simulink model "solar_pv_protected_c07_circuit"  (R2026b)
(part 6 of 16)

      | 試験資料            ; C:\Users\hosik\OneDrive\ドキュメント\ChatGPT\oosem\evaluation\pv_protection_integration_20261023_r01\runtime\observations\standard_final_r04_aggregate\aggregate.json
      | 
      | 【通電許可・停止・再許可の流れ】
      | この回路での役割    ; パネルから主電力段への通電を許可し、逆流または異常時に停止し、条件が整うまで勝手に再投入しない。
      | 起動手順1           ; マイコンはMCU_RUNとMCU_REARMをLowに置き、保持回路のクリアを成立させる。電源投入時のQ状態が最初からLowとは仮定しない。
      | 起動手順2           ; PV_U6が3.3Vと2.5Vを監視する。両方が窓内に入り復帰待ち時間を経たとき、2本のRESETが解放されANALOG_OKがHighになる。
      | 起動手順3           ; マイコンはADC CH7の保護前PV電圧とCH0の保護後VINを十分に整定して読み、入力電圧・電圧差・故障原因の解消を確認する。OFF中の電流ゼロだけを理由に復帰しない。
      | 起動手順4           ; MCU_RUNをHighへ上げる。REV_OK/ANALOG_OK/MCU_RUNがそろってクリアが解除された後、MCU_REARMへ短い立上りパルスを1回与える。Q=PV_ALLOWがHighとなる。
      | 起動手順5           ; LTC7000A自身のUV/OV・電源準備・過電流条件も成立したときゲートを充電する。RGと追加RCでON側の傾きを抑える。これは主電力段Q1/Q2のPWM制御とは別の保護開閉。
      | 逆流した場合        ; U2の出力がV_REVを下回るとPV_U3がREV_OKをLowへ下げる。公称判定は約−0.5A。AND出力がLowとなりPV_U5を非同期クリアし、PV_ALLOW Lowでゲートを放電する。停止後も保持し、再許可パルスなしに復帰しない。
      | 順方向の異常        ; LTC7000AがR27の差動電圧から順方向過電流を判定する。ISET=GND/1mΩの公称検出は約20A。UV/OVも独立に判定する。OC_FAULT_NはLow有効の故障通知。マイコンは原因を確認しRUNをLowへ戻してから復帰手順を行う設計意図。
      | 停止情報            ; PV_STOPPEDは保持回路の反転出力。実際のMOSFET遮断や故障原因を単独で保証しない。OC_FAULT_Nと電圧・電流測定を用途に応じて併用する。
      | 確認の境界          ; 試験で与えた指令・境界条件と、RP2040上で動くMicroPythonプログラムの実行確認は別。今回の記述は実ファームウェアの動作試験を実施したという意味ではない。
      | 試験との対応        ; この図面は実部品の端子と接続を示す。保存実行モジュール SHA256=f40bf5e1ef20bc97d0d4775a6ac457f3c30378c5fe9d07d29ab7bde4d975da32 の数値計算用ICコアを図面コピーから除去してある。実行用のICはメーカーのトランジスタモデルではなく、限定範囲の近似動作モデル。試験の合否と条件は C:\Users\hosik\OneDrive\ドキュメント\ChatGPT\oosem\evaluation\pv_protection_integration_20261023_r01\runtime\observations\standard_final_r04_aggregate\aggregate.json を参照する。
      | 用語と記号          ; IC：Integrated Circuit（集積回路）。GND：Ground（共通の基準電位・電流帰路）。MCU：Microcontroller Unit（マイコン）。High/Low：デジタル信号の高/低レベル。UV：Under Voltage（低電圧）、OV：Over Voltage（過電圧）、OC：Over Current（過電流）。SOA：Safe Operating Area（安全動作領域）。末尾NはLowで有効になる信号を表す。
      | 
      | 【c07 図面整理】
      | 機能区画Gate_Driver / Reverse_Detector / Stop_Latchを展開。GND以外のConnection Labelを直接配線へ置換。ICは一部品として表示。元c06の電気的接続・部品値・型番を保持する静的な図面変更。動作試験の再実行や実機確認ではない。
      mask Display: disp(sprintf('パネル側保護回路 c06\nLTC7000A / 逆流判定 / 停止保持\nダブルクリックで詳細'));port_label('lconn',1,'PV_IN');port_label('lconn',2,'GND');port_label('lconn',3,'P3V3');port_label('lconn',4,'VREF2V5');port_label('lconn',5,'MCU_RUN');port_label('lconn',6,'MCU_REARM');port_label('rconn',1,'PV_OUT');port_label('rconn',2,'IPV_OUT');port_label('rconn',3,'OC_FAULT_N');port_label('rconn',4,'PV_STOPPED');
  ProtectionNet_FLT : ConnectionLabel  Description=|  Label=PROTECTION_FLT_N
      | この回路での名前　　; PROTECTION_FLT_N
      | 種別　　　　　　　　; ConnectionLabel
      | この回路での役割　　; 保護IC P_U1のFLT出力から、RP2040基板U7のGP13へ異常状態を返す。P_RFLT_PUを介して3.3Vへプルアップされる。すべての異常や逆流を個別通知する信号ではない。
      | この場所の直接接続　; P_RFLT_PU（LTC4364のオープンドレインFLTをMCUの3.3 V系へ引き上げる／22 kΩ）: 2
      |                     ; P_U1（保護MOSFETを制御する保護IC／LTC4364IMS-1#PBF）: FLT
      | 直接接続の範囲　　　; このラベルから実際の線・分岐・明示的な境界端子だけを追った接続。同名ラベルによる離れた場所への接続はこの欄に含めない。
      | 同一ネットの主接続　; P_U1（保護MOSFETを制御する保護IC／LTC4364IMS-1#PBF）: FLT
      |                     ; U7（RP2040搭載Pico W／SC0918）: 17(GP13)
      |                     ; P_RFLT_PU（LTC4364のオープンドレインFLTをMCUの3.3 V系へ引き上げる／22 kΩ）: 2
      | 同一ネット全端子　　; P_RFLT_PU: 2
      |                     ; P_U1: FLT
      |                     ; U7: 17(GP13)
      | 接続部品数　　　　　; 3部品（部品番号で集計。同一ネット全体）
      | 接続端子数　　　　　; 3端子（423端子の部品対応表で集計。ラベル・境界ポートの重複は含めない）
      | この場所の端子数　　; 2端子／2部品（同名ラベルによる接続を除く）
      | 同階層同名ラベル数　; 2個（このラベル自身を含む）
      | 全階層の接続ラベル　; 2個（実際に同じノードへつながるラベル。名前が違う別名も含む）
      | 接続ルール　　　　　; 同じ階層の同じラベル名を仮想配線として結ぶ。別のSubsystem内とは名前だけでつながらず、明示的なConnection Portと配線をたどる。色は用途の表示であり接続を決めない。
      | 確認の範囲　　　　　; 現在の保存回路の端子・配線から求めた静的接続。抵抗やICの内部を導線として短絡せずに集計した。説明の更新は動作シミュレーション、タイミング、実部品の性能・実機動作を保証するものではない。
      | 記録の基準　　　　　; measurement_label_layout_20261022_r01/after_layout_graph.json。部品対応表は端子名の対応付けにのみ使用。
      | 
      | 【この説明欄の略語・記号】
      | 用語1　　　　　　　 ; IC：Integrated Circuit（集積回路）。複数の電子素子と機能を小さな半導体チップに集積した部品。
      | 用語2　　　　　　　 ; MCU：Microcontroller Unit（マイクロコントローラ）。プログラムを実行し、測定値の処理や出力制御を担当する小型計算機。
      | 用語3　　　　　　　 ; GPIO：General-Purpose Input/Output（汎用入出力端子）。入力・出力や周辺機能に割り当てられる端子。GPの後の数字はRP2040の端子信号番号で、基板上の物理ピン番号とは別。
      | 用語4　　　　　　　 ; MOSFET：Metal-Oxide-Semiconductor Field-Effect Transistor（金属・酸化膜・半導体構造の電界効果トランジスタ）。ゲートとソースの電圧でドレインとソースの導通を制御する素子。N-MOSはNチャネル型を表す。
      | 用語5　　　　　　　 ; FLT：Fault（故障状態通知）。LTC4364の故障警告出力。全種類の異常や逆流を一律に通知する信号という意味ではない。
  ProtectionNet_MCU_EN : ConnectionLabel  Description=|  Label=MAIN_EN
      | この回路での名前　　; MAIN_EN
      | 種別　　　　　　　　; ConnectionLabel
      | この回路での役割　　; RP2040基板U7のGP11から、保護回路の停止入力へ指令を渡す。直接同じノードなのは直列抵抗P_RSHDN_SERの入力側までで、保護ICのSHDNにはこの抵抗を介して接続する。
      | この場所の直接接続　; P_RSHDN_SER（RP2040のMAIN_ENとLTC4364のSHDN間へ入る／1 kΩ）: 1
      | 直接接続の範囲　　　; このラベルから実際の線・分岐・明示的な境界端子だけを追った接続。同名ラベルによる離れた場所への接続はこの欄に含めない。
      | 同一ネットの主接続　; U7（RP2040搭載Pico W／SC0918）: 15(GP11)
      |                     ; P_RSHDN_SER（RP2040のMAIN_ENとLTC4364のSHDN間へ入る／1 kΩ）: 1
      | 同一ネット全端子　　; P_RSHDN_SER: 1
      |                     ; U7: 15(GP11)
      | 接続部品数　　　　　; 2部品（部品番号で集計。同一ネット全体）
      | 接続端子数　　　　　; 2端子（423端子の部品対応表で集計。ラベル・境界ポートの重複は含めない）
      | この場所の端子数　　; 1端子／1部品（同名ラベルによる接続を除く）
      | 同階層同名ラベル数　; 2個（このラベル自身を含む）
      | 全階層の接続ラベル　; 2個（実際に同じノードへつながるラベル。名前が違う別名も含む）
      | 接続ルール　　　　　; 同じ階層の同じラベル名を仮想配線として結ぶ。別のSubsystem内とは名前だけでつながらず、明示的なConnection Portと配線をたどる。色は用途の表示であり接続を決めない。
      | 確認の範囲　　　　　; 現在の保存回路の端子・配線から求めた静的接続。抵抗やICの内部を導線として短絡せずに集計した。説明の更新は動作シミュレーション、タイミング、実部品の性能・実機動作を保証するものではない。
      | 記録の基準　　　　　; measurement_label_layout_20261022_r01/after_layout_graph.json。部品対応表は端子名の対応付けにのみ使用。
      | 
      | 【この説明欄の略語・記号】
      | 用語1　　　　　　　 ; IC：Integrated Circuit（集積回路）。複数の電子素子と機能を小さな半導体チップに集積した部品。
      | 用語2　　　　　　　 ; MCU：Microcontroller Unit（マイクロコントローラ）。プログラムを実行し、測定値の処理や出力制御を担当する小型計算機。
      | 用語3　　　　　　　 ; GPIO：General-Purpose Input/Output（汎用入出力端子）。入力・出力や周辺機能に割り当てられる端子。GPの後の数字はRP2040の端子信号番号で、基板上の物理ピン番号とは別。
      | 用語4　　　　　　　 ; SHDN：Shutdown（停止制御端子）。LTC4364ではLowで停止を指示する。Highは動作許可であり、保護判定を無効にするものではない。
      | 用語5　　　　　　　 ; EN：Enable（動作許可）。対象機能の動作を許可する信号。端子ごとの有効レベルや接続状態に従う。
  ProtectionNet_RETURN : ConnectionLabel  Description=|  Label=GND
      | この回路での名前　　; GND
      | 種別　　　　　　　　; ConnectionLabel
      | この回路での役割　　; 電池BT1の負極、太陽電池列の負極、制御・測定・保護回路のGNDを結ぶ共通の帰路。高側駆動の浮動帰路SWとは別のノード。
      | 共通帰路の代表接続　; BT1（充電先の蓄電池／51.2V 100Ah LiFePO4）: -
      |                     ; PV1（直列太陽電池列の負極側パネル／400W panel 1/2）: -
      |                     ; U7（RP2040搭載Pico W／SC0918）: 3(GND), 8(GND), 13(GND), 18(GND), 23(GND), 28(GND), 33(AGND), 38(GND)
      |                     ; U1（外付けADC／MCP3208-CI/SL）: 8(CH7), 9(DGND), 14(AGND)
      |                     ; P_U1（保護MOSFETを制御する保護IC／LTC4364IMS-1#PBF）: GND
      |                     ; Q2（同期整流降圧回路の下側スイッチ／TK9R6E15Q5,S1X）: 3(S)
      |                     ; U9（低側の光ゲートドライバ／ACPL-P346-560E）: 4(VEE)
      |                     ; U10（高側ゲート用の浮動電源を作る絶縁DC/DC／UCC14131QDWNRQ1）: 1(GNDP), 2(GNDP), 5(GNDP), 8(GNDP), 9(GNDP), 10(GNDP), 11(GNDP), 12(GNDP), 13(GNDP), 14(GNDP), 15(GNDP), 16(GNDP), 17(GNDP), 18(GNDP)
      | この場所の直接接続　; P_RSHDN_PD（SHDNをGNDへ下げ、MCU未駆動時に停止側へ保つ／47 kΩ）: 2
      | 直接接続の範囲　　　; このラベルから実際の線・分岐・明示的な境界端子だけを追った接続。同名ラベルによる離れた場所への接続はこの欄に含めない。
      | 同一ネット全端子　　; BT1: -
      |                     ; C1: 2(n)
      |                     ; C2: 2(n)
      |                     ; C3: 2(n)
      |                     ; C4: 2(n)
      |                     ; C7: 2(n)
      |                     ; C8: 2(n)
      |                     ; C9: 2(n)
      |                     ; C10: 2(n)
      |                     ; C13: 2(n)
      |                     ; C14: 2(n)
      |                     ; C15: 2(n)
      |                     ; C16: 2(n)
      |                     ; C17: 2
      |                     ; C18: 2
      |                     ; C19: 2
      |                     ; C20: 2
      |                     ; C21: 2
      |                     ; C22: 2
      |                     ; C23: 2
      |                     ; C24: 2
      |                     ; C25: 2
      |                     ; C26: 2
      |                     ; C27: 2
      |                     ; C28: 2
      |                     ; C29: 2
      |                     ; C30: 2
      |                     ; C31: 2
      |                     ; C33: 2
      |                     ; C34: 2
      |                     ; C35: 2
      |                     ; C36: 2
      |                     ; C40: 2
      |                     ; C41: 2
      |                     ; C42: 2
      |                     ; C43: 2
      |                     ; C44: 2
      |                     ; C45: 2
      |                     ; C46: 2
      |                     ; C47: 2
      |                     ; C48: 2
      |                     ; D2: 2(A)
      |                     ; PV1: -
      |                     ; P_CHG: N
      |                     ; P_COUT: N
      |                     ; P_CTMR: N
      |                     ; P_D1: A
      |                     ; P_R3: 2
      |                     ; P_R8: 2
      |                     ; P_RSHDN_PD: 2
      |                     ; P_U1: GND
      |                     ; Q2: 3(S)
      |                     ; Q3: 1(S1), 4(S2)
      |                     ; R1: 2(n)
      |                     ; R18: 2
      |                     ; R21: 2
      |                     ; R24: 2
      |                     ; R35: 2
      |                     ; R42: 2
      |                     ; R44: 2
      |                     ; R48: 2
      |                     ; U1: 8(CH7), 9(DGND), 14(AGND)
      |                     ; U2: 2(GND), 3(REF2), 4(RESERVED_GND)
      |                     ; U3: 2(GND), 3(REF2), 4(RESERVED_GND)
      |                     ; U4: 3(GND)
      |                     ; U5: 3(GND)
      |                     ; U6: 3(GND)
      |                     ; U7: 3(GND), 8(GND), 13(GND), 18(GND), 23(GND), 28(GND), 33(AGND), 38(GND)
      |                     ; U9: 4(VEE)
      |                     ; U10: 1(GNDP), 2(GNDP), 5(GNDP), 8(GNDP), 9(GNDP), 10(GNDP), 11(GNDP), 12(GNDP), 13(GNDP), 14(GNDP), 15(GNDP), 16(GNDP), 17(GNDP), 18(GNDP)
      |                     ; U11: 2(GND)
      |                     ; U12: 2(GND)
      | 接続部品数　　　　　; 72部品（部品番号で集計。同一ネット全体）
      | 接続端子数　　　　　; 99端子（423端子の部品対応表で集計。ラベル・境界ポートの重複は含めない）
      | この場所の端子数　　; 1端子／1部品（同名ラベルによる接続を除く）
      | 同階層同名ラベル数　; 75個（このラベル自身を含む）
      | 全階層の接続ラベル　; 87個（実際に同じノードへつながるラベル。名前が違う別名も含む）
      | 接続ルール　　　　　; 同じ階層の同じラベル名を仮想配線として結ぶ。別のSubsystem内とは名前だけでつながらず、明示的なConnection Portと配線をたどる。色は用途の表示であり接続を決めない。
      | 確認の範囲　　　　　; 現在の保存回路の端子・配線から求めた静的接続。抵抗やICの内部を導線として短絡せずに集計した。説明の更新は動作シミュレーション、タイミング、実部品の性能・実機動作を保証するものではない。
      | 記録の基準　　　　　; measurement_label_layout_20261022_r01/after_layout_graph.json。部品対応表は端子名の対応付けにのみ使用。
      | 
      | 【この説明欄の略語・記号】
      | 用語1　　　　　　　 ; DC：Direct Current（直流）。ここでは直流電源または直流成分。DCバイアスはコンデンサに重なる直流電圧を指す。
      | 用語2　　　　　　　 ; DC/DC：DC-to-DC Converter（直流電圧変換器）。直流入力を別の直流電圧へ変換する電源回路。絶縁の有無は個々の部品説明で確認する。
      | 用語3　　　　　　　 ; ADC：Analog-to-Digital Converter（アナログ・デジタル変換器）。測定電圧をデジタル値へ変換する回路。電流や温度も、センサーで電圧へ変換した後に読み取る。
      | 用語4　　　　　　　 ; IC：Integrated Circuit（集積回路）。複数の電子素子と機能を小さな半導体チップに集積した部品。
      | 用語5　　　　　　　 ; MCU：Microcontroller Unit（マイクロコントローラ）。プログラムを実行し、測定値の処理や出力制御を担当する小型計算機。
      | 用語6　　　　　　　 ; CH：Channel（測定チャネル）。CH0〜CH7はADCの入力番号であり、同時測定を意味しない。
      | 用語7　　　　　　　 ; MOSFET：Metal-Oxide-Semiconductor Field-Effect Transistor（金属・酸化膜・半導体構造の電界効果トランジスタ）。ゲートとソースの電圧でドレインとソースの導通を制御する素子。N-MOSはNチャネル型を表す。
      | 用語8　　　　　　　 ; LiFePO4：Lithium Iron Phosphate（リン酸鉄リチウム）。電池の正極材料を示す化学式。英語の頭文字を並べた略語ではない。
      | 用語9　　　　　　　 ; GND：Ground（回路の基準電位・電流帰路）。この図の共通基準。保護接地や大地への接続を意味するとは限らない。
      | 用語10　　　　　　　; AGND：Analog Ground（アナログ回路の基準端子）。アナログ部分の電流帰路。現図では共通GNDへ接続されるが、実装時の電流経路への配慮は別途必要。
      | 用語11　　　　　　　; DGND：Digital Ground（デジタル回路の基準端子）。デジタル部分の電流帰路。現図では共通GNDへ接続される。
      | 用語12　　　　　　　; SHDN：Shutdown（停止制御端子）。LTC4364ではLowで停止を指示する。Highは動作許可であり、保護判定を無効にするものではない。
      | 用語13　　　　　　　; VREF/REF：基準電圧を表す端子名。REFはReference（基準）の意味。ADCの変換尺度や電流アンプの出力基準に使う。REF1/REF2の接続電位は個別に確認する。
      | 用語14　　　　　　　; VCC/VDD/VEE/VS：ICの電源端子名。文字の歴史的な由来を現在の接続機能へ当てはめない。現回路のVEEはU8/U10では浮動基準SW、U9ではGND。各電圧・基準は端子と接続を参照する。
      | 用語15　　　　　　　; GNDP：U10の一次側電源の基準端子。絶縁電源の入力側GND。二次側基準VEE=SWと直接同一の導体ではない。
      | 用語16　　　　　　　; SW：Switching Node（スイッチング点）。主電力段の上下MOSFETとL1がつながる、電圧が高速に切り替わる点。GNDとは別電位。
  ProtectionNet_VLOGIC : ConnectionLabel  Description=|  Label=V3V3
      | この回路での名前　　; V3V3
      | 種別　　　　　　　　; ConnectionLabel
      | この回路での役割　　; RP2040基板U7の3.3V出力から、ADC・電流検出IC・温度センサー・基準電圧ICなどへ電源を分配する。信号のプルアップ抵抗にも供給する。
      | この場所の直接接続　; P_RFLT_PU（LTC4364のオープンドレインFLTをMCUの3.3 V系へ引き上げる／22 kΩ）: 1
      | 直接接続の範囲　　　; このラベルから実際の線・分岐・明示的な境界端子だけを追った接続。同名ラベルによる離れた場所への接続はこの欄に含めない。
      | 同一ネットの主接続　; U7（RP2040搭載Pico W／SC0918）: 36(3V3_OUT)
      |                     ; U1（外付けADC／MCP3208-CI/SL）: 16(VDD)
      |                     ; U2（PV入力電流の検出アンプ／INA241A3IDDFR）: 6(VS)
      |                     ; U3（L1直後の出力電流の検出アンプ／INA241A3IDDFR）: 6(VS)
      |                     ; U4（電池温度センサー／TMP235A2DBZR）: 1(VDD)
      |                     ; U5（放熱器温度センサー／TMP235A2DBZR）: 1(VDD)
      |                     ; U6（2.5Vの測定基準電圧源／REF3025EAIDBZR）: 1(IN)
      |                     ; R49（U10のオープンドレインPG信号BIAS_PGをPicoの3V3へ引き上げ、GP9で読める電圧にする／10k 1%）: 2
      |                     ; P_RFLT_PU（LTC4364のオープンドレインFLTをMCUの3.3 V系へ引き上げる／22 kΩ）: 1
      | 同一ネット全端子　　; C17: 1
      |                     ; C18: 1
      |                     ; C22: 1
      |                     ; C24: 1
      |                     ; C26: 1
      |                     ; C28: 1
      |                     ; C30: 1
      |                     ; P_RFLT_PU: 1
      |                     ; R15: 1
      |                     ; R49: 2
      |                     ; U1: 16(VDD)
      |                     ; U2: 6(VS)
      |                     ; U3: 6(VS)
      |                     ; U4: 1(VDD)
      |                     ; U5: 1(VDD)
      |                     ; U6: 1(IN)
      |                     ; U7: 36(3V3_OUT)
      | 接続部品数　　　　　; 17部品（部品番号で集計。同一ネット全体）
      | 接続端子数　　　　　; 17端子（423端子の部品対応表で集計。ラベル・境界ポートの重複は含めない）
      | この場所の端子数　　; 1端子／1部品（同名ラベルによる接続を除く）
      | 同階層同名ラベル数　; 10個（このラベル自身を含む）
      | 全階層の接続ラベル　; 10個（実際に同じノードへつながるラベル。名前が違う別名も含む）
      | 接続ルール　　　　　; 同じ階層の同じラベル名を仮想配線として結ぶ。別のSubsystem内とは名前だけでつながらず、明示的なConnection Portと配線をたどる。色は用途の表示であり接続を決めない。
      | 確認の範囲　　　　　; 現在の保存回路の端子・配線から求めた静的接続。抵抗やICの内部を導線として短絡せずに集計した。説明の更新は動作シミュレーション、タイミング、実部品の性能・実機動作を保証するものではない。
      | 記録の基準　　　　　; measurement_label_layout_20261022_r01/after_layout_graph.json。部品対応表は端子名の対応付けにのみ使用。
      | 
      | 【この説明欄の略語・記号】
      | 用語1　　　　　　　 ; ADC：Analog-to-Digital Converter（アナログ・デジタル変換器）。測定電圧をデジタル値へ変換する回路。電流や温度も、センサーで電圧へ変換した後に読み取る。
      | 用語2　　　　　　　 ; IC：Integrated Circuit（集積回路）。複数の電子素子と機能を小さな半導体チップに集積した部品。
      | 用語3　　　　　　　 ; MCU：Microcontroller Unit（マイクロコントローラ）。プログラムを実行し、測定値の処理や出力制御を担当する小型計算機。
      | 用語4　　　　　　　 ; GPIO：General-Purpose Input/Output（汎用入出力端子）。入力・出力や周辺機能に割り当てられる端子。GPの後の数字はRP2040の端子信号番号で、基板上の物理ピン番号とは別。
      | 用語5　　　　　　　 ; MOSFET：Metal-Oxide-Semiconductor Field-Effect Transistor（金属・酸化膜・半導体構造の電界効果トランジスタ）。ゲートとソースの電圧でドレインとソースの導通を制御する素子。N-MOSはNチャネル型を表す。
      | 用語6　　　　　　　 ; PV：Photovoltaic（太陽光発電）。光を電気へ変える発電方式。PVを含むネット名は太陽電池側の測定・電力経路を表す。
      | 用語7　　　　　　　 ; GND：Ground（回路の基準電位・電流帰路）。この図の共通基準。保護接地や大地への接続を意味するとは限らない。
      | 用語8　　　　　　　 ; PG：Power Good（電源状態通知）。電源出力が規定状態にあるかを知らせる信号。プルアップ条件と実際の通知条件は対象ICの説明で確認する。
      | 用語9　　　　　　　 ; FLT：Fault（故障状態通知）。LTC4364の故障警告出力。全種類の異常や逆流を一律に通知する信号という意味ではない。
      | 用語10　　　　　　　; VCC/VDD/VEE/VS：ICの電源端子名。文字の歴史的な由来を現在の接続機能へ当てはめない。現回路のVEEはU8/U10では浮動基準SW、U9ではGND。各電圧・基準は端子と接続を参照する。
      | 用語11　　　　　　　; SW：Switching Node（スイッチング点）。主電力段の上下MOSFETとL1がつながる、電圧が高速に切り替わる点。GNDとは別電位。
  Q1 : ee_lib/Semiconductors & Converters/N-Channel MOSFET  Description=|  paramTerminal=ee.enum.mosfet.numberOfTerminals.three  parameterization=ee.enum.mosfet.parameterization.datasheet  Beta=5.0 A/V^2  Rds=0.025 Ohm  Id=6.0 A  Vgs=10 V  Vth=1.7 V  Vth0=1.7 V  lam=0 1/V  gamma_vth=0.5 V^(1/2)  phib=0.5 V  Vth1=1.9071 V  Vbs1=-1 V  Vth2=2.066 V  Vbs2=-2 V  Tmeas=25 degC  Vgs_vec=[-1, -.5, 2, 3, 4, 5] V  Vds_vec=[0, 2, 4, 8, 12, 16, 20] V  Vbs_vec=[0, -4, -6, -12] V  T_vec=[25, 125] degC  Vth_vec=[.4, 1.2, 1.4, 1.45] V  Vth_mat=[.4, .35; 1.2, 1.15; 1.4, 1.35; 1.45, 1.4] V  Ids_mat=[0, 0, 0, 0, 0, 0, 0; 0, 0, 0, 0, 0, 0, 0; 0, .003, .0038, .0043, .0046, .0048, .0049; 0, .0055, .008, .009, .0095, .01, .0101; 0, .0115, .016, .018, .019, .0195, .02; 0, .0152, .0225, .0265, .028, .0295, .03] A  Ids_mat0=[0, 0, 0, 0, 0, 0, 0; 0, 0, 0, 0, 0, 0, 0; 0, .003, .0038, .0043, .0046, .0048, .0049; 0, .0055, .008, .009, .0095, .01, .0101; 0, .0115, .016, .018, .019, .0195, .02; 0, .0152, .0225, .0265, .028, .0295, .03] A  Ids_mat_3D=zeros(6, 7, 2) A  Ids_mat_3D0=zeros(6, 7, 2) A  IV_table_symmetry=ee.enum.mosfet.symmetricNIV.no  RS=0.0001 Ohm  RD=0.01 Ohm  RB=0.001 Ohm  LeadRs=0 Ohm  LeadRd=0 Ohm  LeadRg=0 Ohm  LeadRb=0 Ohm  LS=0 nH  LD=0 nH  LG=0 nH  LB=0 nH  C_param=ee.enum.mosfet.capacitanceParam.fixedciss  C_GS=270 pF  C_GD=80 pF  C_GB=0 pF  C_DS=0 pF  C_iss=350 pF  C_rss=80 pF  C_oss=0 pF  C_iss_vec=[720, 700, 590, 470, 390, 310] pF  C_rss_vec=[450, 400, 300, 190, 95, 55] pF  C_oss_vec=[900, 810, 690, 420, 270, 170] pF  C_GS_vec=[270, 300, 290, 280, 295, 255] pF  C_GD_vec=[450, 400, 300, 190, 95, 55] pF  C_GB_vec=[270, 300, 290, 280, 295, 255] pF  C_Vgs_vec=0 V  C_DS_vec=[450, 410, 390, 230, 175, 115] pF  C_Vds_vec=[.1, .3, 1, 3, 10, 30] V  V_GS_for_cap_data=0 V  charge_linearity_param=ee.enum.mosfet.cgdLinearity.constant  C_OX=200 pF  V_C_OX=-0.5 V  charge_linearity_param_vgb=ee.enum.mosfet.cgbLinearity.instantly  charge_linearity_param_with_vgb=ee.enum.mosfet.cgbLinearityWithSeparateCgb.instantly  Di_param=ee.enum.mosfet.diodeParam.no  IsDiode=1e-12 A  Vbi=0.6 V  n=1  Cj0Diode=0 pF  TT=50e-9 s  Tmeas_dio=25 degC  TableTypeNoT=ee.enum.mosfet.tableType.IfMat  TableType=ee.enum.diode.tableType.IfMat  IfVec=[.07, .12, .19, 1.75, 4.24, 7.32, 11.2] A  IfMat=[.07, .12, .19, 1.75, 4.24, 7.32, 11.2; .16, .3, .72, 2.14, 4.02, 6.35, 9.12] A  VfVecV=[.9, 1.15, 1.25, 1.5, 1.75, 2.17, 2.6, 2.85] V  VfMatV=[.9, 1.15, 1.25, 1.5, 1.75, 2.17, 2.6, 2.85; .58, .68, .75, 1.1, 1.38, 1.77, 2.27, 2.7] V  TjVec=[25, 125] degC  VfVec=[.5, .7, .9, 1.3, 1.7, 2.1, 2.5] V  IfVecV=[.1, .2, .5, 1, 2, 4, 7, 10] A  diode_Goff=1e-12 1/Ohm  prmDatasheet=ee.enum.temperatureParameterization.none  prmEquCoeff=ee.enum.temperatureParameterization.none  dVth_dT=-6 mV/K  dVth0_dT=-6 mV/K  Rds_T2=0.037 Ohm  BEXDatasheet=-1.5  BEXEquCoeff=-1.5  etaisDatasheet=3  etaisEquCoeff=3  Tmeas2=125 degC  etaisTabulated=3  TdeviceDatasheet=25 degC  TdeviceEquCoeff=25 degC  TdeviceTabulated=25 degC  i_g_specify=off  i_g_priority=None  i_g=0 A  i_g_nominal_specify=off  i_g_nominal_value=1  i_g_nominal_unit=A  i_d_specify=off  i_d_priority=None  i_d=0 A  i_d_nominal_specify=off  i_d_nominal_value=1  i_d_nominal_unit=A  i_b_specify=off  i_b_priority=None  i_b=0 A  i_b_nominal_specify=off  i_b_nominal_value=1  i_b_nominal_unit=A  voltage_gs_specify=off  voltage_gs_priority=None  voltage_gs=0 V  voltage_gs_nominal_specify=off  voltage_gs_nominal_value=1  voltage_gs_nominal_unit=V  voltage_ds_specify=off  voltage_ds_priority=None  voltage_ds=0 V  voltage_ds_nominal_specify=off  voltage_ds_nominal_value=1  voltage_ds_nominal_unit=V  voltage_bs_specify=off  voltage_bs_priority=None  voltage_bs=0 V  voltage_bs_nominal_specify=off  voltage_bs_nominal_value=1  voltage_bs_nominal_unit=V  v_Cgs_specify=off  v_Cgs_priority=High  v_Cgs=0 V  v_Cgs_nominal_specify=off  v_Cgs_nominal_value=1  v_Cgs_nominal_unit=V  v_Cds_specify=off  v_Cds_priority=High  v_Cds=0 V  v_Cds_nominal_specify=off  v_Cds_nominal_value=1  v_Cds_nominal_unit=V  v_Cbs_specify=off  v_Cbs_priority=High  v_Cbs=0 V  v_Cbs_nominal_specify=off  v_Cbs_nominal_value=1  v_Cbs_nominal_unit=V  thermal_network_parameterization=ee.enum.thermalNetworkTopology.junctionCase  Rth=[0, 10] K/W  Rth_Cauer=[1, 3, 10] K/W  Rth_Foster=[.08, .14, .22, .16] K/W  thermal_mass_parameterization=ee.enum.thermalNetwork.timeconstant  thermal_mass=[0, 1] J/K  thermal_mass_Cauer=[.1, .3, 1] J/K  thermal_mass_Foster=[.001, .005, .05, .5] J/K  thermal_time_constant=[0, 10] s  thermal_time_constant_Cauer=[1, 3, 10] s  thermal_time_constant_Foster=[7e-05, .0007, .01, .08] s  thermal_mass_initial_temperatures=[25, 25] degC  thermal_mass_initial_temperatures_Cauer=[25, 25, 25] degC  Tvec_initial_Foster=[25, 25, 25, 25] degC  betaref=18 A/V^2  Vfbref=-1.1 V  gamma=3.5 V^(1/2)  phib2ref=1 V  thesatref=0.4 1/V  alpha=0  Vp=5e-2 V  thesrref=0 1/V  m=8  Tref=25 degC  Rsref=2e-3 Ohm  Rdref=0.17 Ohm  Rgref=8.4 Ohm  Rbref=2e-3 Ohm  Cox=1500 pF  Cgso=100 pF  Cgdo=14 pF  Isref=5.2e-13 A  Cj0=480 pF  Tprm=ee.enum.temperatureParameterization.none  etabet=1.3  Stvfb=5e-4 V/K  Stphib=-8.5e-4 V/K  etasat=1.04  etasr=0.65  etar=0.95  etais=3  Tsim=25 degC  Ig_specify=off  Ig_priority=None  Ig=0 A  Ig_nominal_specify=off  Ig_nominal_value=1  Ig_nominal_unit=nA  Ids_specify=off  Ids_priority=None  Ids=0 A  Ids_nominal_specify=off  Ids_nominal_value=1  Ids_nominal_unit=A  Ib_specify=off  Ib_priority=None  Ib=0 A  Ib_nominal_specify=off  Ib_nominal_value=1  Ib_nominal_unit=uA  V_gs_specify=off  V_gs_priority=None  V_gs=0 V  V_gs_nominal_specify=off  V_gs_nominal_value=1  V_gs_nominal_unit=V  V_ds_specify=off  V_ds_priority=None  V_ds=0 V  V_ds_nominal_specify=off  V_ds_nominal_value=1  V_ds_nominal_unit=V  V_bs_specify=off  V_bs_priority=None  V_bs=0 V  V_bs_nominal_specify=off  V_bs_nominal_value=1  V_bs_nominal_unit=V  QGoverCox_specify=off  QGoverCox_priority=None  QGoverCox=0 V  QGoverCox_nominal_specify=off  QGoverCox_nominal_value=1  QGoverCox_nominal_unit=V  QDoverCox_specify=off  QDoverCox_priority=None  QDoverCox=0 V  QDoverCox_nominal_specify=off  QDoverCox_nominal_value=1  QDoverCox_nominal_unit=V  QBoverCox_specify=off  QBoverCox_priority=None  QBoverCox=0 V  QBoverCox_nominal_specify=off  QBoverCox_nominal_value=1  QBoverCox_nominal_unit=V  T0=[25, 25] degC  T0_Cauer=[25, 25, 25] degC
      | この回路での名前　　; Q1
      | 部品名　　　　　　　; TK9R6E15Q5,S1X
      | この回路での役割　　; 太陽電池から主インダクタL1へ電力を送り込む、降圧回路の上側スイッチ。
      | ここでの動き　　　　; ゲートドライバU8の指令でON/OFFし、入力電源をL1側へつなぐ時間を調整する。ソースの電圧も上下するため、ゲートはソースSWに対する電圧で駆動する。
      | 
      | 【詳しい働き・仕様・接続・確認の範囲】
      | 部品種別　　　　　　; 上側NチャネルMOSFET
      | 公称値　　　　　　　; TK9R6E15Q5,S1X
      | 配置目的　　　　　　; 同期整流降圧回路の上側スイッチ。VINをSWへ断続的に接続し、L1へエネルギーを渡す。
      | 意図する動作　　　　; U8からR36を介して駆動。ソースSWはスイッチングするため、ゲート電圧はSW基準で扱う。Q2との同時ONを避ける必要がある。
      | 端子と接続　　　　　; 3 S → SW、1 G → GATE_H、2 D → VIN
      | モデルの範囲　　　　; Simscape標準NチャネルMOSFETの近似。掲載型番の全特性へ同定済みではなく、設定値とメーカー定格を区別する。Idはモデル校正用電流で最大許容電流ではない。
      | モデル設定　　　　　; Rds=25 mΩ、Vgs=10 V、Id=6 A、Vth=1.7 V、LeadRg=0 Ω。これらは保存モデルの設定値であり、すべてが実部品の保証値という意味ではない。
      | 確認の範囲　　　　　; 本説明は保存回路の部品情報・端子割当・既存設計意図を整理したもの。今回の説明更新によって新たな動作試験や実機検証を実施した意味ではない。
      | 設計記録　　　　　　; evaluation\component_annotations_20261022_r01\before_graph.json
      | evaluation\component_annotations_20261022_r01\before_metadata.json
      | evaluation\protection_capacitor_integration_20261021_r01\final_delivery\independent_readback\physical_bom.json
      | 
      | 【この説明欄の略語・記号】
      | 用語1　　　　　　　 ; MOSFET：Metal-Oxide-Semiconductor Field-Effect Transistor（金属・酸化膜・半導体構造の電界効果トランジスタ）。ゲートとソースの電圧でドレインとソースの導通を制御する素子。N-MOSはNチャネル型を表す。
      | 用語2　　　　　　　 ; VGS：Gate-to-Source Voltage（ゲート・ソース間電圧）。ゲートの電圧をソース基準で表す。GND基準のゲート電圧とは同じとは限らない。
      | 用語3　　　　　　　 ; Rds：Drain-to-Source On-Resistance（導通時のドレイン・ソース間抵抗）。十分にONにした条件での抵抗。温度やゲート電圧などの条件に依存する。
      | 用語4　　　　　　　 ; Vth：Threshold Voltage（しきい値電圧）。MOSFETが指定された小電流を流し始めるゲート電圧の目安。十分にONにする駆動電圧ではない。
      | 用語5　　　　　　　 ; ID：Drain Current（ドレイン電流）。MOSFETのドレインを流れる電流。Idというモデル設定値は校正条件である場合があり、最大電流定格とは区別する。
      | 用語6　　　　　　　 ; LeadRg：Gate lead resistance（モデル内のゲート側直列抵抗パラメータ）。このモデルで内部ゲート抵抗をまとめて与える設定名。パッケージのリード単独の抵抗という保証値ではない。
      | 用語7　　　　　　　 ; GND：Ground（回路の基準電位・電流帰路）。この図の共通基準。保護接地や大地への接続を意味するとは限らない。
      | 用語8　　　　　　　 ; VIN/VOUT：入力電圧・出力電圧を表す端子／ネット名。INは入力、OUTは出力。電源変換器の電力端子なのか、検出用端子なのかは対象部品によって異なるため、端子と接続の説明に従う。
      | 用語9　　　　　　　 ; SW：Switching Node（スイッチング点）。主電力段の上下MOSFETとL1がつながる、電圧が高速に切り替わる点。GNDとは別電位。
      settings: AttributesFormatString=N-MOS 上側
  Q2 : ee_lib/Semiconductors & Converters/N-Channel MOSFET  Description=|  paramTerminal=ee.enum.mosfet.numberOfTerminals.three  parameterization=ee.enum.mosfet.parameterization.datasheet  Beta=5.0 A/V^2  Rds=0.025 Ohm  Id=6.0 A  Vgs=10 V  Vth=1.7 V  Vth0=1.7 V  lam=0 1/V  gamma_vth=0.5 V^(1/2)  phib=0.5 V  Vth1=1.9071 V  Vbs1=-1 V  Vth2=2.066 V  Vbs2=-2 V  Tmeas=25 degC  Vgs_vec=[-1, -.5, 2, 3, 4, 5] V  Vds_vec=[0, 2, 4, 8, 12, 16, 20] V  Vbs_vec=[0, -4, -6, -12] V  T_vec=[25, 125] degC  Vth_vec=[.4, 1.2, 1.4, 1.45] V  Vth_mat=[.4, .35; 1.2, 1.15; 1.4, 1.35; 1.45, 1.4] V  Ids_mat=[0, 0, 0, 0, 0, 0, 0; 0, 0, 0, 0, 0, 0, 0; 0, .003, .0038, .0043, .0046, .0048, .0049; 0, .0055, .008, .009, .0095, .01, .0101; 0, .0115, .016, .018, .019, .0195, .02; 0, .0152, .0225, .0265, .028, .0295, .03] A  Ids_mat0=[0, 0, 0, 0, 0, 0, 0; 0, 0, 0, 0, 0, 0, 0; 0, .003, .0038, .0043, .0046, .0048, .0049; 0, .0055, .008, .009, .0095, .01, .0101; 0, .0115, .016, .018, .019, .0195, .02; 0, .0152, .0225, .0265, .028, .0295, .03] A  Ids_mat_3D=zeros(6, 7, 2) A  Ids_mat_3D0=zeros(6, 7, 2) A  IV_table_symmetry=ee.enum.mosfet.symmetricNIV.no  RS=0.0001 Ohm  RD=0.01 Ohm  RB=0.001 Ohm  LeadRs=0 Ohm  LeadRd=0 Ohm  LeadRg=0 Ohm  LeadRb=0 Ohm  LS=0 nH  LD=0 nH  LG=0 nH  LB=0 nH  C_param=ee.enum.mosfet.capacitanceParam.fixedciss  C_GS=270 pF  C_GD=80 pF  C_GB=0 pF  C_DS=0 pF  C_iss=350 pF  C_rss=80 pF  C_oss=0 pF  C_iss_vec=[720, 700, 590, 470, 390, 310] pF  C_rss_vec=[450, 400, 300, 190, 95, 55] pF  C_oss_vec=[900, 810, 690, 420, 270, 170] pF  C_GS_vec=[270, 300, 290, 280, 295, 255] pF  C_GD_vec=[450, 400, 300, 190, 95, 55] pF  C_GB_vec=[270, 300, 290, 280, 295, 255] pF  C_Vgs_vec=0 V  C_DS_vec=[450, 410, 390, 230, 175, 115] pF  C_Vds_vec=[.1, .3, 1, 3, 10, 30] V  V_GS_for_cap_data=0 V  charge_linearity_param=ee.enum.mosfet.cgdLinearity.constant  C_OX=200 pF  V_C_OX=-0.5 V  charge_linearity_param_vgb=ee.enum.mosfet.cgbLinearity.instantly  charge_linearity_param_with_vgb=ee.enum.mosfet.cgbLinearityWithSeparateCgb.instantly  Di_param=ee.enum.mosfet.diodeParam.no  IsDiode=1e-12 A  Vbi=0.6 V  n=1  Cj0Diode=0 pF  TT=50e-9 s  Tmeas_dio=25 degC  TableTypeNoT=ee.enum.mosfet.tableType.IfMat  TableType=ee.enum.diode.tableType.IfMat  IfVec=[.07, .12, .19, 1.75, 4.24, 7.32, 11.2] A  IfMat=[.07, .12, .19, 1.75, 4.24, 7.32, 11.2; .16, .3, .72, 2.14, 4.02, 6.35, 9.12] A  VfVecV=[.9, 1.15, 1.25, 1.5, 1.75, 2.17, 2.6, 2.85] V  VfMatV=[.9, 1.15, 1.25, 1.5, 1.75, 2.17, 2.6, 2.85; .58, .68, .75, 1.1, 1.38, 1.77, 2.27, 2.7] V  TjVec=[25, 125] degC  VfVec=[.5, .7, .9, 1.3, 1.7, 2.1, 2.5] V  IfVecV=[.1, .2, .5, 1, 2, 4, 7, 10] A  diode_Goff=1e-12 1/Ohm  prmDatasheet=ee.enum.temperatureParameterization.none  prmEquCoeff=ee.enum.temperatureParameterization.none  dVth_dT=-6 mV/K  dVth0_dT=-6 mV/K  Rds_T2=0.037 Ohm  BEXDatasheet=-1.5  BEXEquCoeff=-1.5  etaisDatasheet=3  etaisEquCoeff=3  Tmeas2=125 degC  etaisTabulated=3  TdeviceDatasheet=25 degC  TdeviceEquCoeff=25 degC  TdeviceTabulated=25 degC  i_g_specify=off  i_g_priority=None  i_g=0 A  i_g_nominal_specify=off  i_g_nominal_value=1  i_g_nominal_unit=A  i_d_specify=off  i_d_priority=None  i_d=0 A  i_d_nominal_specify=off  i_d_nominal_value=1  i_d_nominal_unit=A  i_b_specify=off  i_b_priority=None  i_b=0 A  i_b_nominal_specify=off  i_b_nominal_value=1  i_b_nominal_unit=A  voltage_gs_specify=off  voltage_gs_priority=None  voltage_gs=0 V  voltage_gs_nominal_specify=off  voltage_gs_nominal_value=1  voltage_gs_nominal_unit=V  voltage_ds_specify=off  voltage_ds_priority=None  voltage_ds=0 V  voltage_ds_nominal_specify=off  voltage_ds_nominal_value=1  voltage_ds_nominal_unit=V  voltage_bs_specify=off  voltage_bs_priority=None  voltage_bs=0 V  voltage_bs_nominal_specify=off  voltage_bs_nominal_value=1  voltage_bs_nominal_unit=V  v_Cgs_specify=off  v_Cgs_priority=High  v_Cgs=0 V  v_Cgs_nominal_specify=off  v_Cgs_nominal_value=1  v_Cgs_nominal_unit=V  v_Cds_specify=off  v_Cds_priority=High  v_Cds=0 V  v_Cds_nominal_specify=off  v_Cds_nominal_value=1  v_Cds_nominal_unit=V  v_Cbs_specify=off  v_Cbs_priority=High  v_Cbs=0 V  v_Cbs_nominal_specify=off  v_Cbs_nominal_value=1  v_Cbs_nominal_unit=V  thermal_network_parameterization=ee.enum.thermalNetworkTopology.junctionCase  Rth=[0, 10] K/W  Rth_Cauer=[1, 3, 10] K/W  Rth_Foster=[.08, .14, .22, .16] K/W  thermal_mass_parameterization=ee.enum.thermalNetwork.timeconstant  thermal_mass=[0, 1] J/K  thermal_mass_Cauer=[.1, .3, 1] J/K  thermal_mass_Foster=[.001, .005, .05, .5] J/K  thermal_time_constant=[0, 10] s  thermal_time_constant_Cauer=[1, 3, 10] s  thermal_time_constant_Foster=[7e-05, .0007, .01, .08] s  thermal_mass_initial_temperatures=[25, 25] degC  thermal_mass_initial_temperatures_Cauer=[25, 25, 25] degC  Tvec_initial_Foster=[25, 25, 25, 25] degC  betaref=18 A/V^2  Vfbref=-1.1 V  gamma=3.5 V^(1/2)  phib2ref=1 V  thesatref=0.4 1/V  alpha=0  Vp=5e-2 V  thesrref=0 1/V  m=8  Tref=25 degC  Rsref=2e-3 Ohm  Rdref=0.17 Ohm  Rgref=8.4 Ohm  Rbref=2e-3 Ohm  Cox=1500 pF  Cgso=100 pF  Cgdo=14 pF  Isref=5.2e-13 A  Cj0=480 pF  Tprm=ee.enum.temperatureParameterization.none  etabet=1.3  Stvfb=5e-4 V/K  Stphib=-8.5e-4 V/K  etasat=1.04  etasr=0.65  etar=0.95  etais=3  Tsim=25 degC  Ig_specify=off  Ig_priority=None  Ig=0 A  Ig_nominal_specify=off  Ig_nominal_value=1  Ig_nominal_unit=nA  Ids_specify=off  Ids_priority=None  Ids=0 A  Ids_nominal_specify=off  Ids_nominal_value=1  Ids_nominal_unit=A  Ib_specify=off  Ib_priority=None  Ib=0 A  Ib_nominal_specify=off  Ib_nominal_value=1  Ib_nominal_unit=uA  V_gs_specify=off  V_gs_priority=None  V_gs=0 V  V_gs_nominal_specify=off  V_gs_nominal_value=1  V_gs_nominal_unit=V  V_ds_specify=off  V_ds_priority=None  V_ds=0 V  V_ds_nominal_specify=off  V_ds_nominal_value=1  V_ds_nominal_unit=V  V_bs_specify=off  V_bs_priority=None  V_bs=0 V  V_bs_nominal_specify=off  V_bs_nominal_value=1  V_bs_nominal_unit=V  QGoverCox_specify=off  QGoverCox_priority=None  QGoverCox=0 V  QGoverCox_nominal_specify=off  QGoverCox_nominal_value=1  QGoverCox_nominal_unit=V  QDoverCox_specify=off  QDoverCox_priority=None  QDoverCox=0 V  QDoverCox_nominal_specify=off  QDoverCox_nominal_value=1  QDoverCox_nominal_unit=V  QBoverCox_specify=off  QBoverCox_priority=None  QBoverCox=0 V  QBoverCox_nominal_specify=off  QBoverCox_nominal_value=1  QBoverCox_nominal_unit=V  T0=[25, 25] degC  T0_Cauer=[25, 25, 25] degC
      | この回路での名前　　; Q2
      | 部品名　　　　　　　; TK9R6E15Q5,S1X
      | この回路での役割　　; 上側スイッチQ1がOFFの間にも、L1の電流が流れ続ける経路を作る下側スイッチ。
      | ここでの動き　　　　; ゲートドライバU9でON/OFFする。ダイオードの代わりに低い抵抗で電流を通す同期整流を担い、Q1との同時ONを避ける制御を必要とする。
      | 
      | 【詳しい働き・仕様・接続・確認の範囲】
      | 部品種別　　　　　　; 下側NチャネルMOSFET
      | 公称値　　　　　　　; TK9R6E15Q5,S1X
      | 配置目的　　　　　　; 同期整流降圧回路の下側スイッチ。Q1 OFF期間にL1電流の経路を作り、ダイオードだけの場合の導通損失を減らす。
      | 意図する動作　　　　; U9からR43を介して駆動。Q1とのデッドタイム、逆電流・軽負荷時の扱いは制御条件に依存する。
      | 端子と接続　　　　　; 3 S → GND、1 G → GATE_L、2 D → SW
      | モデルの範囲　　　　; Simscape標準NチャネルMOSFETの近似。掲載型番の全特性へ同定済みではなく、設定値とメーカー定格を区別する。Idはモデル校正用電流で最大許容電流ではない。
      | モデル設定　　　　　; Rds=25 mΩ、Vgs=10 V、Id=6 A、Vth=1.7 V、LeadRg=0 Ω。これらは保存モデルの設定値であり、すべてが実部品の保証値という意味ではない。
      | 確認の範囲　　　　　; 本説明は保存回路の部品情報・端子割当・既存設計意図を整理したもの。今回の説明更新によって新たな動作試験や実機検証を実施した意味ではない。
      | 設計記録　　　　　　; evaluation\component_annotations_20261022_r01\before_graph.json
      | evaluation\component_annotations_20261022_r01\before_metadata.json
      | evaluation\protection_capacitor_integration_20261021_r01\final_delivery\independent_readback\physical_bom.json
      | 
      | 【この説明欄の略語・記号】
      | 用語1　　　　　　　 ; MOSFET：Metal-Oxide-Semiconductor Field-Effect Transistor（金属・酸化膜・半導体構造の電界効果トランジスタ）。ゲートとソースの電圧でドレインとソースの導通を制御する素子。N-MOSはNチャネル型を表す。
      | 用語2　　　　　　　 ; VGS：Gate-to-Source Voltage（ゲート・ソース間電圧）。ゲートの電圧をソース基準で表す。GND基準のゲート電圧とは同じとは限らない。
      | 用語3　　　　　　　 ; Rds：Drain-to-Source On-Resistance（導通時のドレイン・ソース間抵抗）。十分にONにした条件での抵抗。温度やゲート電圧などの条件に依存する。
      | 用語4　　　　　　　 ; Vth：Threshold Voltage（しきい値電圧）。MOSFETが指定された小電流を流し始めるゲート電圧の目安。十分にONにする駆動電圧ではない。
      | 用語5　　　　　　　 ; ID：Drain Current（ドレイン電流）。MOSFETのドレインを流れる電流。Idというモデル設定値は校正条件である場合があり、最大電流定格とは区別する。
      | 用語6　　　　　　　 ; LeadRg：Gate lead resistance（モデル内のゲート側直列抵抗パラメータ）。このモデルで内部ゲート抵抗をまとめて与える設定名。パッケージのリード単独の抵抗という保証値ではない。
      | 用語7　　　　　　　 ; GND：Ground（回路の基準電位・電流帰路）。この図の共通基準。保護接地や大地への接続を意味するとは限らない。
      | 用語8　　　　　　　 ; SW：Switching Node（スイッチング点）。主電力段の上下MOSFETとL1がつながる、電圧が高速に切り替わる点。GNDとは別電位。
      settings: AttributesFormatString=N-MOS 同期整流
  Q3A : ee_lib/Semiconductors & Converters/N-Channel MOSFET  Description=|  paramTerminal=ee.enum.mosfet.numberOfTerminals.three  parameterization=ee.enum.mosfet.parameterization.datasheet  Beta=5.0 A/V^2  Rds=0.025 Ohm  Id=6.0 A  Vgs=10 V  Vth=1.7 V  Vth0=1.7 V  lam=0 1/V  gamma_vth=0.5 V^(1/2)  phib=0.5 V  Vth1=1.9071 V  Vbs1=-1 V  Vth2=2.066 V  Vbs2=-2 V  Tmeas=25 degC  Vgs_vec=[-1, -.5, 2, 3, 4, 5] V  Vds_vec=[0, 2, 4, 8, 12, 16, 20] V  Vbs_vec=[0, -4, -6, -12] V  T_vec=[25, 125] degC  Vth_vec=[.4, 1.2, 1.4, 1.45] V  Vth_mat=[.4, .35; 1.2, 1.15; 1.4, 1.35; 1.45, 1.4] V  Ids_mat=[0, 0, 0, 0, 0, 0, 0; 0, 0, 0, 0, 0, 0, 0; 0, .003, .0038, .0043, .0046, .0048, .0049; 0, .0055, .008, .009, .0095, .01, .0101; 0, .0115, .016, .018, .019, .0195, .02; 0, .0152, .0225, .0265, .028, .0295, .03] A  Ids_mat0=[0, 0, 0, 0, 0, 0, 0; 0, 0, 0, 0, 0, 0, 0; 0, .003, .0038, .0043, .0046, .0048, .0049; 0, .0055, .008, .009, .0095, .01, .0101; 0, .0115, .016, .018, .019, .0195, .02; 0, .0152, .0225, .0265, .028, .0295, .03] A  Ids_mat_3D=zeros(6, 7, 2) A  Ids_mat_3D0=zeros(6, 7, 2) A  IV_table_symmetry=ee.enum.mosfet.symmetricNIV.no  RS=0.0001 Ohm  RD=0.01 Ohm  RB=0.001 Ohm  LeadRs=0 Ohm  LeadRd=0 Ohm  LeadRg=0 Ohm  LeadRb=0 Ohm  LS=0 nH  LD=0 nH  LG=0 nH  LB=0 nH  C_param=ee.enum.mosfet.capacitanceParam.fixedciss  C_GS=270 pF  C_GD=80 pF  C_GB=0 pF  C_DS=0 pF  C_iss=350 pF  C_rss=80 pF  C_oss=0 pF  C_iss_vec=[720, 700, 590, 470, 390, 310] pF  C_rss_vec=[450, 400, 300, 190, 95, 55] pF  C_oss_vec=[900, 810, 690, 420, 270, 170] pF  C_GS_vec=[270, 300, 290, 280, 295, 255] pF  C_GD_vec=[450, 400, 300, 190, 95, 55] pF  C_GB_vec=[270, 300, 290, 280, 295, 255] pF  C_Vgs_vec=0 V  C_DS_vec=[450, 410, 390, 230, 175, 115] pF  C_Vds_vec=[.1, .3, 1, 3, 10, 30] V  V_GS_for_cap_data=0 V  charge_linearity_param=ee.enum.mosfet.cgdLinearity.constant  C_OX=200 pF  V_C_OX=-0.5 V  charge_linearity_param_vgb=ee.enum.mosfet.cgbLinearity.instantly  charge_linearity_param_with_vgb=ee.enum.mosfet.cgbLinearityWithSeparateCgb.instantly  Di_param=ee.enum.mosfet.diodeParam.no  IsDiode=1e-12 A  Vbi=0.6 V  n=1  Cj0Diode=0 pF  TT=50e-9 s  Tmeas_dio=25 degC  TableTypeNoT=ee.enum.mosfet.tableType.IfMat  TableType=ee.enum.diode.tableType.IfMat  IfVec=[.07, .12, .19, 1.75, 4.24, 7.32, 11.2] A  IfMat=[.07, .12, .19, 1.75, 4.24, 7.32, 11.2; .16, .3, .72, 2.14, 4.02, 6.35, 9.12] A  VfVecV=[.9, 1.15, 1.25, 1.5, 1.75, 2.17, 2.6, 2.85] V  VfMatV=[.9, 1.15, 1.25, 1.5, 1.75, 2.17, 2.6, 2.85; .58, .68, .75, 1.1, 1.38, 1.77, 2.27, 2.7] V  TjVec=[25, 125] degC  VfVec=[.5, .7, .9, 1.3, 1.7, 2.1, 2.5] V  IfVecV=[.1, .2, .5, 1, 2, 4, 7, 10] A  diode_Goff=1e-12 1/Ohm  prmDatasheet=ee.enum.temperatureParameterization.none  prmEquCoeff=ee.enum.temperatureParameterization.none  dVth_dT=-6 mV/K  dVth0_dT=-6 mV/K  Rds_T2=0.037 Ohm  BEXDatasheet=-1.5  BEXEquCoeff=-1.5  etaisDatasheet=3  etaisEquCoeff=3  Tmeas2=125 degC  etaisTabulated=3  TdeviceDatasheet=25 degC  TdeviceEquCoeff=25 degC  TdeviceTabulated=25 degC  i_g_specify=off  i_g_priority=None  i_g=0 A  i_g_nominal_specify=off  i_g_nominal_value=1  i_g_nominal_unit=A  i_d_specify=off  i_d_priority=None  i_d=0 A  i_d_nominal_specify=off  i_d_nominal_value=1  i_d_nominal_unit=A  i_b_specify=off  i_b_priority=None  i_b=0 A  i_b_nominal_specify=off  i_b_nominal_value=1  i_b_nominal_unit=A  voltage_gs_specify=off  voltage_gs_priority=None  voltage_gs=0 V  voltage_gs_nominal_specify=off  voltage_gs_nominal_value=1  voltage_gs_nominal_unit=V  voltage_ds_specify=off  voltage_ds_priority=None  voltage_ds=0 V  voltage_ds_nominal_specify=off  voltage_ds_nominal_value=1  voltage_ds_nominal_unit=V  voltage_bs_specify=off  voltage_bs_priority=None  voltage_bs=0 V  voltage_bs_nominal_specify=off  voltage_bs_nominal_value=1  voltage_bs_nominal_unit=V  v_Cgs_specify=off  v_Cgs_priority=High  v_Cgs=0 V  v_Cgs_nominal_specify=off  v_Cgs_nominal_value=1  v_Cgs_nominal_unit=V  v_Cds_specify=off  v_Cds_priority=High  v_Cds=0 V  v_Cds_nominal_specify=off  v_Cds_nominal_value=1  v_Cds_nominal_unit=V  v_Cbs_specify=off  v_Cbs_priority=High  v_Cbs=0 V  v_Cbs_nominal_specify=off  v_Cbs_nominal_value=1  v_Cbs_nominal_unit=V  thermal_network_parameterization=ee.enum.thermalNetworkTopology.junctionCase  Rth=[0, 10] K/W  Rth_Cauer=[1, 3, 10] K/W  Rth_Foster=[.08, .14, .22, .16] K/W  thermal_mass_parameterization=ee.enum.thermalNetwork.timeconstant  thermal_mass=[0, 1] J/K  thermal_mass_Cauer=[.1, .3, 1] J/K  thermal_mass_Foster=[.001, .005, .05, .5] J/K  thermal_time_constant=[0, 10] s  thermal_time_constant_Cauer=[1, 3, 10] s  thermal_time_constant_Foster=[7e-05, .0007, .01, .08] s  thermal_mass_initial_temperatures=[25, 25] degC  thermal_mass_initial_temperatures_Cauer=[25, 25, 25] degC  Tvec_initial_Foster=[25, 25, 25, 25] degC  betaref=18 A/V^2  Vfbref=-1.1 V  gamma=3.5 V^(1/2)  phib2ref=1 V  thesatref=0.4 1/V  alpha=0  Vp=5e-2 V  thesrref=0 1/V  m=8  Tref=25 degC  Rsref=2e-3 Ohm  Rdref=0.17 Ohm  Rgref=8.4 Ohm  Rbref=2e-3 Ohm  Cox=1500 pF  Cgso=100 pF  Cgdo=14 pF  Isref=5.2e-13 A  Cj0=480 pF  Tprm=ee.enum.temperatureParameterization.none  etabet=1.3  Stvfb=5e-4 V/K  Stphib=-8.5e-4 V/K  etasat=1.04  etasr=0.65  etar=0.95  etais=3  Tsim=25 degC  Ig_specify=off  Ig_priority=None  Ig=0 A  Ig_nominal_specify=off  Ig_nominal_value=1  Ig_nominal_unit=nA  Ids_specify=off  Ids_priority=None  Ids=0 A  Ids_nominal_specify=off  Ids_nominal_value=1  Ids_nominal_unit=A  Ib_specify=off  Ib_priority=None  Ib=0 A  Ib_nominal_specify=off  Ib_nominal_value=1  Ib_nominal_unit=uA  V_gs_specify=off  V_gs_priority=None  V_gs=0 V  V_gs_nominal_specify=off  V_gs_nominal_value=1  V_gs_nominal_unit=V  V_ds_specify=off  V_ds_priority=None  V_ds=0 V  V_ds_nominal_specify=off  V_ds_nominal_value=1  V_ds_nominal_unit=V  V_bs_specify=off  V_bs_priority=None  V_bs=0 V  V_bs_nominal_specify=off  V_bs_nominal_value=1  V_bs_nominal_unit=V  QGoverCox_specify=off  QGoverCox_priority=None  QGoverCox=0 V  QGoverCox_nominal_specify=off  QGoverCox_nominal_value=1  QGoverCox_nominal_unit=V  QDoverCox_specify=off  QDoverCox_priority=None  QDoverCox=0 V  QDoverCox_nominal_specify=off  QDoverCox_nominal_value=1  QDoverCox_nominal_unit=V  QBoverCox_specify=off  QBoverCox_priority=None  QBoverCox=0 V  QBoverCox_nominal_specify=off  QBoverCox_nominal_value=1  QBoverCox_nominal_unit=V  T0=[25, 25] degC  T0_Cauer=[25, 25, 25] degC
      | この回路での名前　　; Q3A
      | 部品名　　　　　　　; PMGD175XNEX
      | この回路での役割　　; 上側ゲートドライバU8の内部発光素子を、マイコンの信号で点滅させる小型スイッチ。
      | ここでの動き　　　　; マイコンの上側指令に応じて発光素子の電流をGNDへ流す。Q3Bと同じ1個の部品に入っている別の素子で、充電用の主電流は流さない。
      | 
      | 【詳しい働き・仕様・接続・確認の範囲】
      | 識別の補足　　　　　; Q3A（同じQ3パッケージ内の素子）
      | 部品種別　　　　　　; デュアルMOSFETの上側ドライバLED駆動素子
      | 公称値　　　　　　　; dual 30V logic-level LED sink
      | 配置目的　　　　　　; RP2040のPWM_Hを受け、U8の入力LED電流をGNDへ引き込む。
      | 意図する動作　　　　; Q3Bと同じPMGD175XNEXパッケージ内の別素子。主電力を直接スイッチングするQ1とは役割が異なる。
      | 端子と接続　　　　　; 1 S1 → GND、2 G1 → H_LED_GATE、6 D1 → H_LED_SINK
      | モデルの範囲　　　　; Simscape標準NチャネルMOSFETの近似。掲載型番の全特性へ同定済みではなく、設定値とメーカー定格を区別する。Idはモデル校正用電流で最大許容電流ではない。
      | モデル設定　　　　　; Rds=25 mΩ、Vgs=10 V、Id=6 A、Vth=1.7 V、LeadRg=0 Ω。これらは保存モデルの設定値であり、すべてが実部品の保証値という意味ではない。
      | 確認の範囲　　　　　; 本説明は保存回路の部品情報・端子割当・既存設計意図を整理したもの。今回の説明更新によって新たな動作試験や実機検証を実施した意味ではない。
      | 設計記録　　　　　　; evaluation\component_annotations_20261022_r01\before_graph.json
      | evaluation\component_annotations_20261022_r01\before_metadata.json
      | evaluation\protection_capacitor_integration_20261021_r01\final_delivery\independent_readback\physical_bom.json
      | 
      | 【この説明欄の略語・記号】
      | 用語1　　　　　　　 ; PWM：Pulse Width Modulation（パルス幅変調）。周期に対するON時間の割合を変えて、スイッチの平均的な電力伝達を調整する方式。
      | 用語2　　　　　　　 ; MOSFET：Metal-Oxide-Semiconductor Field-Effect Transistor（金属・酸化膜・半導体構造の電界効果トランジスタ）。ゲートとソースの電圧でドレインとソースの導通を制御する素子。N-MOSはNチャネル型を表す。
      | 用語3　　　　　　　 ; VGS：Gate-to-Source Voltage（ゲート・ソース間電圧）。ゲートの電圧をソース基準で表す。GND基準のゲート電圧とは同じとは限らない。
      | 用語4　　　　　　　 ; Rds：Drain-to-Source On-Resistance（導通時のドレイン・ソース間抵抗）。十分にONにした条件での抵抗。温度やゲート電圧などの条件に依存する。
      | 用語5　　　　　　　 ; Vth：Threshold Voltage（しきい値電圧）。MOSFETが指定された小電流を流し始めるゲート電圧の目安。十分にONにする駆動電圧ではない。
      | 用語6　　　　　　　 ; ID：Drain Current（ドレイン電流）。MOSFETのドレインを流れる電流。Idというモデル設定値は校正条件である場合があり、最大電流定格とは区別する。
      | 用語7　　　　　　　 ; LeadRg：Gate lead resistance（モデル内のゲート側直列抵抗パラメータ）。このモデルで内部ゲート抵抗をまとめて与える設定名。パッケージのリード単独の抵抗という保証値ではない。
      | 用語8　　　　　　　 ; LED：Light-Emitting Diode（発光ダイオード）。本回路のゲートドライバ入力では光によって信号を伝え、入力側と出力側を絶縁するために用いる。
      | 用語9　　　　　　　 ; GND：Ground（回路の基準電位・電流帰路）。この図の共通基準。保護接地や大地への接続を意味するとは限らない。
      settings: AttributesFormatString=N-MOS LED駆動 A
  Q3B : ee_lib/Semiconductors & Converters/N-Channel MOSFET  Description=|  paramTerminal=ee.enum.mosfet.numberOfTerminals.three  parameterization=ee.enum.mosfet.parameterization.datasheet  Beta=5.0 A/V^2  Rds=0.025 Ohm  Id=6.0 A  Vgs=10 V  Vth=1.7 V  Vth0=1.7 V  lam=0 1/V  gamma_vth=0.5 V^(1/2)  phib=0.5 V  Vth1=1.9071 V  Vbs1=-1 V  Vth2=2.066 V  Vbs2=-2 V  Tmeas=25 degC  Vgs_vec=[-1, -.5, 2, 3, 4, 5] V  Vds_vec=[0, 2, 4, 8, 12, 16, 20] V  Vbs_vec=[0, -4, -6, -12] V  T_vec=[25, 125] degC  Vth_vec=[.4, 1.2, 1.4, 1.45] V  Vth_mat=[.4, .35; 1.2, 1.15; 1.4, 1.35; 1.45, 1.4] V  Ids_mat=[0, 0, 0, 0, 0, 0, 0; 0, 0, 0, 0, 0, 0, 0; 0, .003, .0038, .0043, .0046, .0048, .0049; 0, .0055, .008, .009, .0095, .01, .0101; 0, .0115, .016, .018, .019, .0195, .02; 0, .0152, .0225, .0265, .028, .0295, .03] A  Ids_mat0=[0, 0, 0, 0, 0, 0, 0; 0, 0, 0, 0, 0, 0, 0; 0, .003, .0038, .0043, .0046, .0048, .0049; 0, .0055, .008, .009, .0095, .01, .0101; 0, .0115, .016, .018, .019, .0195, .02; 0, .0152, .0225, .0265, .028, .0295, .03] A  Ids_mat_3D=zeros(6, 7, 2) A  Ids_mat_3D0=zeros(6, 7, 2) A  IV_table_symmetry=ee.enum.mosfet.symmetricNIV.no  RS=0.0001 Ohm  RD=0.01 Ohm  RB=0.001 Ohm  LeadRs=0 Ohm  LeadRd=0 Ohm  LeadRg=0 Ohm  LeadRb=0 Ohm  LS=0 nH  LD=0 nH  LG=0 nH  LB=0 nH  C_param=ee.enum.mosfet.capacitanceParam.fixedciss  C_GS=270 pF  C_GD=80 pF  C_GB=0 pF  C_DS=0 pF  C_iss=350 pF  C_rss=80 pF  C_oss=0 pF  C_iss_vec=[720, 700, 590, 470, 390, 310] pF  C_rss_vec=[450, 400, 300, 190, 95, 55] pF  C_oss_vec=[900, 810, 690, 420, 270, 170] pF  C_GS_vec=[270, 300, 290, 280, 295, 255] pF  C_GD_vec=[450, 400, 300, 190, 95, 55] pF  C_GB_vec=[270, 300, 290, 280, 295, 255] pF  C_Vgs_vec=0 V  C_DS_vec=[450, 410, 390, 230, 175, 115] pF  C_Vds_vec=[.1, .3, 1, 3, 10, 30] V  V_GS_for_cap_data=0 V  charge_linearity_param=ee.enum.mosfet.cgdLinearity.constant  C_OX=200 pF  V_C_OX=-0.5 V  charge_linearity_param_vgb=ee.enum.mosfet.cgbLinearity.instantly  charge_linearity_param_with_vgb=ee.enum.mosfet.cgbLinearityWithSeparateCgb.instantly  Di_param=ee.enum.mosfet.diodeParam.no  IsDiode=1e-12 A  Vbi=0.6 V  n=1  Cj0Diode=0 pF  TT=50e-9 s  Tmeas_dio=25 degC  TableTypeNoT=ee.enum.mosfet.tableType.IfMat  TableType=ee.enum.diode.tableType.IfMat  IfVec=[.07, .12, .19, 1.75, 4.24, 7.32, 11.2] A  IfMat=[.07, .12, .19, 1.75, 4.24, 7.32, 11.2; .16, .3, .72, 2.14, 4.02, 6.35, 9.12] A  VfVecV=[.9, 1.15, 1.25, 1.5, 1.75, 2.17, 2.6, 2.85] V  VfMatV=[.9, 1.15, 1.25, 1.5, 1.75, 2.17, 2.6, 2.85; .58, .68, .75, 1.1, 1.38, 1.77, 2.27, 2.7] V  TjVec=[25, 125] degC  VfVec=[.5, .7, .9, 1.3, 1.7, 2.1, 2.5] V  IfVecV=[.1, .2, .5, 1, 2, 4, 7, 10] A  diode_Goff=1e-12 1/Ohm  prmDatasheet=ee.enum.temperatureParameterization.none  prmEquCoeff=ee.enum.temperatureParameterization.none  dVth_dT=-6 mV/K  dVth0_dT=-6 mV/K  Rds_T2=0.037 Ohm  BEXDatasheet=-1.5  BEXEquCoeff=-1.5  etaisDatasheet=3  etaisEquCoeff=3  Tmeas2=125 degC  etaisTabulated=3  TdeviceDatasheet=25 degC  TdeviceEquCoeff=25 degC  TdeviceTabulated=25 degC  i_g_specify=off  i_g_priority=None  i_g=0 A  i_g_nominal_specify=off  i_g_nominal_value=1  i_g_nominal_unit=A  i_d_specify=off  i_d_priority=None  i_d=0 A  i_d_nominal_specify=off  i_d_nominal_value=1  i_d_nominal_unit=A  i_b_specify=off  i_b_priority=None  i_b=0 A  i_b_nominal_specify=off  i_b_nominal_value=1  i_b_nominal_unit=A  voltage_gs_specify=off  voltage_gs_priority=None  voltage_gs=0 V  voltage_gs_nominal_specify=off  voltage_gs_nominal_value=1  voltage_gs_nominal_unit=V  voltage_ds_specify=off  voltage_ds_priority=None  voltage_ds=0 V  voltage_ds_nominal_specify=off  voltage_ds_nominal_value=1  voltage_ds_nominal_unit=V  voltage_bs_specify=off  voltage_bs_priority=None  voltage_bs=0 V  voltage_bs_nominal_specify=off  voltage_bs_nominal_value=1  voltage_bs_nominal_unit=V  v_Cgs_specify=off  v_Cgs_priority=High  v_Cgs=0 V  v_Cgs_nominal_specify=off  v_Cgs_nominal_value=1  v_Cgs_nominal_unit=V  v_Cds_specify=off  v_Cds_priority=High  v_Cds=0 V  v_Cds_nominal_specify=off  v_Cds_nominal_value=1  v_Cds_nominal_unit=V  v_Cbs_specify=off  v_Cbs_priority=High  v_Cbs=0 V  v_Cbs_nominal_specify=off  v_Cbs_nominal_value=1  v_Cbs_nominal_unit=V  thermal_network_parameterization=ee.enum.thermalNetworkTopology.junctionCase  Rth=[0, 10] K/W  Rth_Cauer=[1, 3, 10] K/W  Rth_Foster=[.08, .14, .22, .16] K/W  thermal_mass_parameterization=ee.enum.thermalNetwork.timeconstant  thermal_mass=[0, 1] J/K  thermal_mass_Cauer=[.1, .3, 1] J/K  thermal_mass_Foster=[.001, .005, .05, .5] J/K  thermal_time_constant=[0, 10] s  thermal_time_constant_Cauer=[1, 3, 10] s  thermal_time_constant_Foster=[7e-05, .0007, .01, .08] s  thermal_mass_initial_temperatures=[25, 25] degC  thermal_mass_initial_temperatures_Cauer=[25, 25, 25] degC  Tvec_initial_Foster=[25, 25, 25, 25] degC  betaref=18 A/V^2  Vfbref=-1.1 V  gamma=3.5 V^(1/2)  phib2ref=1 V  thesatref=0.4 1/V  alpha=0  Vp=5e-2 V  thesrref=0 1/V  m=8  Tref=25 degC  Rsref=2e-3 Ohm  Rdref=0.17 Ohm  Rgref=8.4 Ohm  Rbref=2e-3 Ohm  Cox=1500 pF  Cgso=100 pF  Cgdo=14 pF  Isref=5.2e-13 A  Cj0=480 pF  Tprm=ee.enum.temperatureParameterization.none  etabet=1.3  Stvfb=5e-4 V/K  Stphib=-8.5e-4 V/K  etasat=1.04  etasr=0.65  etar=0.95  etais=3  Tsim=25 degC  Ig_specify=off  Ig_priority=None  Ig=0 A  Ig_nominal_specify=off  Ig_nominal_value=1  Ig_nominal_unit=nA  Ids_specify=off  Ids_priority=None  Ids=0 A  Ids_nominal_specify=off  Ids_nominal_value=1  Ids_nominal_unit=A  Ib_specify=off  Ib_priority=None  Ib=0 A  Ib_nominal_specify=off  Ib_nominal_value=1  Ib_nominal_unit=uA  V_gs_specify=off  V_gs_priority=None  V_gs=0 V  V_gs_nominal_specify=off  V_gs_nominal_value=1  V_gs_nominal_unit=V  V_ds_specify=off  V_ds_priority=None  V_ds=0 V  V_ds_nominal_specify=off  V_ds_nominal_value=1  V_ds_nominal_unit=V  V_bs_specify=off  V_bs_priority=None  V_bs=0 V  V_bs_nominal_specify=off  V_bs_nominal_value=1  V_bs_nominal_unit=V  QGoverCox_specify=off  QGoverCox_priority=None  QGoverCox=0 V  QGoverCox_nominal_specify=off  QGoverCox_nominal_value=1  QGoverCox_nominal_unit=V  QDoverCox_specify=off  QDoverCox_priority=None  QDoverCox=0 V  QDoverCox_nominal_specify=off  QDoverCox_nominal_value=1  QDoverCox_nominal_unit=V  QBoverCox_specify=off  QBoverCox_priority=None  QBoverCox=0 V  QBoverCox_nominal_specify=off  QBoverCox_nominal_value=1  QBoverCox_nominal_unit=V  T0=[25, 25] degC  T0_Cauer=[25, 25, 25] degC
      | この回路での名前　　; Q3B
      | 部品名　　　　　　　; PMGD175XNEX
      | この回路での役割　　; 下側ゲートドライバU9の内部発光素子を、マイコンの信号で点滅させる小型スイッチ。
      | ここでの動き　　　　; マイコンの下側指令に応じて発光素子の電流をGNDへ流す。Q3Aと同じ1個の部品に入っている別の素子で、上下の指令を別々に扱う。
      | 
      | 【詳しい働き・仕様・接続・確認の範囲】
      | 識別の補足　　　　　; Q3B（同じQ3パッケージ内の素子）
      | 部品種別　　　　　　; デュアルMOSFETの下側ドライバLED駆動素子
      | 公称値　　　　　　　; dual 30V logic-level LED sink
      | 配置目的　　　　　　; RP2040のPWM_Lを受け、U9の入力LED電流をGNDへ引き込む。
      | 意図する動作　　　　; Q3Aと同じPMGD175XNEXパッケージ内の別素子。ゲートのプルダウンで未駆動時の状態を定める。
      | 端子と接続　　　　　; 3 D2 → L_LED_SINK、4 S2 → GND、5 G2 → L_LED_GATE
      | モデルの範囲　　　　; Simscape標準NチャネルMOSFETの近似。掲載型番の全特性へ同定済みではなく、設定値とメーカー定格を区別する。Idはモデル校正用電流で最大許容電流ではない。
      | モデル設定　　　　　; Rds=25 mΩ、Vgs=10 V、Id=6 A、Vth=1.7 V、LeadRg=0 Ω。これらは保存モデルの設定値であり、すべてが実部品の保証値という意味ではない。
      | 確認の範囲　　　　　; 本説明は保存回路の部品情報・端子割当・既存設計意図を整理したもの。今回の説明更新によって新たな動作試験や実機検証を実施した意味ではない。
      | 設計記録　　　　　　; evaluation\component_annotations_20261022_r01\before_graph.json
      | evaluation\component_annotations_20261022_r01\before_metadata.json
      | evaluation\protection_capacitor_integration_20261021_r01\final_delivery\independent_readback\physical_bom.json
      | 
      | 【この説明欄の略語・記号】
      | 用語1　　　　　　　 ; PWM：Pulse Width Modulation（パルス幅変調）。周期に対するON時間の割合を変えて、スイッチの平均的な電力伝達を調整する方式。
      | 用語2　　　　　　　 ; MOSFET：Metal-Oxide-Semiconductor Field-Effect Transistor（金属・酸化膜・半導体構造の電界効果トランジスタ）。ゲートとソースの電圧でドレインとソースの導通を制御する素子。N-MOSはNチャネル型を表す。
      | 用語3　　　　　　　 ; VGS：Gate-to-Source Voltage（ゲート・ソース間電圧）。ゲートの電圧をソース基準で表す。GND基準のゲート電圧とは同じとは限らない。
      | 用語4　　　　　　　 ; Rds：Drain-to-Source On-Resistance（導通時のドレイン・ソース間抵抗）。十分にONにした条件での抵抗。温度やゲート電圧などの条件に依存する。
      | 用語5　　　　　　　 ; Vth：Threshold Voltage（しきい値電圧）。MOSFETが指定された小電流を流し始めるゲート電圧の目安。十分にONにする駆動電圧ではない。
      | 用語6　　　　　　　 ; ID：Drain Current（ドレイン電流）。MOSFETのドレインを流れる電流。Idというモデル設定値は校正条件である場合があり、最大電流定格とは区別する。
      | 用語7　　　　　　　 ; LeadRg：Gate lead resistance（モデル内のゲート側直列抵抗パラメータ）。このモデルで内部ゲート抵抗をまとめて与える設定名。パッケージのリード単独の抵抗という保証値ではない。
      | 用語8　　　　　　　 ; LED：Light-Emitting Diode（発光ダイオード）。本回路のゲートドライバ入力では光によって信号を伝え、入力側と出力側を絶縁するために用いる。
      | 用語9　　　　　　　 ; GND：Ground（回路の基準電位・電流帰路）。この図の共通基準。保護接地や大地への接続を意味するとは限らない。
      settings: AttributesFormatString=N-MOS LED駆動 B
  R1 : fl_lib/Electrical/Electrical Elements/Resistor  Description=|  R=15000 Ohm  i_specify=off  i_priority=None  i=0 A  i_nominal_specify=off  i_nominal_value=1  i_nominal_unit=A  v_specify=off  v_priority=None  v=0 V  v_nominal_specify=off  v_nominal_value=1  v_nominal_unit=V
      | この回路での名前　　; R1
      | 部品名　　　　　　　; PR02000201502FA100
      | この回路での役割　　; 充電器の入力コンデンサに残った電荷を、電源を切った後に少しずつ抜くための抵抗。
      | ここでの動き　　　　; 入力電圧がかかる場所から共通GNDへ、小さな電流の通り道を常に作る。蓄えた電気を熱として消費するため、通電中にも損失が出る。実際の放電時間はコンデンサの容量と最初の電圧で変わる。
      | 
      | 【詳しい働き・仕様・接続・確認の範囲】
      | 部品種別　　　　　　; 入力コンデンサ放電抵抗
      | 公称値　　　　　　　; 15 kohm
      | 配置目的　　　　　　; VIN–GND間へ常時接続し、入力側コンデンサの電荷を徐々に放電する。
      | 意図する動作　　　　; 通電時は常時損失が発生する。放電時間は合成容量・初期電圧に依存し、感電防止の保証時間は未確定。
      | 端子と接続　　　　　; 2 n → GND、1 p → VIN
      | モデルの範囲　　　　; Simscape抵抗の集中定数表現。部品の許容差、定格電力、温度係数、寄生インダクタンスの適合を示すものではない。
      | モデル設定　　　　　; R=15 kΩ。これらは保存モデルの設定値であり、すべてが実部品の保証値という意味ではない。
      | 確認の範囲　　　　　; 本説明は保存回路の部品情報・端子割当・既存設計意図を整理したもの。今回の説明更新によって新たな動作試験や実機検証を実施した意味ではない。
      | 設計記録　　　　　　; evaluation\component_annotations_20261022_r01\before_graph.json
      | evaluation\component_annotations_20261022_r01\before_metadata.json
      | evaluation\protection_capacitor_integration_20261021_r01\final_delivery\independent_readback\physical_bom.json
      | 
      | 【この説明欄の略語・記号】
      | 用語1　　　　　　　 ; GND：Ground（回路の基準電位・電流帰路）。この図の共通基準。保護接地や大地への接続を意味するとは限らない。
      | 用語2　　　　　　　 ; VIN/VOUT：入力電圧・出力電圧を表す端子／ネット名。INは入力、OUTは出力。電源変換器の電力端子なのか、検出用端子なのかは対象部品によって異なるため、端子と接続の説明に従う。
      settings: AttributesFormatString=15 kΩ
  R10 : fl_lib/Electrical/Electrical Elements/Resistor  Description=|  R=4.42 Ohm  i_specify=off  i_priority=None  i=0 A  i_nominal_specify=off  i_nominal_value=1  i_nominal_unit=A  v_specify=off  v_priority=None  v=0 V  v_nominal_specify=off  v_nominal_value=1  v_nominal_unit=V
      | この回路での名前　　; R10
      | 部品名　　　　　　　; CRCW25124R42FKEGHP
      | この回路での役割　　; 主電力MOSFET Q1・Q2の切替え時に生じる、電圧の振動を弱めるためのスナバ抵抗。
      | ここでの動き　　　　; C1と組み合わせ、切替え時の振動エネルギーを熱として消費する。R9と直列の一組になり、同じ二個直列の枝を六組並列にして抵抗値と電力負担を分ける。実際の減衰量・パルス電力・温度は別途確認する。
      | 
      | 【詳しい働き・仕様・接続・確認の範囲】
      | 部品種別　　　　　　; スナバ抵抗
      | 公称値　　　　　　　; 4.42 ohm
      | 配置目的　　　　　　; Q1/Q2のSWノードからC1へつながるスナバ抵抗網の一部。R3〜R14は2個直列の枝を6本並列にした構成。
      | 意図する動作　　　　; スイッチング時の振動エネルギーを抵抗で消費する意図。個々のパルス電力・温度・配置寄生は別途確認する。
      | 端子と接続　　　　　; 2 n → SNUB_C、1 p → SNUB_MID_4
      | モデルの範囲　　　　; Simscape抵抗の集中定数表現。部品の許容差、定格電力、温度係数、寄生インダクタンスの適合を示すものではない。
      | モデル設定　　　　　; R=4.42 Ω。これらは保存モデルの設定値であり、すべてが実部品の保証値という意味ではない。
      | 確認の範囲　　　　　; 本説明は保存回路の部品情報・端子割当・既存設計意図を整理したもの。今回の説明更新によって新たな動作試験や実機検証を実施した意味ではない。
      | 設計記録　　　　　　; evaluation\component_annotations_20261022_r01\before_graph.json
      | evaluation\component_annotations_20261022_r01\before_metadata.json
      | evaluation\protection_capacitor_integration_20261021_r01\final_delivery\independent_readback\physical_bom.json
      | 
      | 【この説明欄の略語・記号】
      | 用語1　　　　　　　 ; MOSFET：Metal-Oxide-Semiconductor Field-Effect Transistor（金属・酸化膜・半導体構造の電界効果トランジスタ）。ゲートとソースの電圧でドレインとソースの導通を制御する素子。N-MOSはNチャネル型を表す。
      | 用語2　　　　　　　 ; GND：Ground（回路の基準電位・電流帰路）。この図の共通基準。保護接地や大地への接続を意味するとは限らない。
      | 用語3　　　　　　　 ; SW：Switching Node（スイッチング点）。主電力段の上下MOSFETとL1がつながる、電圧が高速に切り替わる点。GNDとは別電位。
      settings: AttributesFormatString=4.42 Ω
  R11 : fl_lib/Electrical/Electrical Elements/Resistor  Description=|  R=4.42 Ohm  i_specify=off  i_priority=None  i=0 A  i_nominal_specify=off  i_nominal_value=1  i_nominal_unit=A  v_specify=off  v_priority=None  v=0 V  v_nominal_specify=off  v_nominal_value=1  v_nominal_unit=V
      | この回路での名前　　; R11
      | 部品名　　　　　　　; CRCW25124R42FKEGHP
      | この回路での役割　　; 主電力MOSFET Q1・Q2の切替え時に生じる、電圧の振動を弱めるためのスナバ抵抗。
      | ここでの動き　　　　; C1と組み合わせ、切替え時の振動エネルギーを熱として消費する。R12と直列の一組になり、同じ二個直列の枝を六組並列にして抵抗値と電力負担を分ける。実際の減衰量・パルス電力・温度は別途確認する。
      | 
      | 【詳しい働き・仕様・接続・確認の範囲】
      | 部品種別　　　　　　; スナバ抵抗
      | 公称値　　　　　　　; 4.42 ohm
      | 配置目的　　　　　　; Q1/Q2のSWノードからC1へつながるスナバ抵抗網の一部。R3〜R14は2個直列の枝を6本並列にした構成。
      | 意図する動作　　　　; スイッチング時の振動エネルギーを抵抗で消費する意図。個々のパルス電力・温度・配置寄生は別途確認する。
      | 端子と接続　　　　　; 1 p → SW、2 n → SNUB_MID_5
      | モデルの範囲　　　　; Simscape抵抗の集中定数表現。部品の許容差、定格電力、温度係数、寄生インダクタンスの適合を示すものではない。
      | モデル設定　　　　　; R=4.42 Ω。これらは保存モデルの設定値であり、すべてが実部品の保証値という意味ではない。
      | 確認の範囲　　　　　; 本説明は保存回路の部品情報・端子割当・既存設計意図を整理したもの。今回の説明更新によって新たな動作試験や実機検証を実施した意味ではない。
      | 設計記録　　　　　　; evaluation\component_annotations_20261022_r01\before_graph.json
      | evaluation\component_annotations_20261022_r01\before_metadata.json
      | evaluation\protection_capacitor_integration_20261021_r01\final_delivery\independent_readback\physical_bom.json
      | 
      | 【この説明欄の略語・記号】
      | 用語1　　　　　　　 ; MOSFET：Metal-Oxide-Semiconductor Field-Effect Transistor（金属・酸化膜・半導体構造の電界効果トランジスタ）。ゲートとソースの電圧でドレインとソースの導通を制御する素子。N-MOSはNチャネル型を表す。
      | 用語2　　　　　　　 ; GND：Ground（回路の基準電位・電流帰路）。この図の共通基準。保護接地や大地への接続を意味するとは限らない。
      | 用語3　　　　　　　 ; SW：Switching Node（スイッチング点）。主電力段の上下MOSFETとL1がつながる、電圧が高速に切り替わる点。GNDとは別電位。
      settings: AttributesFormatString=4.42 Ω
  R12 : fl_lib/Electrical/Electrical Elements/Resistor  Description=|  R=4.42 Ohm  i_specify=off  i_priority=None  i=0 A  i_nominal_specify=off  i_nominal_value=1  i_nominal_unit=A  v_specify=off  v_priority=None  v=0 V  v_nominal_specify=off  v_nominal_value=1  v_nominal_unit=V
      | この回路での名前　　; R12
      | 部品名　　　　　　　; CRCW25124R42FKEGHP
      | この回路での役割　　; 主電力MOSFET Q1・Q2の切替え時に生じる、電圧の振動を弱めるためのスナバ抵抗。
      | ここでの動き　　　　; C1と組み合わせ、切替え時の振動エネルギーを熱として消費する。R11と直列の一組になり、同じ二個直列の枝を六組並列にして抵抗値と電力負担を分ける。実際の減衰量・パルス電力・温度は別途確認する。
      | 
      | 【詳しい働き・仕様・接続・確認の範囲】
      | 部品種別　　　　　　; スナバ抵抗
      | 公称値　　　　　　　; 4.42 ohm
      | 配置目的　　　　　　; Q1/Q2のSWノードからC1へつながるスナバ抵抗網の一部。R3〜R14は2個直列の枝を6本並列にした構成。
      | 意図する動作　　　　; スイッチング時の振動エネルギーを抵抗で消費する意図。個々のパルス電力・温度・配置寄生は別途確認する。
      | 端子と接続　　　　　; 2 n → SNUB_C、1 p → SNUB_MID_5
      | モデルの範囲　　　　; Simscape抵抗の集中定数表現。部品の許容差、定格電力、温度係数、寄生インダクタンスの適合を示すものではない。
      | モデル設定　　　　　; R=4.42 Ω。これらは保存モデルの設定値であり、すべてが実部品の保証値という意味ではない。
      | 確認の範囲　　　　　; 本説明は保存回路の部品情報・端子割当・既存設計意図を整理したもの。今回の説明更新によって新たな動作試験や実機検証を実施した意味ではない。
      | 設計記録　　　　　　; evaluation\component_annotations_20261022_r01\before_graph.json
      | evaluation\component_annotations_20261022_r01\before_metadata.json
      | evaluation\protection_capacitor_integration_20261021_r01\final_delivery\independent_readback\physical_bom.json
      | 
      | 【この説明欄の略語・記号】
      | 用語1　　　　　　　 ; MOSFET：Metal-Oxide-Semiconductor Field-Effect Transistor（金属・酸化膜・半導体構造の電界効果トランジスタ）。ゲートとソースの電圧でドレインとソースの導通を制御する素子。N-MOSはNチャネル型を表す。
      | 用語2　　　　　　　 ; GND：Ground（回路の基準電位・電流帰路）。この図の共通基準。保護接地や大地への接続を意味するとは限らない。
      | 用語3　　　　　　　 ; SW：Switching Node（スイッチング点）。主電力段の上下MOSFETとL1がつながる、電圧が高速に切り替わる点。GNDとは別電位。
      settings: AttributesFormatString=4.42 Ω
  R13 : fl_lib/Electrical/Electrical Elements/Resistor  Description=|  R=4.42 Ohm  i_specify=off  i_priority=None  i=0 A  i_nominal_specify=off  i_nominal_value=1  i_nominal_unit=A  v_specify=off  v_priority=None  v=0 V  v_nominal_specify=off  v_nominal_value=1  v_nominal_unit=V
      | この回路での名前　　; R13
      | 部品名　　　　　　　; CRCW25124R42FKEGHP
      | この回路での役割　　; 主電力MOSFET Q1・Q2の切替え時に生じる、電圧の振動を弱めるためのスナバ抵抗。
      | ここでの動き　　　　; C1と組み合わせ、切替え時の振動エネルギーを熱として消費する。R14と直列の一組になり、同じ二個直列の枝を六組並列にして抵抗値と電力負担を分ける。実際の減衰量・パルス電力・温度は別途確認する。
      | 
      | 【詳しい働き・仕様・接続・確認の範囲】
      | 部品種別　　　　　　; スナバ抵抗
      | 公称値　　　　　　　; 4.42 ohm
      | 配置目的　　　　　　; Q1/Q2のSWノードからC1へつながるスナバ抵抗網の一部。R3〜R14は2個直列の枝を6本並列にした構成。
      | 意図する動作　　　　; スイッチング時の振動エネルギーを抵抗で消費する意図。個々のパルス電力・温度・配置寄生は別途確認する。
      | 端子と接続　　　　　; 2 n → SNUB_MID_6、1 p → SW
      | モデルの範囲　　　　; Simscape抵抗の集中定数表現。部品の許容差、定格電力、温度係数、寄生インダクタンスの適合を示すものではない。
      | モデル設定　　　　　; R=4.42 Ω。これらは保存モデルの設定値であり、すべてが実部品の保証値という意味ではない。
      | 確認の範囲　　　　　; 本説明は保存回路の部品情報・端子割当・既存設計意図を整理したもの。今回の説明更新によって新たな動作試験や実機検証を実施した意味ではない。
      | 設計記録　　　　　　; evaluation\component_annotations_20261022_r01\before_graph.json
      | evaluation\component_annotations_20261022_r01\before_metadata.json
      | evaluation\protection_capacitor_integration_20261021_r01\final_delivery\independent_readback\physical_bom.json
      | 
      | 【この説明欄の略語・記号】
      | 用語1　　　　　　　 ; MOSFET：Metal-Oxide-Semiconductor Field-Effect Transistor（金属・酸化膜・半導体構造の電界効果トランジスタ）。ゲートとソースの電圧でドレインとソースの導通を制御する素子。N-MOSはNチャネル型を表す。
      | 用語2　　　　　　　 ; GND：Ground（回路の基準電位・電流帰路）。この図の共通基準。保護接地や大地への接続を意味するとは限らない。
      | 用語3　　　　　　　 ; SW：Switching Node（スイッチング点）。主電力段の上下MOSFETとL1がつながる、電圧が高速に切り替わる点。GNDとは別電位。
      settings: AttributesFormatString=4.42 Ω
  R14 : fl_lib/Electrical/Electrical Elements/Resistor  Description=|  R=4.42 Ohm  i_specify=off  i_priority=None  i=0 A  i_nominal_specify=off  i_nominal_value=1  i_nominal_unit=A  v_specify=off  v_priority=None  v=0 V  v_nominal_specify=off  v_nominal_value=1  v_nominal_unit=V
      | この回路での名前　　; R14
      | 部品名　　　　　　　; CRCW25124R42FKEGHP
      | この回路での役割　　; 主電力MOSFET Q1・Q2の切替え時に生じる、電圧の振動を弱めるためのスナバ抵抗。
      | ここでの動き　　　　; C1と組み合わせ、切替え時の振動エネルギーを熱として消費する。R13と直列の一組になり、同じ二個直列の枝を六組並列にして抵抗値と電力負担を分ける。実際の減衰量・パルス電力・温度は別途確認する。
      | 
      | 【詳しい働き・仕様・接続・確認の範囲】
      | 部品種別　　　　　　; スナバ抵抗
      | 公称値　　　　　　　; 4.42 ohm
      | 配置目的　　　　　　; Q1/Q2のSWノードからC1へつながるスナバ抵抗網の一部。R3〜R14は2個直列の枝を6本並列にした構成。
      | 意図する動作　　　　; スイッチング時の振動エネルギーを抵抗で消費する意図。個々のパルス電力・温度・配置寄生は別途確認する。
      | 端子と接続　　　　　; 2 n → SNUB_C、1 p → SNUB_MID_6
      | モデルの範囲　　　　; Simscape抵抗の集中定数表現。部品の許容差、定格電力、温度係数、寄生インダクタンスの適合を示すものではない。
      | モデル設定　　　　　; R=4.42 Ω。これらは保存モデルの設定値であり、すべてが実部品の保証値という意味ではない。
      | 確認の範囲　　　　　; 本説明は保存回路の部品情報・端子割当・既存設計意図を整理したもの。今回の説明更新によって新たな動作試験や実機検証を実施した意味ではない。
      | 設計記録　　　　　　; evaluation\component_annotations_20261022_r01\before_graph.json
      | evaluation\component_annotations_20261022_r01\before_metadata.json
      | evaluation\protection_capacitor_integration_20261021_r01\final_delivery\independent_readback\physical_bom.json
      | 
      | 【この説明欄の略語・記号】
      | 用語1　　　　　　　 ; MOSFET：Metal-Oxide-Semiconductor Field-Effect Transistor（金属・酸化膜・半導体構造の電界効果トランジスタ）。ゲートとソースの電圧でドレインとソースの導通を制御する素子。N-MOSはNチャネル型を表す。
      | 用語2　　　　　　　 ; GND：Ground（回路の基準電位・電流帰路）。この図の共通基準。保護接地や大地への接続を意味するとは限らない。
      | 用語3　　　　　　　 ; SW：Switching Node（スイッチング点）。主電力段の上下MOSFETとL1がつながる、電圧が高速に切り替わる点。GNDとは別電位。
      settings: AttributesFormatString=4.42 Ω
  R15 : fl_lib/Electrical/Electrical Elements/Resistor  Description=|  R=10000 Ohm  i_specify=off  i_priority=None  i=0 A  i_nominal_specify=off  i_nominal_value=1  i_nominal_unit=A  v_specify=off  v_priority=None  v=0 V  v_nominal_specify=off  v_nominal_value=1  v_nominal_unit=V
      | この回路での名前　　; R15
      | 部品名　　　　　　　; RC0603FR-0710KL
      | この回路での役割　　; マイコンがまだ信号を出していない間、測定用の変換IC U1を通信の非選択状態に置くための抵抗。
      | ここでの動き　　　　; U1の選択信号を3.3 V側のHighへ引き上げる。通信するときはマイコンがこの信号をLowへ引き下げてU1を選ぶ。U1本体へ運転電力を供給する役目ではない。
      | 
      | 【詳しい働き・仕様・接続・確認の範囲】
      | 部品種別　　　　　　; ADCチップ選択プルアップ抵抗
      | 公称値　　　　　　　; 10 kohm
      | 配置目的　　　　　　; SPI_CS_Nを3V3へ引き上げ、RP2040の出力が未確定なときにU1を非選択側へ保つ。
      | 意図する動作　　　　; 通信時にはGPIOがLOWへ駆動して選択する。起動中のGPIO設定との整合はファームウェア側でも確認する。
      | 端子と接続　　　　　; 1 1 → 3V3、2 2 → SPI_CS_N
      | モデルの範囲　　　　; Simscape抵抗の集中定数表現。部品の許容差、定格電力、温度係数、寄生インダクタンスの適合を示すものではない。
      | モデル設定　　　　　; R=10 kΩ。これらは保存モデルの設定値であり、すべてが実部品の保証値という意味ではない。
      | 確認の範囲　　　　　; 本説明は保存回路の部品情報・端子割当・既存設計意図を整理したもの。今回の説明更新によって新たな動作試験や実機検証を実施した意味ではない。
      | 設計記録　　　　　　; evaluation\component_annotations_20261022_r01\before_graph.json
      | evaluation\component_annotations_20261022_r01\before_metadata.json
      | evaluation\protection_capacitor_integration_20261021_r01\final_delivery\independent_readback\physical_bom.json
      | 
      | 【この説明欄の略語・記号】
      | 用語1　　　　　　　 ; ADC：Analog-to-Digital Converter（アナログ・デジタル変換器）。測定電圧をデジタル値へ変換する回路。電流や温度も、センサーで電圧へ変換した後に読み取る。
      | 用語2　　　　　　　 ; GPIO：General-Purpose Input/Output（汎用入出力端子）。入力・出力や周辺機能に割り当てられる端子。GPの後の数字はRP2040の端子信号番号で、基板上の物理ピン番号とは別。
      | 用語3　　　　　　　 ; SPI：Serial Peripheral Interface（同期式シリアル通信）。クロックとデータ線を使う通信方式。本回路ではRP2040と外付け測定用ADCの通信に使う。
      | 用語4　　　　　　　 ; CS_N：Chip Select（チップ選択信号）。末尾Nはこの設計でLow有効を表す。Lowにして通信対象のADCを選択する。
      settings: AttributesFormatString=10 kΩ
  R16 : fl_lib/Electrical/Electrical Elements/Resistor  Description=|  R=75000 Ohm  i_specify=off  i_priority=None  i=0 A  i_nominal_specify=off  i_nominal_value=1  i_nominal_unit=A  v_specify=off  v_priority=None  v=0 V  v_nominal_specify=off  v_nominal_value=1  v_nominal_unit=V
      | この回路での名前　　; R16
      | 部品名　　　　　　　; RG2012P-753-B-T5
      | この回路での役割　　; 太陽光パネル側の入力電圧を、測定用の変換IC U1に入力できる小さな電圧へ縮めるための抵抗。
      | ここでの動き　　　　; R17と直列になり、高い電圧を受け持つ側の抵抗を二個に分ける。二個それぞれ75 kΩで、通常の分圧動作では高電圧側の電圧負担を分担する。下側のR18と合わせて測定信号を作る。
      | 
      | 【詳しい働き・仕様・接続・確認の範囲】
      | 部品種別　　　　　　; PV入力電圧分圧・上側抵抗
      | 公称値　　　　　　　; 75 kohm 0.1%
      | 配置目的　　　　　　; VINの電圧をADC範囲へ縮小する分圧回路の上側75 kΩの1個。
      | 意図する動作　　　　; R17と直列、R18を下側として使用。電圧定格・許容差・入力異常時のADC保護は別評価。
      | 端子と接続　　　　　; 1 1 → VIN、2 2 → VPV_DIV_MID
      | モデルの範囲　　　　; Simscape抵抗の集中定数表現。部品の許容差、定格電力、温度係数、寄生インダクタンスの適合を示すものではない。
      | モデル設定　　　　　; R=75 kΩ。これらは保存モデルの設定値であり、すべてが実部品の保証値という意味ではない。
      | 確認の範囲　　　　　; 本説明は保存回路の部品情報・端子割当・既存設計意図を整理したもの。今回の説明更新によって新たな動作試験や実機検証を実施した意味ではない。
      | 設計記録　　　　　　; evaluation\component_annotations_20261022_r01\before_graph.json
      | evaluation\component_annotations_20261022_r01\before_metadata.json
      | evaluation\protection_capacitor_integration_20261021_r01\final_delivery\independent_readback\physical_bom.json
      | 
      | 【この説明欄の略語・記号】
      | 用語1　　　　　　　 ; ADC：Analog-to-Digital Converter（アナログ・デジタル変換器）。測定電圧をデジタル値へ変換する回路。電流や温度も、センサーで電圧へ変換した後に読み取る。
      | 用語2　　　　　　　 ; PV：Photovoltaic（太陽光発電）。光を電気へ変える発電方式。PVを含むネット名は太陽電池側の測定・電力経路を表す。
      | 用語3　　　　　　　 ; VIN/VOUT：入力電圧・出力電圧を表す端子／ネット名。INは入力、OUTは出力。電源変換器の電力端子なのか、検出用端子なのかは対象部品によって異なるため、端子と接続の説明に従う。
      settings: AttributesFormatString=75 kΩ
  R17 : fl_lib/Electrical/Electrical Elements/Resistor  Description=|  R=75000 Ohm  i_specify=off  i_priority=None  i=0 A  i_nominal_specify=off  i_nominal_value=1  i_nominal_unit=A  v_specify=off  v_priority=None  v=0 V  v_nominal_specify=off  v_nominal_value=1  v_nominal_unit=V
      | この回路での名前　　; R17
      | 部品名　　　　　　　; RG2012P-753-B-T5
      | この回路での役割　　; 太陽光パネル側の入力電圧の測定で、電圧を小さくする働きと抵抗一個あたりの電圧負担を、R16と分けるための抵抗。
      | ここでの動き　　　　; R16と合わせて上側150 kΩとなり、下側R18の3.3 kΩと組み合わせる。公称の測定電圧は元の電圧の3.3/(75+75+3.3)、約2.15%になる。抵抗の誤差や測定ICの誤差は別に含める。
      | 
      | 【詳しい働き・仕様・接続・確認の範囲】
      | 部品種別　　　　　　; PV入力電圧分圧・上側直列抵抗
      | 公称値　　　　　　　; 75 kohm 0.1%
      | 配置目的　　　　　　; R16に直列に追加される75 kΩで、高電圧側の分圧抵抗を分担する。
      | 意図する動作　　　　; R18=3.3 kΩと合わせた公称分圧比は3.3/(75+75+3.3)。ADC_VPVの値を元電圧へ換算する係数に用いる。
      | 端子と接続　　　　　; 1 1 → VPV_DIV_MID、2 2 → ADC_VPV
      | モデルの範囲　　　　; Simscape抵抗の集中定数表現。部品の許容差、定格電力、温度係数、寄生インダクタンスの適合を示すものではない。
      | モデル設定　　　　　; R=75 kΩ。これらは保存モデルの設定値であり、すべてが実部品の保証値という意味ではない。
      | 確認の範囲　　　　　; 本説明は保存回路の部品情報・端子割当・既存設計意図を整理したもの。今回の説明更新によって新たな動作試験や実機検証を実施した意味ではない。
      | 設計記録　　　　　　; evaluation\component_annotations_20261022_r01\before_graph.json
      | evaluation\component_annotations_20261022_r01\before_metadata.json
      | evaluation\protection_capacitor_integration_20261021_r01\final_delivery\independent_readback\physical_bom.json
      | 
      | 【この説明欄の略語・記号】
      | 用語1　　　　　　　 ; ADC：Analog-to-Digital Converter（アナログ・デジタル変換器）。測定電圧をデジタル値へ変換する回路。電流や温度も、センサーで電圧へ変換した後に読み取る。
      | 用語2　　　　　　　 ; PV：Photovoltaic（太陽光発電）。光を電気へ変える発電方式。PVを含むネット名は太陽電池側の測定・電力経路を表す。
      settings: AttributesFormatString=75 kΩ
  R18 : fl_lib/Electrical/Electrical Elements/Resistor  Description=|  R=3300 Ohm  i_specify=off  i_priority=None  i=0 A  i_nominal_specify=off  i_nominal_value=1  i_nominal_unit=A  v_specify=off  v_priority=None  v=0 V  v_nominal_specify=off  v_nominal_value=1  v_nominal_unit=V
      | この回路での名前　　; R18
      | 部品名　　　　　　　; RG2012P-332-B-T5
      | この回路での役割　　; 太陽光パネル側の入力電圧を何分の一にして測定するかを、上側の抵抗と一緒に決めるための抵抗。
      | ここでの動き　　　　; R16・R17から来た測定点を3.3 kΩで共通GNDへつなぐ。上側合計150 kΩとの比で、測定電圧は元の約2.15%になる。同じ測定点のコンデンサと組み合わせ、信号に混ざる速い変化も抑える。
      | 
      | 【詳しい働き・仕様・接続・確認の範囲】
      | 部品種別　　　　　　; PV入力電圧分圧・下側抵抗
      | 公称値　　　　　　　; 3.3 kohm 0.1%
      | 配置目的　　　　　　; ADC_VPVからGNDへ接続し、上側150 kΩとともに分圧比を決める。
      | 意図する動作　　　　; 分圧ノードのコンデンサとRCフィルタも構成する。公称比だけで測定精度を保証せず、抵抗公差・ADC・基準源も誤差に含める。
      | 端子と接続　　　　　; 1 1 → ADC_VPV、2 2 → GND
      | モデルの範囲　　　　; Simscape抵抗の集中定数表現。部品の許容差、定格電力、温度係数、寄生インダクタンスの適合を示すものではない。
      | モデル設定　　　　　; R=3.3 kΩ。これらは保存モデルの設定値であり、すべてが実部品の保証値という意味ではない。
      | 確認の範囲　　　　　; 本説明は保存回路の部品情報・端子割当・既存設計意図を整理したもの。今回の説明更新によって新たな動作試験や実機検証を実施した意味ではない。
      | 設計記録　　　　　　; evaluation\component_annotations_20261022_r01\before_graph.json
      | evaluation\component_annotations_20261022_r01\before_metadata.json
      | evaluation\protection_capacitor_integration_20261021_r01\final_delivery\independent_readback\physical_bom.json
      | 
      | 【この説明欄の略語・記号】
      | 用語1　　　　　　　 ; ADC：Analog-to-Digital Converter（アナログ・デジタル変換器）。測定電圧をデジタル値へ変換する回路。電流や温度も、センサーで電圧へ変換した後に読み取る。
      | 用語2　　　　　　　 ; PV：Photovoltaic（太陽光発電）。光を電気へ変える発電方式。PVを含むネット名は太陽電池側の測定・電力経路を表す。
      | 用語3　　　　　　　 ; RC：Resistor-Capacitor（抵抗とコンデンサの組合せ）。主に測定信号のフィルタや時定数を作る。カットオフ周波数は実際の接続と抵抗・容量から求める。
      | 用語4　　　　　　　 ; GND：Ground（回路の基準電位・電流帰路）。この図の共通基準。保護接地や大地への接続を意味するとは限らない。
      settings: AttributesFormatString=3.3 kΩ
  R19 : fl_lib/Electrical/Electrical Elements/Resistor  Description=|  R=75000 Ohm  i_specify=off  i_priority=None  i=0 A  i_nominal_specify=off  i_nominal_value=1  i_nominal_unit=A  v_specify=off  v_priority=None  v=0 V  v_nominal_specify=off  v_nominal_value=1  v_nominal_unit=V
      | この回路での名前　　; R19
      | 部品名　　　　　　　; RG2012P-753-B-T5
      | この回路での役割　　; 充電器の出力電圧を、測定用の変換IC U1に入力できる小さな電圧へ縮めるための抵抗。
      | ここでの動き　　　　; R20と直列になり、高い電圧を受け持つ側の抵抗を二個に分ける。二個それぞれ75 kΩで、通常の分圧動作では高電圧側の電圧負担を分担する。下側のR21と合わせて測定信号を作る。
      | 
      | 【詳しい働き・仕様・接続・確認の範囲】
      | 部品種別　　　　　　; 充電器出力電圧分圧・上側抵抗
      | 公称値　　　　　　　; 75 kohm 0.1%
      | 配置目的　　　　　　; VOUTの電圧をADC範囲へ縮小する分圧回路の上側75 kΩの1個。
      | 意図する動作　　　　; R20と直列、R21を下側として使用。電圧定格・許容差・入力異常時のADC保護は別評価。
      | 端子と接続　　　　　; 1 1 → VOUT、2 2 → VOUT_DIV_MID
      | モデルの範囲　　　　; Simscape抵抗の集中定数表現。部品の許容差、定格電力、温度係数、寄生インダクタンスの適合を示すものではない。
      | モデル設定　　　　　; R=75 kΩ。これらは保存モデルの設定値であり、すべてが実部品の保証値という意味ではない。
      | 確認の範囲　　　　　; 本説明は保存回路の部品情報・端子割当・既存設計意図を整理したもの。今回の説明更新によって新たな動作試験や実機検証を実施した意味ではない。
      | 設計記録　　　　　　; evaluation\component_annotations_20261022_r01\before_graph.json
      | evaluation\component_annotations_20261022_r01\before_metadata.json
      | evaluation\protection_capacitor_integration_20261021_r01\final_delivery\independent_readback\physical_bom.json
      | 
      | 【この説明欄の略語・記号】
      | 用語1　　　　　　　 ; ADC：Analog-to-Digital Converter（アナログ・デジタル変換器）。測定電圧をデジタル値へ変換する回路。電流や温度も、センサーで電圧へ変換した後に読み取る。
      | 用語2　　　　　　　 ; VIN/VOUT：入力電圧・出力電圧を表す端子／ネット名。INは入力、OUTは出力。電源変換器の電力端子なのか、検出用端子なのかは対象部品によって異なるため、端子と接続の説明に従う。
      settings: AttributesFormatString=75 kΩ
  R2 : Subsystem  Description=|  mask(太陽光充電回路 編集用部品){PartRef=R2, PartMPN=CSS4J-4026R-1L00F, PartValue=1 mOhm / Kelvin, DesignValue=CSS4J-4026R-1L00F, SourceRef=MAIN_SHUNT}
      | この回路での名前　　; R2
      | 部品名　　　　　　　; CSS4J-4026R-1L00F
      | この回路での役割　　; インダクタを出た充電電流を測るための、小さな抵抗。
      | ここでの動き　　　　; 充電電流が通ると生じる微小な電圧差を、測定用アンプU3に渡す。大電流を流す端子と電圧を測る端子を分け、主配線の電圧降下を測定へ混ぜにくくする。
      | 
      | 【詳しい働き・仕様・接続・確認の範囲】
      | 部品種別　　　　　　; 充電電流測定用4端子シャント
      | 公称値　　　　　　　; CSS4J-4026R-1L00F
      | 配置目的　　　　　　; L_OUTからVOUTへ流れる電流の電圧降下をU3で測定する。
      | 意図する動作　　　　; 電力端子IP/IMと測定端子KP/KMを分離するKelvin接続。図面で同電位でも、PCBでは電流配線と測定配線を端子近傍まで分ける。
      | 端子と接続　　　　　; IM IM → VOUT、KM KM → IL_SENSE_M、IP IP → L_OUT、KP KP → IL_SENSE_P
      | モデルの範囲　　　　; 4端子の接続を内部の標準抵抗へ割り当てた表現。Kelvin配線の抵抗・熱・磁気結合を実測同定したモデルではない。
      | モデル設定　　　　　; 内部シャントR=1 mΩ。これらは保存モデルの設定値であり、すべてが実部品の保証値という意味ではない。
      | 確認の範囲　　　　　; 本説明は保存回路の部品情報・端子割当・既存設計意図を整理したもの。今回の説明更新によって新たな動作試験や実機検証を実施した意味ではない。
      | 設計記録　　　　　　; evaluation\component_annotations_20261022_r01\before_graph.json
      | evaluation\component_annotations_20261022_r01\before_metadata.json
      | evaluation\protection_capacitor_integration_20261021_r01\final_delivery\independent_readback\physical_bom.json
      | 
      | 【この説明欄の略語・記号】
      | 用語1　　　　　　　 ; PCB：Printed Circuit Board（プリント配線板）。部品を実装し、銅配線で接続する基板。
      | 用語2　　　　　　　 ; VIN/VOUT：入力電圧・出力電圧を表す端子／ネット名。INは入力、OUTは出力。電源変換器の電力端子なのか、検出用端子なのかは対象部品によって異なるため、端子と接続の説明に従う。
      | 用語3　　　　　　　 ; IP/IM・KP/KM：4端子シャントの端子役割を区別する設計上の表記。IP/IMは主電流端子、KP/KMはKelvin（4端子測定）の検出端子。P/Mは正側・負側の区別であり、端子番号は採用部品の割当を参照する。
      mask prompts: PartRef "物理部品番号"; PartMPN "部品型番"; PartValue "部品値・表示値"; DesignValue "元設計値（記録）"; SourceRef "旧参照名（記録）"
      mask help: 回路図編集用です。端子・配線は実際のSimscape接続ですが、部品内部の動作式は未実装です。値・型番を変更し、配線をドラッグして編集できます。
      settings: AttributesFormatString=CSS4J-4026R-1L00F
      mask Display:
      | color('black');
      | plot([0 .30 .30 .35],[0.181818 0.181818 .5 .5]);
      | plot([0 .30 .30],[0.5 0.5 .5]);
      | plot([0 .13 .13 .70 .70],[0.818182 0.818182 .94 .94 .5]);
      | plot([.35 .35 .65 .65 .35],[.35 .65 .65 .35 .35]);
      | plot([.65 .70 .70 1],[.5 .5 0.5 0.5]);
      | text(0,0.261818,'IP','horizontalAlignment','left');
      | text(0,0.58,'KP','horizontalAlignment','left');
      | text(0,0.898182,'KM','horizontalAlignment','left');
      | text(1,0.58,'IM','horizontalAlignment','right');
  R20 : fl_lib/Electrical/Electrical Elements/Resistor  Description=|  R=75000 Ohm  i_specify=off  i_priority=None  i=0 A  i_nominal_specify=off  i_nominal_value=1  i_nominal_unit=A  v_specify=off  v_priority=None  v=0 V  v_nominal_specify=off  v_nominal_value=1  v_nominal_unit=V
      | この回路での名前　　; R20
      | 部品名　　　　　　　; RG2012P-753-B-T5
      | この回路での役割　　; 充電器の出力電圧の測定で、電圧を小さくする働きと抵抗一個あたりの電圧負担を、R19と分けるための抵抗。
      | ここでの動き　　　　; R19と合わせて上側150 kΩとなり、下側R21の3.3 kΩと組み合わせる。公称の測定電圧は元の電圧の3.3/(75+75+3.3)、約2.15%になる。抵抗の誤差や測定ICの誤差は別に含める。
      | 
      | 【詳しい働き・仕様・接続・確認の範囲】
      | 部品種別　　　　　　; 充電器出力電圧分圧・上側直列抵抗
      | 公称値　　　　　　　; 75 kohm 0.1%
      | 配置目的　　　　　　; R19に直列に追加される75 kΩで、高電圧側の分圧抵抗を分担する。
      | 意図する動作　　　　; R21=3.3 kΩと合わせた公称分圧比は3.3/(75+75+3.3)。ADC_VOUTの値を元電圧へ換算する係数に用いる。
      | 端子と接続　　　　　; 1 1 → VOUT_DIV_MID、2 2 → ADC_VOUT
      | モデルの範囲　　　　; Simscape抵抗の集中定数表現。部品の許容差、定格電力、温度係数、寄生インダクタンスの適合を示すものではない。
      | モデル設定　　　　　; R=75 kΩ。これらは保存モデルの設定値であり、すべてが実部品の保証値という意味ではない。
      | 確認の範囲　　　　　; 本説明は保存回路の部品情報・端子割当・既存設計意図を整理したもの。今回の説明更新によって新たな動作試験や実機検証を実施した意味ではない。
      | 設計記録　　　　　　; evaluation\component_annotations_20261022_r01\before_graph.json
      | evaluation\component_annotations_20261022_r01\before_metadata.json
      | evaluation\protection_capacitor_integration_20261021_r01\final_delivery\independent_readback\physical_bom.json
      | 
      | 【この説明欄の略語・記号】
      | 用語1　　　　　　　 ; ADC：Analog-to-Digital Converter（アナログ・デジタル変換器）。測定電圧をデジタル値へ変換する回路。電流や温度も、センサーで電圧へ変換した後に読み取る。
      | 用語2　　　　　　　 ; VIN/VOUT：入力電圧・出力電圧を表す端子／ネット名。INは入力、OUTは出力。電源変換器の電力端子なのか、検出用端子なのかは対象部品によって異なるため、端子と接続の説明に従う。
      settings: AttributesFormatString=75 kΩ
  R21 : fl_lib/Electrical/Electrical Elements/Resistor  Description=|  R=3300 Ohm  i_specify=off  i_priority=None  i=0 A  i_nominal_specify=off  i_nominal_value=1  i_nominal_unit=A  v_specify=off  v_priority=None  v=0 V  v_nominal_specify=off  v_nominal_value=1  v_nominal_unit=V
      | この回路での名前　　; R21
      | 部品名　　　　　　　; RG2012P-332-B-T5
      | この回路での役割　　; 充電器の出力電圧を何分の一にして測定するかを、上側の抵抗と一緒に決めるための抵抗。
      | ここでの動き　　　　; R19・R20から来た測定点を3.3 kΩで共通GNDへつなぐ。上側合計150 kΩとの比で、測定電圧は元の約2.15%になる。同じ測定点のコンデンサと組み合わせ、信号に混ざる速い変化も抑える。
      | 
      | 【詳しい働き・仕様・接続・確認の範囲】
      | 部品種別　　　　　　; 充電器出力電圧分圧・下側抵抗
      | 公称値　　　　　　　; 3.3 kohm 0.1%
      | 配置目的　　　　　　; ADC_VOUTからGNDへ接続し、上側150 kΩとともに分圧比を決める。
      | 意図する動作　　　　; 分圧ノードのコンデンサとRCフィルタも構成する。公称比だけで測定精度を保証せず、抵抗公差・ADC・基準源も誤差に含める。
      | 端子と接続　　　　　; 1 1 → ADC_VOUT、2 2 → GND
      | モデルの範囲　　　　; Simscape抵抗の集中定数表現。部品の許容差、定格電力、温度係数、寄生インダクタンスの適合を示すものではない。
      | モデル設定　　　　　; R=3.3 kΩ。これらは保存モデルの設定値であり、すべてが実部品の保証値という意味ではない。
      | 確認の範囲　　　　　; 本説明は保存回路の部品情報・端子割当・既存設計意図を整理したもの。今回の説明更新によって新たな動作試験や実機検証を実施した意味ではない。
      | 設計記録　　　　　　; evaluation\component_annotations_20261022_r01\before_graph.json
      | evaluation\component_annotations_20261022_r01\before_metadata.json
      | evaluation\protection_capacitor_integration_20261021_r01\final_delivery\independent_readback\physical_bom.json
      | 
      | 【この説明欄の略語・記号】
      | 用語1　　　　　　　 ; ADC：Analog-to-Digital Converter（アナログ・デジタル変換器）。測定電圧をデジタル値へ変換する回路。電流や温度も、センサーで電圧へ変換した後に読み取る。
      | 用語2　　　　　　　 ; RC：Resistor-Capacitor（抵抗とコンデンサの組合せ）。主に測定信号のフィルタや時定数を作る。カットオフ周波数は実際の接続と抵抗・容量から求める。
      | 用語3　　　　　　　 ; GND：Ground（回路の基準電位・電流帰路）。この図の共通基準。保護接地や大地への接続を意味するとは限らない。
      | 用語4　　　　　　　 ; VIN/VOUT：入力電圧・出力電圧を表す端子／ネット名。INは入力、OUTは出力。電源変換器の電力端子なのか、検出用端子なのかは対象部品によって異なるため、端子と接続の説明に従う。
      settings: AttributesFormatString=3.3 kΩ
  R22 : fl_lib/Electrical/Electrical Elements/Resistor  Description=|  R=75000 Ohm  i_specify=off  i_priority=None  i=0 A  i_nominal_specify=off  i_nominal_value=1  i_nominal_unit=A  v_specify=off  v_priority=None  v=0 V  v_nominal_specify=off  v_nominal_value=1  v_nominal_unit=V
      | この回路での名前　　; R22
      | 部品名　　　　　　　; RG2012P-753-B-T5
      | この回路での役割　　; 蓄電池側の電圧を、測定用の変換IC U1に入力できる小さな電圧へ縮めるための抵抗。
      | ここでの動き　　　　; R23と直列になり、高い電圧を受け持つ側の抵抗を二個に分ける。二個それぞれ75 kΩで、通常の分圧動作では高電圧側の電圧負担を分担する。下側のR24と合わせて測定信号を作る。
      | 
      | 【詳しい働き・仕様・接続・確認の範囲】
      | 部品種別　　　　　　; 電池側電圧分圧・上側抵抗
      | 公称値　　　　　　　; 75 kohm 0.1%
      | 配置目的　　　　　　; BAT_PLUSの電圧をADC範囲へ縮小する分圧回路の上側75 kΩの1個。
      | 意図する動作　　　　; R23と直列、R24を下側として使用。電圧定格・許容差・入力異常時のADC保護は別評価。
      | 端子と接続　　　　　; 1 1 → BAT_PLUS、2 2 → VBAT_DIV_MID
      | モデルの範囲　　　　; Simscape抵抗の集中定数表現。部品の許容差、定格電力、温度係数、寄生インダクタンスの適合を示すものではない。
      | モデル設定　　　　　; R=75 kΩ。これらは保存モデルの設定値であり、すべてが実部品の保証値という意味ではない。
      | 確認の範囲　　　　　; 本説明は保存回路の部品情報・端子割当・既存設計意図を整理したもの。今回の説明更新によって新たな動作試験や実機検証を実施した意味ではない。
      | 設計記録　　　　　　; evaluation\component_annotations_20261022_r01\before_graph.json
      | evaluation\component_annotations_20261022_r01\before_metadata.json
      | evaluation\protection_capacitor_integration_20261021_r01\final_delivery\independent_readback\physical_bom.json
      | 
      | 【この説明欄の略語・記号】
      | 用語1　　　　　　　 ; ADC：Analog-to-Digital Converter（アナログ・デジタル変換器）。測定電圧をデジタル値へ変換する回路。電流や温度も、センサーで電圧へ変換した後に読み取る。
      settings: AttributesFormatString=75 kΩ
  R23 : fl_lib/Electrical/Electrical Elements/Resistor  Description=|  R=75000 Ohm  i_specify=off  i_priority=None  i=0 A  i_nominal_specify=off  i_nominal_value=1  i_nominal_unit=A  v_specify=off  v_priority=None  v=0 V  v_nominal_specify=off  v_nominal_value=1  v_nominal_unit=V
      | この回路での名前　　; R23
      | 部品名　　　　　　　; RG2012P-753-B-T5
      | この回路での役割　　; 蓄電池側の電圧の測定で、電圧を小さくする働きと抵抗一個あたりの電圧負担を、R22と分けるための抵抗。
      | ここでの動き　　　　; R22と合わせて上側150 kΩとなり、下側R24の3.3 kΩと組み合わせる。公称の測定電圧は元の電圧の3.3/(75+75+3.3)、約2.15%になる。抵抗の誤差や測定ICの誤差は別に含める。
      | 
      | 【詳しい働き・仕様・接続・確認の範囲】
      | 部品種別　　　　　　; 電池側電圧分圧・上側直列抵抗
      | 公称値　　　　　　　; 75 kohm 0.1%
      | 配置目的　　　　　　; R22に直列に追加される75 kΩで、高電圧側の分圧抵抗を分担する。
      | 意図する動作　　　　; R24=3.3 kΩと合わせた公称分圧比は3.3/(75+75+3.3)。ADC_VBATの値を元電圧へ換算する係数に用いる。
      | 端子と接続　　　　　; 1 1 → VBAT_DIV_MID、2 2 → ADC_VBAT
      | モデルの範囲　　　　; Simscape抵抗の集中定数表現。部品の許容差、定格電力、温度係数、寄生インダクタンスの適合を示すものではない。
      | モデル設定　　　　　; R=75 kΩ。これらは保存モデルの設定値であり、すべてが実部品の保証値という意味ではない。
      | 確認の範囲　　　　　; 本説明は保存回路の部品情報・端子割当・既存設計意図を整理したもの。今回の説明更新によって新たな動作試験や実機検証を実施した意味ではない。
      | 設計記録　　　　　　; evaluation\component_annotations_20261022_r01\before_graph.json
      | evaluation\component_annotations_20261022_r01\before_metadata.json
      | evaluation\protection_capacitor_integration_20261021_r01\final_delivery\independent_readback\physical_bom.json
      | 
      | 【この説明欄の略語・記号】
      | 用語1　　　　　　　 ; ADC：Analog-to-Digital Converter（アナログ・デジタル変換器）。測定電圧をデジタル値へ変換する回路。電流や温度も、センサーで電圧へ変換した後に読み取る。
      settings: AttributesFormatString=75 kΩ
  R24 : fl_lib/Electrical/Electrical Elements/Resistor  Description=|  R=3300 Ohm  i_specify=off  i_priority=None  i=0 A  i_nominal_specify=off  i_nominal_value=1  i_nominal_unit=A  v_specify=off  v_priority=None  v=0 V  v_nominal_specify=off  v_nominal_value=1  v_nominal_unit=V
      | この回路での名前　　; R24
      | 部品名　　　　　　　; RG2012P-332-B-T5
      | この回路での役割　　; 蓄電池側の電圧を何分の一にして測定するかを、上側の抵抗と一緒に決めるための抵抗。
      | ここでの動き　　　　; R22・R23から来た測定点を3.3 kΩで共通GNDへつなぐ。上側合計150 kΩとの比で、測定電圧は元の約2.15%になる。同じ測定点のコンデンサと組み合わせ、信号に混ざる速い変化も抑える。
      | 
      | 【詳しい働き・仕様・接続・確認の範囲】
      | 部品種別　　　　　　; 電池側電圧分圧・下側抵抗
      | 公称値　　　　　　　; 3.3 kohm 0.1%
      | 配置目的　　　　　　; ADC_VBATからGNDへ接続し、上側150 kΩとともに分圧比を決める。
      | 意図する動作　　　　; 分圧ノードのコンデンサとRCフィルタも構成する。公称比だけで測定精度を保証せず、抵抗公差・ADC・基準源も誤差に含める。
      | 端子と接続　　　　　; 1 1 → ADC_VBAT、2 2 → GND
      | モデルの範囲　　　　; Simscape抵抗の集中定数表現。部品の許容差、定格電力、温度係数、寄生インダクタンスの適合を示すものではない。
      | モデル設定　　　　　; R=3.3 kΩ。これらは保存モデルの設定値であり、すべてが実部品の保証値という意味ではない。
      | 確認の範囲　　　　　; 本説明は保存回路の部品情報・端子割当・既存設計意図を整理したもの。今回の説明更新によって新たな動作試験や実機検証を実施した意味ではない。
      | 設計記録　　　　　　; evaluation\component_annotations_20261022_r01\before_graph.json
      | evaluation\component_annotations_20261022_r01\before_metadata.json
      | evaluation\protection_capacitor_integration_20261021_r01\final_delivery\independent_readback\physical_bom.json
      | 
      | 【この説明欄の略語・記号】
      | 用語1　　　　　　　 ; ADC：Analog-to-Digital Converter（アナログ・デジタル変換器）。測定電圧をデジタル値へ変換する回路。電流や温度も、センサーで電圧へ変換した後に読み取る。
      | 用語2　　　　　　　 ; RC：Resistor-Capacitor（抵抗とコンデンサの組合せ）。主に測定信号のフィルタや時定数を作る。カットオフ周波数は実際の接続と抵抗・容量から求める。
      | 用語3　　　　　　　 ; GND：Ground（回路の基準電位・電流帰路）。この図の共通基準。保護接地や大地への接続を意味するとは限らない。
      settings: AttributesFormatString=3.3 kΩ
  R25 : fl_lib/Electrical/Electrical Elements/Resistor  Description=|  R=100 Ohm  i_specify=off  i_priority=None  i=0 A  i_nominal_specify=off  i_nominal_value=1  i_nominal_unit=A  v_specify=off  v_priority=None  v=0 V  v_nominal_specify=off  v_nominal_value=1  v_nominal_unit=V
      | この回路での名前　　; R25
      | 部品名　　　　　　　; RG2012P-101-B-T5
      | この回路での役割　　; 太陽光パネルの電流を測る信号に混ざった速い変動を弱め、測定用の変換IC U1へ渡すための抵抗。
      | ここでの動き　　　　; 電流測定アンプU2の出力とU1の入力の間に入り、C23と組み合わせて信号をならす。100 Ωと100 nFの公称値による時定数は10 µsだが、実際に値が落ち着く時間にはアンプとU1の動作も関係する。
      | 
      | 【詳しい働き・仕様・接続・確認の範囲】
      | 部品種別　　　　　　; PV電流信号フィルタ抵抗
      | 公称値　　　　　　　; 100 ohm 0.1%
      | 配置目的　　　　　　; U2出力IPV_OUTとADC_IPVの間に入り、C23とともにADC入力の高周波変動を抑える。
      | 意図する動作　　　　; 公称100 Ωと100 nFでRC時定数10 µs。実際の整定はアンプ出力・ADC取得動作も含めて判断する。
      | 端子と接続　　　　　; 1 1 → IPV_OUT、2 2 → ADC_IPV
      | モデルの範囲　　　　; Simscape抵抗の集中定数表現。部品の許容差、定格電力、温度係数、寄生インダクタンスの適合を示すものではない。
      | モデル設定　　　　　; R=100 Ω。これらは保存モデルの設定値であり、すべてが実部品の保証値という意味ではない。
      | 確認の範囲　　　　　; 本説明は保存回路の部品情報・端子割当・既存設計意図を整理したもの。今回の説明更新によって新たな動作試験や実機検証を実施した意味ではない。
      | 設計記録　　　　　　; evaluation\component_annotations_20261022_r01\before_graph.json
      | evaluation\component_annotations_20261022_r01\before_metadata.json
      | evaluation\protection_capacitor_integration_20261021_r01\final_delivery\independent_readback\physical_bom.json
      | 
      | 【この説明欄の略語・記号】
      | 用語1　　　　　　　 ; ADC：Analog-to-Digital Converter（アナログ・デジタル変換器）。測定電圧をデジタル値へ変換する回路。電流や温度も、センサーで電圧へ変換した後に読み取る。
      | 用語2　　　　　　　 ; PV：Photovoltaic（太陽光発電）。光を電気へ変える発電方式。PVを含むネット名は太陽電池側の測定・電力経路を表す。
      | 用語3　　　　　　　 ; RC：Resistor-Capacitor（抵抗とコンデンサの組合せ）。主に測定信号のフィルタや時定数を作る。カットオフ周波数は実際の接続と抵抗・容量から求める。
      settings: AttributesFormatString=100 Ω
  R26 : fl_lib/Electrical/Electrical Elements/Resistor  Description=|  R=100 Ohm  i_specify=off  i_priority=None  i=0 A  i_nominal_specify=off  i_nominal_value=1  i_nominal_unit=A  v_specify=off  v_priority=None  v=0 V  v_nominal_specify=off  v_nominal_value=1  v_nominal_unit=V
      | この回路での名前　　; R26
      | 部品名　　　　　　　; RG2012P-101-B-T5
      | この回路での役割　　; 充電電流を測る信号に混ざった速い変動を弱め、測定用の変換IC U1へ渡すための抵抗。
      | ここでの動き　　　　; 電流測定アンプU3の出力とU1の入力の間に入り、C25と組み合わせて信号をならす。100 Ωと100 nFの公称値による時定数は10 µsで、信号の変化をならす一方で応答の遅れも加わる。
      | 
      | 【詳しい働き・仕様・接続・確認の範囲】
      | 部品種別　　　　　　; 充電電流信号フィルタ抵抗
      | 公称値　　　　　　　; 100 ohm 0.1%
      | 配置目的　　　　　　; U3出力IL_OUTとADC_ILの間に入り、C25とともにADC入力の高周波変動を抑える。
      | 意図する動作　　　　; 公称100 Ωと100 nFでRC時定数10 µs。サンプリング周期とフィルタ遅延を区別する。
      | 端子と接続　　　　　; 1 1 → IL_OUT、2 2 → ADC_IL
      | モデルの範囲　　　　; Simscape抵抗の集中定数表現。部品の許容差、定格電力、温度係数、寄生インダクタンスの適合を示すものではない。
      | モデル設定　　　　　; R=100 Ω。これらは保存モデルの設定値であり、すべてが実部品の保証値という意味ではない。
      | 確認の範囲　　　　　; 本説明は保存回路の部品情報・端子割当・既存設計意図を整理したもの。今回の説明更新によって新たな動作試験や実機検証を実施した意味ではない。
      | 設計記録　　　　　　; evaluation\component_annotations_20261022_r01\before_graph.json
      | evaluation\component_annotations_20261022_r01\before_metadata.json
      | evaluation\protection_capacitor_integration_20261021_r01\final_delivery\independent_readback\physical_bom.json
      | 
      | 【この説明欄の略語・記号】
      | 用語1　　　　　　　 ; ADC：Analog-to-Digital Converter（アナログ・デジタル変換器）。測定電圧をデジタル値へ変換する回路。電流や温度も、センサーで電圧へ変換した後に読み取る。
      | 用語2　　　　　　　 ; RC：Resistor-Capacitor（抵抗とコンデンサの組合せ）。主に測定信号のフィルタや時定数を作る。カットオフ周波数は実際の接続と抵抗・容量から求める。
      settings: AttributesFormatString=100 Ω
  R28 : fl_lib/Electrical/Electrical Elements/Resistor  Description=|  R=47 Ohm  i_specify=off  i_priority=None  i=0 A  i_nominal_specify=off  i_nominal_value=1  i_nominal_unit=A  v_specify=off  v_priority=None  v=0 V  v_nominal_specify=off  v_nominal_value=1  v_nominal_unit=V
      | この回路での名前　　; R28
      | 部品名　　　　　　　; RG2012P-470-B-T5
      | この回路での役割　　; 蓄電池の温度を測る信号から、測定時に混ざる非常に速い変動を弱めるための抵抗。
      | ここでの動き　　　　; 温度センサーU4と測定用の変換IC U1の間に入り、C27と組み合わせる。47 Ωと680 pFという小さな組合せなので、ゆっくり変わる温度そのものを長時間平均するための値ではない。
      | 
      | 【詳しい働き・仕様・接続・確認の範囲】
      | 部品種別　　　　　　; 電池温度信号フィルタ抵抗
      | 公称値　　　　　　　; 47 ohm
      | 配置目的　　　　　　; U4出力TBAT_OUTとADC_TBATの間に入り、C27と組み合わせる。
      | 意図する動作　　　　; 47 Ωと680 pFは主にADC取得時の高周波成分を扱う小さなRC。温度の低速変化そのものを大きく平滑化する値とは限らない。
      | 端子と接続　　　　　; 1 1 → TBAT_OUT、2 2 → ADC_TBAT
      | モデルの範囲　　　　; Simscape抵抗の集中定数表現。部品の許容差、定格電力、温度係数、寄生インダクタンスの適合を示すものではない。
      | モデル設定　　　　　; R=47 Ω。これらは保存モデルの設定値であり、すべてが実部品の保証値という意味ではない。
      | 確認の範囲　　　　　; 本説明は保存回路の部品情報・端子割当・既存設計意図を整理したもの。今回の説明更新によって新たな動作試験や実機検証を実施した意味ではない。
      | 設計記録　　　　　　; evaluation\component_annotations_20261022_r01\before_graph.json
      | evaluation\component_annotations_20261022_r01\before_metadata.json
      | evaluation\protection_capacitor_integration_20261021_r01\final_delivery\independent_readback\physical_bom.json
      | 
      | 【この説明欄の略語・記号】
      | 用語1　　　　　　　 ; ADC：Analog-to-Digital Converter（アナログ・デジタル変換器）。測定電圧をデジタル値へ変換する回路。電流や温度も、センサーで電圧へ変換した後に読み取る。
      | 用語2　　　　　　　 ; RC：Resistor-Capacitor（抵抗とコンデンサの組合せ）。主に測定信号のフィルタや時定数を作る。カットオフ周波数は実際の接続と抵抗・容量から求める。
      settings: AttributesFormatString=47 Ω
  R29 : fl_lib/Electrical/Electrical Elements/Resistor  Description=|  R=47 Ohm  i_specify=off  i_priority=None  i=0 A  i_nominal_specify=off  i_nominal_value=1  i_nominal_unit=A  v_specify=off  v_priority=None  v=0 V  v_nominal_specify=off  v_nominal_value=1  v_nominal_unit=V
      | この回路での名前　　; R29
      | 部品名　　　　　　　; RG2012P-470-B-T5
      | この回路での役割　　; 放熱器の温度を測る信号から、測定時に混ざる非常に速い変動を弱めるための抵抗。
      | ここでの動き　　　　; 温度センサーU5と測定用の変換IC U1の間に入り、C29と組み合わせる。扱うのはセンサーを置いた位置の温度信号であり、MOSFET内部の接合温度を直接測る機能ではない。
      | 
      | 【詳しい働き・仕様・接続・確認の範囲】
      | 部品種別　　　　　　; 放熱器温度信号フィルタ抵抗
      | 公称値　　　　　　　; 47 ohm
      | 配置目的　　　　　　; U5出力TSINK_OUTとADC_TSINKの間に入り、C29と組み合わせる。
      | 意図する動作　　　　; センサーの設置位置からMOSFET接合温度を直接測定したことにはならない。
      | 端子と接続　　　　　; 1 1 → TSINK_OUT、2 2 → ADC_TSINK
      | モデルの範囲　　　　; Simscape抵抗の集中定数表現。部品の許容差、定格電力、温度係数、寄生インダクタンスの適合を示すものではない。
      | モデル設定　　　　　; R=47 Ω。これらは保存モデルの設定値であり、すべてが実部品の保証値という意味ではない。
      | 確認の範囲　　　　　; 本説明は保存回路の部品情報・端子割当・既存設計意図を整理したもの。今回の説明更新によって新たな動作試験や実機検証を実施した意味ではない。
      | 設計記録　　　　　　; evaluation\component_annotations_20261022_r01\before_graph.json
      | evaluation\component_annotations_20261022_r01\before_metadata.json
      | evaluation\protection_capacitor_integration_20261021_r01\final_delivery\independent_readback\physical_bom.json
      | 
      | 【この説明欄の略語・記号】
      | 用語1　　　　　　　 ; ADC：Analog-to-Digital Converter（アナログ・デジタル変換器）。測定電圧をデジタル値へ変換する回路。電流や温度も、センサーで電圧へ変換した後に読み取る。
      | 用語2　　　　　　　 ; MOSFET：Metal-Oxide-Semiconductor Field-Effect Transistor（金属・酸化膜・半導体構造の電界効果トランジスタ）。ゲートとソースの電圧でドレインとソースの導通を制御する素子。N-MOSはNチャネル型を表す。
      settings: AttributesFormatString=47 Ω
  R3 : fl_lib/Electrical/Electrical Elements/Resistor  Description=|  R=4.42 Ohm  i_specify=off  i_priority=None  i=0 A  i_nominal_specify=off  i_nominal_value=1  i_nominal_unit=A  v_specify=off  v_priority=None  v=0 V  v_nominal_specify=off  v_nominal_value=1  v_nominal_unit=V
      | この回路での名前　　; R3
      | 部品名　　　　　　　; CRCW25124R42FKEGHP
      | この回路での役割　　; 主電力MOSFET Q1・Q2の切替え時に生じる、電圧の振動を弱めるためのスナバ抵抗。
      | ここでの動き　　　　; C1と組み合わせ、切替え時の振動エネルギーを熱として消費する。R4と直列の一組になり、同じ二個直列の枝を六組並列にして抵抗値と電力負担を分ける。実際の減衰量・パルス電力・温度は別途確認する。
      | 
      | 【詳しい働き・仕様・接続・確認の範囲】
      | 部品種別　　　　　　; スナバ抵抗
      | 公称値　　　　　　　; 4.42 ohm
      | 配置目的　　　　　　; Q1/Q2のSWノードからC1へつながるスナバ抵抗網の一部。R3〜R14は2個直列の枝を6本並列にした構成。
      | 意図する動作　　　　; スイッチング時の振動エネルギーを抵抗で消費する意図。個々のパルス電力・温度・配置寄生は別途確認する。
      | 端子と接続　　　　　; 2 n → SNUB_MID_1、1 p → SW
      | モデルの範囲　　　　; Simscape抵抗の集中定数表現。部品の許容差、定格電力、温度係数、寄生インダクタンスの適合を示すものではない。
      | モデル設定　　　　　; R=4.42 Ω。これらは保存モデルの設定値であり、すべてが実部品の保証値という意味ではない。
      | 確認の範囲　　　　　; 本説明は保存回路の部品情報・端子割当・既存設計意図を整理したもの。今回の説明更新によって新たな動作試験や実機検証を実施した意味ではない。
      | 設計記録　　　　　　; evaluation\component_annotations_20261022_r01\before_graph.json
      | evaluation\component_annotations_20261022_r01\before_metadata.json
      | evaluation\protection_capacitor_integration_20261021_r01\final_delivery\independent_readback\physical_bom.json
      | 
      | 【この説明欄の略語・記号】
      | 用語1　　　　　　　 ; MOSFET：Metal-Oxide-Semiconductor Field-Effect Transistor（金属・酸化膜・半導体構造の電界効果トランジスタ）。ゲートとソースの電圧でドレインとソースの導通を制御する素子。N-MOSはNチャネル型を表す。
      | 用語2　　　　　　　 ; GND：Ground（回路の基準電位・電流帰路）。この図の共通基準。保護接地や大地への接続を意味するとは限らない。
      | 用語3　　　　　　　 ; SW：Switching Node（スイッチング点）。主電力段の上下MOSFETとL1がつながる、電圧が高速に切り替わる点。GNDとは別電位。
      settings: AttributesFormatString=4.42 Ω
  R30 : fl_lib/Electrical/Electrical Elements/Resistor  Description=|  R=0.1 Ohm  i_specify=off  i_priority=None  i=0 A  i_nominal_specify=off  i_nominal_value=1  i_nominal_unit=A  v_specify=off  v_priority=None  v=0 V  v_nominal_specify=off  v_nominal_value=1  v_nominal_unit=V
      | この回路での名前　　; R30
      | 部品名　　　　　　　; ERJ3RSFR10V
      | この回路での役割　　; 測定の基準電圧を作るU6が、出力側のコンデンサC31を接続した状態で働くよう、コンデンサ枝の性質を調整するための抵抗。
      | ここでの動き　　　　; C31へ出入りする電流の経路に0.1 Ωを加える。測定用ICへ基準電圧を渡す本線ではなく、C31につながる枝に入っている。安定性はU6の条件と実コンデンサの損失を合わせて確認する。
      | 
      | 【詳しい働き・仕様・接続・確認の範囲】
      | 部品種別　　　　　　; 基準電源コンデンサ枝の直列抵抗
      | 公称値　　　　　　　; 0.1 ohm 1%
      | 配置目的　　　　　　; 基準源出力とC31の間へ入れ、容量負荷との関係を調整する。
      | 意図する動作　　　　; ADCのVREF本流に直列挿入した抵抗ではなく、C31の枝にある0.1 Ω。REF3025Eの安定条件と実コンデンサのESRを併せて確認する。
      | 端子と接続　　　　　; 1 1 → VREF2V5_ADC、2 2 → VREF_CAP_NODE
      | モデルの範囲　　　　; Simscape抵抗の集中定数表現。部品の許容差、定格電力、温度係数、寄生インダクタンスの適合を示すものではない。
      | モデル設定　　　　　; R=100 mΩ。これらは保存モデルの設定値であり、すべてが実部品の保証値という意味ではない。
      | 確認の範囲　　　　　; 本説明は保存回路の部品情報・端子割当・既存設計意図を整理したもの。今回の説明更新によって新たな動作試験や実機検証を実施した意味ではない。
      | 設計記録　　　　　　; evaluation\component_annotations_20261022_r01\before_graph.json
      | evaluation\component_annotations_20261022_r01\before_metadata.json
      | evaluation\protection_capacitor_integration_20261021_r01\final_delivery\independent_readback\physical_bom.json
      | 
      | 【この説明欄の略語・記号】
      | 用語1　　　　　　　 ; ESR：Equivalent Series Resistance（等価直列抵抗）。コンデンサの損失を直列抵抗で表した量。周波数・温度で変わり、損失とリプル電圧に関係する。
      | 用語2　　　　　　　 ; ADC：Analog-to-Digital Converter（アナログ・デジタル変換器）。測定電圧をデジタル値へ変換する回路。電流や温度も、センサーで電圧へ変換した後に読み取る。
      | 用語3　　　　　　　 ; VREF/REF：基準電圧を表す端子名。REFはReference（基準）の意味。ADCの変換尺度や電流アンプの出力基準に使う。REF1/REF2の接続電位は個別に確認する。
      settings: AttributesFormatString=100 mΩ
  R31 : fl_lib/Electrical/Electrical Elements/Resistor  Description=|  R=232 Ohm  i_specify=off  i_priority=None  i=0 A  i_nominal_specify=off  i_nominal_value=1  i_nominal_unit=A  v_specify=off  v_priority=None  v=0 V  v_nominal_specify=off  v_nominal_value=1  v_nominal_unit=V
      | この回路での名前　　; R31
      | 部品名　　　　　　　; ERJ6ENF2320V
      | この回路での役割　　; 上側ゲートドライバU8へ制御信号を伝える発光素子に、流れすぎる電流を抑えるための抵抗。
      | ここでの動き　　　　; 5 V電源から発光素子へ入る側に置き、発光素子を出た側のR32と一緒に電流を決める。Q3Aが導通すると電流が流れ、発光によって絶縁された先へ制御信号が伝わる。実電流は電源電圧と発光素子などの電圧降下でも変わる。
      | 
      | 【詳しい働き・仕様・接続・確認の範囲】
      | 部品種別　　　　　　; 上側ドライバLEDアノード側抵抗
      | 公称値　　　　　　　; 232 ohm 1% 0.125W
      | 配置目的　　　　　　; P5からU8のLEDへ流す電流をR32とともに制限する。
      | 意図する動作　　　　; LEDの順方向電圧、Q3Aの電圧降下、P5の変動で実電流が変わる。
      | 端子と接続　　　　　; 1 1 → P5、2 2 → H_LED_A
      | モデルの範囲　　　　; Simscape抵抗の集中定数表現。部品の許容差、定格電力、温度係数、寄生インダクタンスの適合を示すものではない。
      | モデル設定　　　　　; R=232 Ω。これらは保存モデルの設定値であり、すべてが実部品の保証値という意味ではない。
      | 確認の範囲　　　　　; 本説明は保存回路の部品情報・端子割当・既存設計意図を整理したもの。今回の説明更新によって新たな動作試験や実機検証を実施した意味ではない。
      | 設計記録　　　　　　; evaluation\component_annotations_20261022_r01\before_graph.json
      | evaluation\component_annotations_20261022_r01\before_metadata.json
      | evaluation\protection_capacitor_integration_20261021_r01\final_delivery\independent_readback\physical_bom.json
      | 
      | 【この説明欄の略語・記号】
      | 用語1　　　　　　　 ; LED：Light-Emitting Diode（発光ダイオード）。本回路のゲートドライバ入力では光によって信号を伝え、入力側と出力側を絶縁するために用いる。
      settings: AttributesFormatString=232 Ω
  R32 : fl_lib/Electrical/Electrical Elements/Resistor  Description=|  R=154 Ohm  i_specify=off  i_priority=None  i=0 A  i_nominal_specify=off  i_nominal_value=1  i_nominal_unit=A  v_specify=off  v_priority=None  v=0 V  v_nominal_specify=off  v_nominal_value=1  v_nominal_unit=V
      | この回路での名前　　; R32
      | 部品名　　　　　　　; ERJ6ENF1540V
      | この回路での役割　　; 上側ゲートドライバU8の発光素子に流す電流を、R31と一緒に制限するための抵抗。
      | ここでの動き　　　　; 発光素子を出てQ3Aへ向かう側に入り、R31と直列で電流を決める。電流を通す・止める指令はQ3Aが受け持ち、この抵抗は流れる量を抑える。
      | 
      | 【詳しい働き・仕様・接続・確認の範囲】
      | 部品種別　　　　　　; 上側ドライバLEDカソード側抵抗
      | 公称値　　　　　　　; 154 ohm 1% 0.125W
      | 配置目的　　　　　　; U8 LEDからQ3Aへ流れる電流をR31とともに制限する。
      | 意図する動作　　　　; R31と直列でLED電流を決める。単独でGPIO電圧をゲート電圧へ増幅する部品ではない。
      | 端子と接続　　　　　; 1 1 → H_LED_K、2 2 → H_LED_SINK
      | モデルの範囲　　　　; Simscape抵抗の集中定数表現。部品の許容差、定格電力、温度係数、寄生インダクタンスの適合を示すものではない。
      | モデル設定　　　　　; R=154 Ω。これらは保存モデルの設定値であり、すべてが実部品の保証値という意味ではない。
      | 確認の範囲　　　　　; 本説明は保存回路の部品情報・端子割当・既存設計意図を整理したもの。今回の説明更新によって新たな動作試験や実機検証を実施した意味ではない。
      | 設計記録　　　　　　; evaluation\component_annotations_20261022_r01\before_graph.json
      | evaluation\component_annotations_20261022_r01\before_metadata.json
      | evaluation\protection_capacitor_integration_20261021_r01\final_delivery\independent_readback\physical_bom.json
      | 
      | 【この説明欄の略語・記号】
      | 用語1　　　　　　　 ; GPIO：General-Purpose Input/Output（汎用入出力端子）。入力・出力や周辺機能に割り当てられる端子。GPの後の数字はRP2040の端子信号番号で、基板上の物理ピン番号とは別。
      | 用語2　　　　　　　 ; LED：Light-Emitting Diode（発光ダイオード）。本回路のゲートドライバ入力では光によって信号を伝え、入力側と出力側を絶縁するために用いる。
      settings: AttributesFormatString=154 Ω
  R33 : fl_lib/Electrical/Electrical Elements/Resistor  Description=|  R=20000 Ohm  i_specify=off  i_priority=None  i=0 A  i_nominal_specify=off  i_nominal_value=1  i_nominal_unit=A  v_specify=off  v_priority=None  v=0 V  v_nominal_specify=off  v_nominal_value=1  v_nominal_unit=V
      | この回路での名前　　; R33
      | 部品名　　　　　　　; ERJ6ENF2002V
      | この回路での役割　　; 上側ゲートドライバU8の発光素子が、わずかな漏れ電流で意図せず光ることを抑えるための抵抗。
      | ここでの動き　　　　; 発光素子の両端に20 kΩの通り道を並列に設け、微小な電流や残った電荷を逃がす。実際に誤点灯を防げる余裕は、発光素子とQ3Aの漏れ電流などを含めて確認する。
      | 
      | 【詳しい働き・仕様・接続・確認の範囲】
      | 部品種別　　　　　　; 上側ドライバLED並列抵抗
      | 公称値　　　　　　　; 20k 1%
      | 配置目的　　　　　　; U8のLEDアノード–カソード間に放電・漏れ電流の迂回経路を設ける。
      | 意図する動作　　　　; 微小電流でLEDが意図せず発光することを抑える意図。実際の誤点灯余裕はLED・MOSFET漏れと合わせて確認する。
      | 端子と接続　　　　　; 1 1 → H_LED_A、2 2 → H_LED_K
      | モデルの範囲　　　　; Simscape抵抗の集中定数表現。部品の許容差、定格電力、温度係数、寄生インダクタンスの適合を示すものではない。
      | モデル設定　　　　　; R=20 kΩ。これらは保存モデルの設定値であり、すべてが実部品の保証値という意味ではない。
      | 確認の範囲　　　　　; 本説明は保存回路の部品情報・端子割当・既存設計意図を整理したもの。今回の説明更新によって新たな動作試験や実機検証を実施した意味ではない。
      | 設計記録　　　　　　; evaluation\component_annotations_20261022_r01\before_graph.json
      | evaluation\component_annotations_20261022_r01\before_metadata.json
      | evaluation\protection_capacitor_integration_20261021_r01\final_delivery\independent_readback\physical_bom.json
      | 
      | 【この説明欄の略語・記号】
      | 用語1　　　　　　　 ; MOSFET：Metal-Oxide-Semiconductor Field-Effect Transistor（金属・酸化膜・半導体構造の電界効果トランジスタ）。ゲートとソースの電圧でドレインとソースの導通を制御する素子。N-MOSはNチャネル型を表す。
      | 用語2　　　　　　　 ; LED：Light-Emitting Diode（発光ダイオード）。本回路のゲートドライバ入力では光によって信号を伝え、入力側と出力側を絶縁するために用いる。
      settings: AttributesFormatString=20 kΩ
  R34 : fl_lib/Electrical/Electrical Elements/Resistor  Description=|  R=330 Ohm  i_specify=off  i_priority=None  i=0 A  i_nominal_specify=off  i_nominal_value=1  i_nominal_unit=A  v_specify=off  v_priority=None  v=0 V  v_nominal_specify=off  v_nominal_value=1  v_nominal_unit=V
      | この回路での名前　　; R34
      | 部品名　　　　　　　; ERJ6ENF3300V
      | この回路での役割　　; 上側ゲートドライバへ信号を送る小型MOSFET Q3Aを、マイコンから駆動するときの瞬間電流を抑えるための抵抗。
      | ここでの動き　　　　; マイコンの出力とQ3Aのゲートの間に330 Ωを入れ、ゲートにたまる電荷の出入りを抑える。そのぶん信号の立上がり・立下がりにも影響する。主電力MOSFETを直接駆動する抵抗とは役割が異なる。
      | 
      | 【詳しい働き・仕様・接続・確認の範囲】
      | 部品種別　　　　　　; 上側LED駆動MOSFETゲート抵抗
      | 公称値　　　　　　　; 330 ohm 1%
      | 配置目的　　　　　　; PWM_HとQ3Aゲートの間に入れ、ゲート充放電の瞬間電流を抑える。
      | 意図する動作　　　　; Q1の主ゲート抵抗R36とは別。PWMのエッジ遅延へ影響する。
      | 端子と接続　　　　　; 1 1 → PWM_H、2 2 → H_LED_GATE
      | モデルの範囲　　　　; Simscape抵抗の集中定数表現。部品の許容差、定格電力、温度係数、寄生インダクタンスの適合を示すものではない。
      | モデル設定　　　　　; R=330 Ω。これらは保存モデルの設定値であり、すべてが実部品の保証値という意味ではない。
      | 確認の範囲　　　　　; 本説明は保存回路の部品情報・端子割当・既存設計意図を整理したもの。今回の説明更新によって新たな動作試験や実機検証を実施した意味ではない。
      | 設計記録　　　　　　; evaluation\component_annotations_20261022_r01\before_graph.json
      | evaluation\component_annotations_20261022_r01\before_metadata.json
      | evaluation\protection_capacitor_integration_20261021_r01\final_delivery\independent_readback\physical_bom.json
      | 
      | 【この説明欄の略語・記号】
      | 用語1　　　　　　　 ; PWM：Pulse Width Modulation（パルス幅変調）。周期に対するON時間の割合を変えて、スイッチの平均的な電力伝達を調整する方式。
      | 用語2　　　　　　　 ; MOSFET：Metal-Oxide-Semiconductor Field-Effect Transistor（金属・酸化膜・半導体構造の電界効果トランジスタ）。ゲートとソースの電圧でドレインとソースの導通を制御する素子。N-MOSはNチャネル型を表す。
      | 用語3　　　　　　　 ; LED：Light-Emitting Diode（発光ダイオード）。本回路のゲートドライバ入力では光によって信号を伝え、入力側と出力側を絶縁するために用いる。
      settings: AttributesFormatString=330 Ω
  R35 : fl_lib/Electrical/Electrical Elements/Resistor  Description=|  R=10000 Ohm  i_specify=off  i_priority=None  i=0 A  i_nominal_specify=off  i_nominal_value=1  i_nominal_unit=A  v_specify=off  v_priority=None  v=0 V  v_nominal_specify=off  v_nominal_value=1  v_nominal_unit=V
      | この回路での名前　　; R35
      | 部品名　　　　　　　; ERJ6ENF1002V
      | この回路での役割　　; マイコンが信号を出していないとき、上側ゲートドライバU8へ送る光信号を消灯側に置くための抵抗。
      | ここでの動き　　　　; 光信号の電流を切り替えるQ3Aのゲートを10 kΩで共通GNDへ引き下げる。マイコン出力が未設定・開放状態の間にゲートの電荷を逃がし、Q3Aをオフ側へ戻す。起動全体の安全性は制御の順序と合わせて確認する。
      | 
      | 【詳しい働き・仕様・接続・確認の範囲】
      | 部品種別　　　　　　; 上側LED駆動MOSFETゲートプルダウン
      | 公称値　　　　　　　; 10k 1%
      | 配置目的　　　　　　; Q3AゲートをGNDへ引き下げ、RP2040未駆動時のLED消灯側の状態を作る。
      | 意図する動作　　　　; GPIOがHi-Zのときの既定状態を担う。起動・停止の全条件での安全性はシーケンスとともに確認する。
      | 端子と接続　　　　　; 1 1 → H_LED_GATE、2 2 → GND
      | モデルの範囲　　　　; Simscape抵抗の集中定数表現。部品の許容差、定格電力、温度係数、寄生インダクタンスの適合を示すものではない。
      | モデル設定　　　　　; R=10 kΩ。これらは保存モデルの設定値であり、すべてが実部品の保証値という意味ではない。
      | 確認の範囲　　　　　; 本説明は保存回路の部品情報・端子割当・既存設計意図を整理したもの。今回の説明更新によって新たな動作試験や実機検証を実施した意味ではない。
      | 設計記録　　　　　　; evaluation\component_annotations_20261022_r01\before_graph.json
      | evaluation\component_annotations_20261022_r01\before_metadata.json
      | evaluation\protection_capacitor_integration_20261021_r01\final_delivery\independent_readback\physical_bom.json
      | 
      | 【この説明欄の略語・記号】
      | 用語1　　　　　　　 ; GPIO：General-Purpose Input/Output（汎用入出力端子）。入力・出力や周辺機能に割り当てられる端子。GPの後の数字はRP2040の端子信号番号で、基板上の物理ピン番号とは別。
      | 用語2　　　　　　　 ; MOSFET：Metal-Oxide-Semiconductor Field-Effect Transistor（金属・酸化膜・半導体構造の電界効果トランジスタ）。ゲートとソースの電圧でドレインとソースの導通を制御する素子。N-MOSはNチャネル型を表す。
      | 用語3　　　　　　　 ; LED：Light-Emitting Diode（発光ダイオード）。本回路のゲートドライバ入力では光によって信号を伝え、入力側と出力側を絶縁するために用いる。
      | 用語4　　　　　　　 ; Hi-Z：High Impedance（高インピーダンス状態）。出力が強くHigh/Lowを駆動していない状態。プルアップやプルダウンによって端子電圧が決まる場合がある。
      | 用語5　　　　　　　 ; GND：Ground（回路の基準電位・電流帰路）。この図の共通基準。保護接地や大地への接続を意味するとは限らない。
      settings: AttributesFormatString=10 kΩ
  R36 : fl_lib/Electrical/Electrical Elements/Resistor  Description=|  R=10 Ohm  i_specify=off  i_priority=None  i=0 A  i_nominal_specify=off  i_nominal_value=1  i_nominal_unit=A  v_specify=off  v_priority=None  v=0 V  v_nominal_specify=off  v_nominal_value=1  v_nominal_unit=V
      | この回路での名前　　; R36
      | 部品名　　　　　　　; ERJ6ENF10R0V
      | この回路での役割　　; 上側の主電力MOSFET Q1をオン・オフする速さを調整するための抵抗。
      | ここでの動き　　　　; ゲートドライバU8からQ1のゲートへ出入りする電流を10 Ωで抑える。速すぎる切替えで生じる電圧の振動と、遅くすることで増える切替え損失の兼ね合いを調整する。現在値だけで波形や上下の同時オン防止が成立したとは判断しない。
      | 
      | 【詳しい働き・仕様・接続・確認の範囲】
      | 部品種別　　　　　　; 上側主MOSFETゲート抵抗
      | 公称値　　　　　　　; 10 ohm 1% 0.125W
      | 配置目的　　　　　　; U8のH_DRVとQ1のGATE_Hの間に入れ、Q1のゲート充放電速度を調整する。
      | 意図する動作　　　　; 速すぎるスイッチングと損失の兼ね合いを調整する。10 Ωだけでリンギング・デッドタイム成立を保証しない。
      | 端子と接続　　　　　; 1 1 → H_DRV、2 2 → GATE_H
      | モデルの範囲　　　　; Simscape抵抗の集中定数表現。部品の許容差、定格電力、温度係数、寄生インダクタンスの適合を示すものではない。
      | モデル設定　　　　　; R=10 Ω。これらは保存モデルの設定値であり、すべてが実部品の保証値という意味ではない。
      | 確認の範囲　　　　　; 本説明は保存回路の部品情報・端子割当・既存設計意図を整理したもの。今回の説明更新によって新たな動作試験や実機検証を実施した意味ではない。
      | 設計記録　　　　　　; evaluation\component_annotations_20261022_r01\before_graph.json
      | evaluation\component_annotations_20261022_r01\before_metadata.json
      | evaluation\protection_capacitor_integration_20261021_r01\final_delivery\independent_readback\physical_bom.json
      | 
      | 【この説明欄の略語・記号】
      | 用語1　　　　　　　 ; MOSFET：Metal-Oxide-Semiconductor Field-Effect Transistor（金属・酸化膜・半導体構造の電界効果トランジスタ）。ゲートとソースの電圧でドレインとソースの導通を制御する素子。N-MOSはNチャネル型を表す。
      settings: AttributesFormatString=10 Ω
  R37 : fl_lib/Electrical/Electrical Elements/Resistor  Description=|  R=10000 Ohm  i_specify=off  i_priority=None  i=0 A  i_nominal_specify=off  i_nominal_value=1  i_nominal_unit=A  v_specify=off  v_priority=None  v=0 V  v_nominal_specify=off  v_nominal_value=1  v_nominal_unit=V
      | この回路での名前　　; R37
      | 部品名　　　　　　　; ERJ6ENF1002V
      | この回路での役割　　; 上側の主電力MOSFET Q1を、ゲートドライバが動いていないときにオフ側へ戻すための抵抗。
      | ここでの動き　　　　; Q1のゲートとソースを10 kΩでつなぎ、ゲートに残った電荷をソースへ逃がす。戻す先は高速に電圧が変わるSWで、共通GNDではない。ゲートとソースの電圧差を小さくする役割を持つ。
      | 
      | 【詳しい働き・仕様・接続・確認の範囲】
      | 部品種別　　　　　　; 上側主MOSFETゲート–ソース抵抗
      | 公称値　　　　　　　; 10k 1%
      | 配置目的　　　　　　; Q1のゲートをソースSWへ戻し、ドライバ未給電時の残留電荷を逃がす。
      | 意図する動作　　　　; GNDへのプルダウンではない。SW電位に追従してVGSを下げる。
      | 端子と接続　　　　　; 1 1 → GATE_H、2 2 → SW
      | モデルの範囲　　　　; Simscape抵抗の集中定数表現。部品の許容差、定格電力、温度係数、寄生インダクタンスの適合を示すものではない。
      | モデル設定　　　　　; R=10 kΩ。これらは保存モデルの設定値であり、すべてが実部品の保証値という意味ではない。
      | 確認の範囲　　　　　; 本説明は保存回路の部品情報・端子割当・既存設計意図を整理したもの。今回の説明更新によって新たな動作試験や実機検証を実施した意味ではない。
      | 設計記録　　　　　　; evaluation\component_annotations_20261022_r01\before_graph.json
      | evaluation\component_annotations_20261022_r01\before_metadata.json
      | evaluation\protection_capacitor_integration_20261021_r01\final_delivery\independent_readback\physical_bom.json
      | 
      | 【この説明欄の略語・記号】
      | 用語1　　　　　　　 ; MOSFET：Metal-Oxide-Semiconductor Field-Effect Transistor（金属・酸化膜・半導体構造の電界効果トランジスタ）。ゲートとソースの電圧でドレインとソースの導通を制御する素子。N-MOSはNチャネル型を表す。
      | 用語2　　　　　　　 ; VGS：Gate-to-Source Voltage（ゲート・ソース間電圧）。ゲートの電圧をソース基準で表す。GND基準のゲート電圧とは同じとは限らない。
      | 用語3　　　　　　　 ; GND：Ground（回路の基準電位・電流帰路）。この図の共通基準。保護接地や大地への接続を意味するとは限らない。
      | 用語4　　　　　　　 ; SW：Switching Node（スイッチング点）。主電力段の上下MOSFETとL1がつながる、電圧が高速に切り替わる点。GNDとは別電位。
      settings: AttributesFormatString=10 kΩ
  R38 : fl_lib/Electrical/Electrical Elements/Resistor  Description=|  R=232 Ohm  i_specify=off  i_priority=None  i=0 A  i_nominal_specify=off  i_nominal_value=1  i_nominal_unit=A  v_specify=off  v_priority=None  v=0 V  v_nominal_specify=off  v_nominal_value=1  v_nominal_unit=V
      | この回路での名前　　; R38
      | 部品名　　　　　　　; ERJ6ENF2320V
      | この回路での役割　　; 下側ゲートドライバU9へ制御信号を伝える発光素子に、流れすぎる電流を抑えるための抵抗。
      | ここでの動き　　　　; 5 V電源から発光素子へ入る側に置き、発光素子を出た側のR39と一緒に電流を決める。Q3Bが導通すると電流が流れ、発光によって絶縁された先へ制御信号が伝わる。実電流は電源電圧と発光素子などの電圧降下でも変わる。
      | 
      | 【詳しい働き・仕様・接続・確認の範囲】
      | 部品種別　　　　　　; 下側ドライバLEDアノード側抵抗
      | 公称値　　　　　　　; 232 ohm 1% 0.125W
      | 配置目的　　　　　　; P5からU9のLEDへ流す電流をR39とともに制限する。
      | 意図する動作　　　　; LEDの順方向電圧、Q3Bの電圧降下、P5の変動で実電流が変わる。
      | 端子と接続　　　　　; 1 1 → P5、2 2 → L_LED_A
      | モデルの範囲　　　　; Simscape抵抗の集中定数表現。部品の許容差、定格電力、温度係数、寄生インダクタンスの適合を示すものではない。
      | モデル設定　　　　　; R=232 Ω。これらは保存モデルの設定値であり、すべてが実部品の保証値という意味ではない。
      | 確認の範囲　　　　　; 本説明は保存回路の部品情報・端子割当・既存設計意図を整理したもの。今回の説明更新によって新たな動作試験や実機検証を実施した意味ではない。
      | 設計記録　　　　　　; evaluation\component_annotations_20261022_r01\before_graph.json
      | evaluation\component_annotations_20261022_r01\before_metadata.json
      | evaluation\protection_capacitor_integration_20261021_r01\final_delivery\independent_readback\physical_bom.json
      | 
      | 【この説明欄の略語・記号】
      | 用語1　　　　　　　 ; LED：Light-Emitting Diode（発光ダイオード）。本回路のゲートドライバ入力では光によって信号を伝え、入力側と出力側を絶縁するために用いる。
      settings: AttributesFormatString=232 Ω
  R39 : fl_lib/Electrical/Electrical Elements/Resistor  Description=|  R=154 Ohm  i_specify=off  i_priority=None  i=0 A  i_nominal_specify=off  i_nominal_value=1  i_nominal_unit=A  v_specify=off  v_priority=None  v=0 V  v_nominal_specify=off  v_nominal_value=1  v_nominal_unit=V
      | この回路での名前　　; R39
      | 部品名　　　　　　　; ERJ6ENF1540V
      | この回路での役割　　; 下側ゲートドライバU9の発光素子に流す電流を、R38と一緒に制限するための抵抗。
      | ここでの動き　　　　; 発光素子を出てQ3Bへ向かう側に入り、R38と直列で電流を決める。電流を通す・止める指令はQ3Bが受け持ち、この抵抗は流れる量を抑える。
      | 
      | 【詳しい働き・仕様・接続・確認の範囲】
      | 部品種別　　　　　　; 下側ドライバLEDカソード側抵抗
      | 公称値　　　　　　　; 154 ohm 1% 0.125W
      | 配置目的　　　　　　; U9 LEDからQ3Bへ流れる電流をR38とともに制限する。
      | 意図する動作　　　　; R38と直列でLED電流を決める。
      | 端子と接続　　　　　; 1 1 → L_LED_K、2 2 → L_LED_SINK
      | モデルの範囲　　　　; Simscape抵抗の集中定数表現。部品の許容差、定格電力、温度係数、寄生インダクタンスの適合を示すものではない。
      | モデル設定　　　　　; R=154 Ω。これらは保存モデルの設定値であり、すべてが実部品の保証値という意味ではない。
      | 確認の範囲　　　　　; 本説明は保存回路の部品情報・端子割当・既存設計意図を整理したもの。今回の説明更新によって新たな動作試験や実機検証を実施した意味ではない。
      | 設計記録　　　　　　; evaluation\component_annotations_20261022_r01\before_graph.json
      | evaluation\component_annotations_20261022_r01\before_metadata.json
      | evaluation\protection_capacitor_integration_20261021_r01\final_delivery\independent_readback\physical_bom.json
      | 
      | 【この説明欄の略語・記号】
      | 用語1　　　　　　　 ; LED：Light-Emitting Diode（発光ダイオード）。本回路のゲートドライバ入力では光によって信号を伝え、入力側と出力側を絶縁するために用いる。
      settings: AttributesFormatString=154 Ω
  R4 : fl_lib/Electrical/Electrical Elements/Resistor  Description=|  R=4.42 Ohm  i_specify=off  i_priority=None  i=0 A  i_nominal_specify=off  i_nominal_value=1  i_nominal_unit=A  v_specify=off  v_priority=None  v=0 V  v_nominal_specify=off  v_nominal_value=1  v_nominal_unit=V
      | この回路での名前　　; R4
      | 部品名　　　　　　　; CRCW25124R42FKEGHP
      | この回路での役割　　; 主電力MOSFET Q1・Q2の切替え時に生じる、電圧の振動を弱めるためのスナバ抵抗。
      | ここでの動き　　　　; C1と組み合わせ、切替え時の振動エネルギーを熱として消費する。R3と直列の一組になり、同じ二個直列の枝を六組並列にして抵抗値と電力負担を分ける。実際の減衰量・パルス電力・温度は別途確認する。
      | 
      | 【詳しい働き・仕様・接続・確認の範囲】
      | 部品種別　　　　　　; スナバ抵抗
      | 公称値　　　　　　　; 4.42 ohm
      | 配置目的　　　　　　; Q1/Q2のSWノードからC1へつながるスナバ抵抗網の一部。R3〜R14は2個直列の枝を6本並列にした構成。
      | 意図する動作　　　　; スイッチング時の振動エネルギーを抵抗で消費する意図。個々のパルス電力・温度・配置寄生は別途確認する。
      | 端子と接続　　　　　; 2 n → SNUB_C、1 p → SNUB_MID_1
      | モデルの範囲　　　　; Simscape抵抗の集中定数表現。部品の許容差、定格電力、温度係数、寄生インダクタンスの適合を示すものではない。
      | モデル設定　　　　　; R=4.42 Ω。これらは保存モデルの設定値であり、すべてが実部品の保証値という意味ではない。
      | 確認の範囲　　　　　; 本説明は保存回路の部品情報・端子割当・既存設計意図を整理したもの。今回の説明更新によって新たな動作試験や実機検証を実施した意味ではない。
      | 設計記録　　　　　　; evaluation\component_annotations_20261022_r01\before_graph.json
      | evaluation\component_annotations_20261022_r01\before_metadata.json
      | evaluation\protection_capacitor_integration_20261021_r01\final_delivery\independent_readback\physical_bom.json
      | 
      | 【この説明欄の略語・記号】
      | 用語1　　　　　　　 ; MOSFET：Metal-Oxide-Semiconductor Field-Effect Transistor（金属・酸化膜・半導体構造の電界効果トランジスタ）。ゲートとソースの電圧でドレインとソースの導通を制御する素子。N-MOSはNチャネル型を表す。
      | 用語2　　　　　　　 ; GND：Ground（回路の基準電位・電流帰路）。この図の共通基準。保護接地や大地への接続を意味するとは限らない。
      | 用語3　　　　　　　 ; SW：Switching Node（スイッチング点）。主電力段の上下MOSFETとL1がつながる、電圧が高速に切り替わる点。GNDとは別電位。
      settings: AttributesFormatString=4.42 Ω
  R40 : fl_lib/Electrical/Electrical Elements/Resistor  Description=|  R=20000 Ohm  i_specify=off  i_priority=None  i=0 A  i_nominal_specify=off  i_nominal_value=1  i_nominal_unit=A  v_specify=off  v_priority=None  v=0 V  v_nominal_specify=off  v_nominal_value=1  v_nominal_unit=V
      | この回路での名前　　; R40
      | 部品名　　　　　　　; ERJ6ENF2002V
      | この回路での役割　　; 下側ゲートドライバU9の発光素子が、わずかな漏れ電流で意図せず光ることを抑えるための抵抗。
      | ここでの動き　　　　; 発光素子の両端に20 kΩの通り道を並列に設け、微小な電流や残った電荷を逃がす。実際に誤点灯を防げる余裕は、発光素子とQ3Bの漏れ電流などを含めて確認する。
      | 
      | 【詳しい働き・仕様・接続・確認の範囲】
      | 部品種別　　　　　　; 下側ドライバLED並列抵抗
      | 公称値　　　　　　　; 20k 1%
      | 配置目的　　　　　　; U9のLED両端に放電・漏れ電流の迂回経路を設ける。
      | 意図する動作　　　　; 微小電流による誤点灯を抑える意図。実部品の漏れとしきい値による評価は残る。
      | 端子と接続　　　　　; 1 1 → L_LED_A、2 2 → L_LED_K
      | モデルの範囲　　　　; Simscape抵抗の集中定数表現。部品の許容差、定格電力、温度係数、寄生インダクタンスの適合を示すものではない。
      | モデル設定　　　　　; R=20 kΩ。これらは保存モデルの設定値であり、すべてが実部品の保証値という意味ではない。
      | 確認の範囲　　　　　; 本説明は保存回路の部品情報・端子割当・既存設計意図を整理したもの。今回の説明更新によって新たな動作試験や実機検証を実施した意味ではない。
      | 設計記録　　　　　　; evaluation\component_annotations_20261022_r01\before_graph.json
      | evaluation\component_annotations_20261022_r01\before_metadata.json
      | evaluation\protection_capacitor_integration_20261021_r01\final_delivery\independent_readback\physical_bom.json
      | 
      | 【この説明欄の略語・記号】
      | 用語1　　　　　　　 ; LED：Light-Emitting Diode（発光ダイオード）。本回路のゲートドライバ入力では光によって信号を伝え、入力側と出力側を絶縁するために用いる。
      settings: AttributesFormatString=20 kΩ
  R41 : fl_lib/Electrical/Electrical Elements/Resistor  Description=|  R=330 Ohm  i_specify=off  i_priority=None  i=0 A  i_nominal_specify=off  i_nominal_value=1  i_nominal_unit=A  v_specify=off  v_priority=None  v=0 V  v_nominal_specify=off  v_nominal_value=1  v_nominal_unit=V
      | この回路での名前　　; R41
      | 部品名　　　　　　　; ERJ6ENF3300V
      | この回路での役割　　; 下側ゲートドライバへ信号を送る小型MOSFET Q3Bを、マイコンから駆動するときの瞬間電流を抑えるための抵抗。
      | ここでの動き　　　　; マイコンの出力とQ3Bのゲートの間に330 Ωを入れ、ゲートにたまる電荷の出入りを抑える。そのぶん信号の立上がり・立下がりにも影響する。主電力MOSFETを直接駆動する抵抗とは役割が異なる。
      | 
      | 【詳しい働き・仕様・接続・確認の範囲】
      | 部品種別　　　　　　; 下側LED駆動MOSFETゲート抵抗
      | 公称値　　　　　　　; 330 ohm 1%
      | 配置目的　　　　　　; PWM_LとQ3Bゲートの間に入れ、ゲート充放電の瞬間電流を抑える。
      | 意図する動作　　　　; 主電力MOSFET Q2のゲート抵抗R43とは別。
      | 端子と接続　　　　　; 1 1 → PWM_L、2 2 → L_LED_GATE
      | モデルの範囲　　　　; Simscape抵抗の集中定数表現。部品の許容差、定格電力、温度係数、寄生インダクタンスの適合を示すものではない。
      | モデル設定　　　　　; R=330 Ω。これらは保存モデルの設定値であり、すべてが実部品の保証値という意味ではない。
      | 確認の範囲　　　　　; 本説明は保存回路の部品情報・端子割当・既存設計意図を整理したもの。今回の説明更新によって新たな動作試験や実機検証を実施した意味ではない。
      | 設計記録　　　　　　; evaluation\component_annotations_20261022_r01\before_graph.json
      | evaluation\component_annotations_20261022_r01\before_metadata.json
      | evaluation\protection_capacitor_integration_20261021_r01\final_delivery\independent_readback\physical_bom.json
      | 
      | 【この説明欄の略語・記号】
      | 用語1　　　　　　　 ; PWM：Pulse Width Modulation（パルス幅変調）。周期に対するON時間の割合を変えて、スイッチの平均的な電力伝達を調整する方式。
      | 用語2　　　　　　　 ; MOSFET：Metal-Oxide-Semiconductor Field-Effect Transistor（金属・酸化膜・半導体構造の電界効果トランジスタ）。ゲートとソースの電圧でドレインとソースの導通を制御する素子。N-MOSはNチャネル型を表す。
      | 用語3　　　　　　　 ; LED：Light-Emitting Diode（発光ダイオード）。本回路のゲートドライバ入力では光によって信号を伝え、入力側と出力側を絶縁するために用いる。
      settings: AttributesFormatString=330 Ω
  R42 : fl_lib/Electrical/Electrical Elements/Resistor  Description=|  R=10000 Ohm  i_specify=off  i_priority=None  i=0 A  i_nominal_specify=off  i_nominal_value=1  i_nominal_unit=A  v_specify=off  v_priority=None  v=0 V  v_nominal_specify=off  v_nominal_value=1  v_nominal_unit=V
      | この回路での名前　　; R42
      | 部品名　　　　　　　; ERJ6ENF1002V
      | この回路での役割　　; マイコンが信号を出していないとき、下側ゲートドライバU9へ送る光信号を消灯側に置くための抵抗。
      | ここでの動き　　　　; 光信号の電流を切り替えるQ3Bのゲートを10 kΩで共通GNDへ引き下げる。マイコン出力が未設定・開放状態の間にゲートの電荷を逃がし、Q3Bをオフ側へ戻す。起動全体の安全性は制御の順序と合わせて確認する。
      | 
      | 【詳しい働き・仕様・接続・確認の範囲】
      | 部品種別　　　　　　; 下側LED駆動MOSFETゲートプルダウン
      | 公称値　　　　　　　; 10k 1%
      | 配置目的　　　　　　; Q3BゲートをGNDへ引き下げ、RP2040未駆動時のLED消灯側の状態を作る。
      | 意図する動作　　　　; GPIOの起動・Hi-Z状態と合わせて扱う。
      | 端子と接続　　　　　; 1 1 → L_LED_GATE、2 2 → GND
      | モデルの範囲　　　　; Simscape抵抗の集中定数表現。部品の許容差、定格電力、温度係数、寄生インダクタンスの適合を示すものではない。
      | モデル設定　　　　　; R=10 kΩ。これらは保存モデルの設定値であり、すべてが実部品の保証値という意味ではない。
      | 確認の範囲　　　　　; 本説明は保存回路の部品情報・端子割当・既存設計意図を整理したもの。今回の説明更新によって新たな動作試験や実機検証を実施した意味ではない。
      | 設計記録　　　　　　; evaluation\component_annotations_20261022_r01\before_graph.json
      | evaluation\component_annotations_20261022_r01\before_metadata.json
      | evaluation\protection_capacitor_integration_20261021_r01\final_delivery\independent_readback\physical_bom.json
      | 
      | 【この説明欄の略語・記号】
      | 用語1　　　　　　　 ; GPIO：General-Purpose Input/Output（汎用入出力端子）。入力・出力や周辺機能に割り当てられる端子。GPの後の数字はRP2040の端子信号番号で、基板上の物理ピン番号とは別。
      | 用語2　　　　　　　 ; MOSFET：Metal-Oxide-Semiconductor Field-Effect Transistor（金属・酸化膜・半導体構造の電界効果トランジスタ）。ゲートとソースの電圧でドレインとソースの導通を制御する素子。N-MOSはNチャネル型を表す。
      | 用語3　　　　　　　 ; LED：Light-Emitting Diode（発光ダイオード）。本回路のゲートドライバ入力では光によって信号を伝え、入力側と出力側を絶縁するために用いる。
      | 用語4　　　　　　　 ; Hi-Z：High Impedance（高インピーダンス状態）。出力が強くHigh/Lowを駆動していない状態。プルアップやプルダウンによって端子電圧が決まる場合がある。
      | 用語5　　　　　　　 ; GND：Ground（回路の基準電位・電流帰路）。この図の共通基準。保護接地や大地への接続を意味するとは限らない。
      settings: AttributesFormatString=10 kΩ
  R43 : fl_lib/Electrical/Electrical Elements/Resistor  Description=|  R=10 Ohm  i_specify=off  i_priority=None  i=0 A  i_nominal_specify=off  i_nominal_value=1  i_nominal_unit=A  v_specify=off  v_priority=None  v=0 V  v_nominal_specify=off  v_nominal_value=1  v_nominal_unit=V
      | この回路での名前　　; R43
      | 部品名　　　　　　　; ERJ6ENF10R0V
      | この回路での役割　　; 下側の主電力MOSFET Q2をオン・オフする速さを調整するための抵抗。
      | ここでの動き　　　　; ゲートドライバU9からQ2のゲートへ出入りする電流を10 Ωで抑える。速すぎる切替えで生じる電圧の振動と、遅くすることで増える切替え損失の兼ね合いを調整する。現在値だけで波形や上下の同時オン防止が成立したとは判断しない。
      | 
      | 【詳しい働き・仕様・接続・確認の範囲】
      | 部品種別　　　　　　; 下側主MOSFETゲート抵抗
      | 公称値　　　　　　　; 10 ohm 1% 0.125W
      | 配置目的　　　　　　; U9のL_DRVとQ2のGATE_Lの間に入れ、Q2のゲート充放電速度を調整する。
      | 意図する動作　　　　; 上側との伝搬遅延差・デッドタイムを含めて適合を評価する。
      | 端子と接続　　　　　; 1 1 → L_DRV、2 2 → GATE_L
      | モデルの範囲　　　　; Simscape抵抗の集中定数表現。部品の許容差、定格電力、温度係数、寄生インダクタンスの適合を示すものではない。
      | モデル設定　　　　　; R=10 Ω。これらは保存モデルの設定値であり、すべてが実部品の保証値という意味ではない。
      | 確認の範囲　　　　　; 本説明は保存回路の部品情報・端子割当・既存設計意図を整理したもの。今回の説明更新によって新たな動作試験や実機検証を実施した意味ではない。
      | 設計記録　　　　　　; evaluation\component_annotations_20261022_r01\before_graph.json
      | evaluation\component_annotations_20261022_r01\before_metadata.json
      | evaluation\protection_capacitor_integration_20261021_r01\final_delivery\independent_readback\physical_bom.json
      | 
      | 【この説明欄の略語・記号】
      | 用語1　　　　　　　 ; MOSFET：Metal-Oxide-Semiconductor Field-Effect Transistor（金属・酸化膜・半導体構造の電界効果トランジスタ）。ゲートとソースの電圧でドレインとソースの導通を制御する素子。N-MOSはNチャネル型を表す。
      settings: AttributesFormatString=10 Ω
  R44 : fl_lib/Electrical/Electrical Elements/Resistor  Description=|  R=10000 Ohm  i_specify=off  i_priority=None  i=0 A  i_nominal_specify=off  i_nominal_value=1  i_nominal_unit=A  v_specify=off  v_priority=None  v=0 V  v_nominal_specify=off  v_nominal_value=1  v_nominal_unit=V
      | この回路での名前　　; R44
      | 部品名　　　　　　　; ERJ6ENF1002V
      | この回路での役割　　; 下側の主電力MOSFET Q2を、ゲートドライバが動いていないときにオフ側へ戻すための抵抗。
      | ここでの動き　　　　; Q2のゲートとソースを10 kΩでつなぎ、ゲートに残った電荷を共通GNDへ逃がす。高速な切替えによる電荷の回り込みまで防げるかは、この抵抗の存在だけでは決まらない。
      | 
      | 【詳しい働き・仕様・接続・確認の範囲】
      | 部品種別　　　　　　; 下側主MOSFETゲート–ソース抵抗
      | 公称値　　　　　　　; 10k 1%
      | 配置目的　　　　　　; Q2のゲートをソースGNDへ戻し、ドライバ未給電時の残留電荷を逃がす。
      | 意図する動作　　　　; 動的なミラー結合による誤点弧対策の成立は、この抵抗の存在だけでは保証しない。
      | 端子と接続　　　　　; 1 1 → GATE_L、2 2 → GND
      | モデルの範囲　　　　; Simscape抵抗の集中定数表現。部品の許容差、定格電力、温度係数、寄生インダクタンスの適合を示すものではない。
      | モデル設定　　　　　; R=10 kΩ。これらは保存モデルの設定値であり、すべてが実部品の保証値という意味ではない。
      | 確認の範囲　　　　　; 本説明は保存回路の部品情報・端子割当・既存設計意図を整理したもの。今回の説明更新によって新たな動作試験や実機検証を実施した意味ではない。
      | 設計記録　　　　　　; evaluation\component_annotations_20261022_r01\before_graph.json
      | evaluation\component_annotations_20261022_r01\before_metadata.json
      | evaluation\protection_capacitor_integration_20261021_r01\final_delivery\independent_readback\physical_bom.json
      | 
      | 【この説明欄の略語・記号】
      | 用語1　　　　　　　 ; MOSFET：Metal-Oxide-Semiconductor Field-Effect Transistor（金属・酸化膜・半導体構造の電界効果トランジスタ）。ゲートとソースの電圧でドレインとソースの導通を制御する素子。N-MOSはNチャネル型を表す。
      | 用語2　　　　　　　 ; GND：Ground（回路の基準電位・電流帰路）。この図の共通基準。保護接地や大地への接続を意味するとは限らない。
      settings: AttributesFormatString=10 kΩ
  R45 : fl_lib/Electrical/Electrical Elements/Resistor  Description=|  R=38300 Ohm  i_specify=off  i_priority=None  i=0 A  i_nominal_specify=off  i_nominal_value=1  i_nominal_unit=A  v_specify=off  v_priority=None  v=0 V  v_nominal_specify=off  v_nominal_value=1  v_nominal_unit=V
      | この回路での名前　　; R45
      | 部品名　　　　　　　; ERJ6ENF3832V
      | この回路での役割　　; 上側ゲートドライバU8用の電源を、約12 Vに設定するための抵抗。
      | ここでの動き　　　　; 絶縁電源U10の出力をR46と一緒に小さな電圧へ分け、U10が出力の高さを調整するための信号を返す。測る基準は上側MOSFETのソースSWで、H12とSWの間を約12 Vにする設定である。
      | 
      | 【詳しい働き・仕様・接続・確認の範囲】
      | 部品種別　　　　　　; 浮動電源の帰還分圧上側抵抗
      | 公称値　　　　　　　; 38.3k 1%
      | 配置目的　　　　　　; H12からH_FBへ接続し、R46とともにU10の出力電圧帰還を構成する。
      | 意図する動作　　　　; 分圧の基準はSW。H12の対GND電圧とH12–SW間の電圧を混同しない。
      | 端子と接続　　　　　; 1 1 → H12、2 2 → H_FB
      | モデルの範囲　　　　; Simscape抵抗の集中定数表現。部品の許容差、定格電力、温度係数、寄生インダクタンスの適合を示すものではない。
      | モデル設定　　　　　; R=38.3 kΩ。これらは保存モデルの設定値であり、すべてが実部品の保証値という意味ではない。
      | 確認の範囲　　　　　; 本説明は保存回路の部品情報・端子割当・既存設計意図を整理したもの。今回の説明更新によって新たな動作試験や実機検証を実施した意味ではない。
      | 設計記録　　　　　　; evaluation\component_annotations_20261022_r01\before_graph.json
      | evaluation\component_annotations_20261022_r01\before_metadata.json
      | evaluation\protection_capacitor_integration_20261021_r01\final_delivery\independent_readback\physical_bom.json
      | 
      | 【この説明欄の略語・記号】
      | 用語1　　　　　　　 ; MOSFET：Metal-Oxide-Semiconductor Field-Effect Transistor（金属・酸化膜・半導体構造の電界効果トランジスタ）。ゲートとソースの電圧でドレインとソースの導通を制御する素子。N-MOSはNチャネル型を表す。
      | 用語2　　　　　　　 ; GND：Ground（回路の基準電位・電流帰路）。この図の共通基準。保護接地や大地への接続を意味するとは限らない。
      | 用語3　　　　　　　 ; FB：Feedback（帰還）。出力などを検出して内部制御へ戻すための信号・端子。
      | 用語4　　　　　　　 ; SW：Switching Node（スイッチング点）。主電力段の上下MOSFETとL1がつながる、電圧が高速に切り替わる点。GNDとは別電位。
      settings: AttributesFormatString=38.3 kΩ
  R46 : fl_lib/Electrical/Electrical Elements/Resistor  Description=|  R=10000 Ohm  i_specify=off  i_priority=None  i=0 A  i_nominal_specify=off  i_nominal_value=1  i_nominal_unit=A  v_specify=off  v_priority=None  v=0 V  v_nominal_specify=off  v_nominal_value=1  v_nominal_unit=V
      | この回路での名前　　; R46
      | 部品名　　　　　　　; ERJ6ENF1002V
      | この回路での役割　　; 上側ゲートドライバU8用の電源電圧を、R45と一緒に決めるための抵抗。
      | ここでの動き　　　　; U10へ戻す電圧検出点を、10 kΩで出力側の基準SWへつなぐ。上側のR45との比で約12 Vの設定を作り、C39もこの検出回路に関わる。基準SW自体は共通GNDとは別に上下する。
      | 
      | 【詳しい働き・仕様・接続・確認の範囲】
      | 部品種別　　　　　　; 浮動電源の帰還分圧下側抵抗
      | 公称値　　　　　　　; 10k 1%
      | 配置目的　　　　　　; H_FBからSWへ接続し、R45とともにU10の出力電圧帰還を構成する。
      | 意図する動作　　　　; C39も同じ帰還系に属する。実安定性はU10の制御と出力容量を含めて確認する。
      | 端子と接続　　　　　; 1 1 → H_FB、2 2 → SW
      | モデルの範囲　　　　; Simscape抵抗の集中定数表現。部品の許容差、定格電力、温度係数、寄生インダクタンスの適合を示すものではない。
      | モデル設定　　　　　; R=10 kΩ。これらは保存モデルの設定値であり、すべてが実部品の保証値という意味ではない。
      | 確認の範囲　　　　　; 本説明は保存回路の部品情報・端子割当・既存設計意図を整理したもの。今回の説明更新によって新たな動作試験や実機検証を実施した意味ではない。
      | 設計記録　　　　　　; evaluation\component_annotations_20261022_r01\before_graph.json
      | evaluation\component_annotations_20261022_r01\before_metadata.json
      | evaluation\protection_capacitor_integration_20261021_r01\final_delivery\independent_readback\physical_bom.json
      | 
      | 【この説明欄の略語・記号】
      | 用語1　　　　　　　 ; MOSFET：Metal-Oxide-Semiconductor Field-Effect Transistor（金属・酸化膜・半導体構造の電界効果トランジスタ）。ゲートとソースの電圧でドレインとソースの導通を制御する素子。N-MOSはNチャネル型を表す。
      | 用語2　　　　　　　 ; GND：Ground（回路の基準電位・電流帰路）。この図の共通基準。保護接地や大地への接続を意味するとは限らない。
      | 用語3　　　　　　　 ; FB：Feedback（帰還）。出力などを検出して内部制御へ戻すための信号・端子。
      | 用語4　　　　　　　 ; SW：Switching Node（スイッチング点）。主電力段の上下MOSFETとL1がつながる、電圧が高速に切り替わる点。GNDとは別電位。
      settings: AttributesFormatString=10 kΩ
  R47 : fl_lib/Electrical/Electrical Elements/Resistor  Description=|  R=0 Ohm  i_specify=off  i_priority=None  i=0 A  i_nominal_specify=off  i_nominal_value=1  i_nominal_unit=A  v_specify=off  v_priority=None  v=0 V  v_nominal_specify=off  v_nominal_value=1  v_nominal_unit=V
      | この回路での名前　　; R47
      | 部品名　　　　　　　; ERJ6GEY0R00V
      | この回路での役割　　; 上側ゲート駆動用電源U10の、出力調整回路の設定接続を作るための0 Ω抵抗。
      | ここでの動き　　　　; U10のRLIMという設定端子を、出力電源H12へつなぐ。ここでの0 Ωは電線に近い接続を作る指定で、電流制限値を0 Aにする意味ではない。RLIMの定量的な設定条件は別途メーカー仕様との照合が必要。
      | 
      | 【詳しい働き・仕様・接続・確認の範囲】
      | 部品種別　　　　　　; 絶縁電源RLIM設定リンク
      | 公称値　　　　　　　; 0 ohm
      | 配置目的　　　　　　; H_RLIMとH12を0 Ωで接続し、U10のRLIM端子の既存設定を実装する。
      | 意図する動作　　　　; 0 Ωは設定接続の意味であり、電流制限値が0 Aという意味ではない。RLIMの定量仕様はメーカー条件との照合が必要。
      | 端子と接続　　　　　; 1 1 → H_RLIM、2 2 → H12
      | モデルの範囲　　　　; Simscape抵抗の集中定数表現。部品の許容差、定格電力、温度係数、寄生インダクタンスの適合を示すものではない。
      | モデル設定　　　　　; R=0 Ω。これらは保存モデルの設定値であり、すべてが実部品の保証値という意味ではない。
      | 確認の範囲　　　　　; 本説明は保存回路の部品情報・端子割当・既存設計意図を整理したもの。今回の説明更新によって新たな動作試験や実機検証を実施した意味ではない。
      | 設計記録　　　　　　; evaluation\component_annotations_20261022_r01\before_graph.json
      | evaluation\component_annotations_20261022_r01\before_metadata.json
      | evaluation\protection_capacitor_integration_20261021_r01\final_delivery\independent_readback\physical_bom.json
      | 
      | 【この説明欄の略語・記号】
      | 用語1　　　　　　　 ; RLIM：U10の外付け抵抗による制限設定端子。外付けR47で二次側の電圧調整に使う電流を制限する端子。主電力段の充電電流制限とは別の機能。
      settings: AttributesFormatString=0 Ω
  R48 : fl_lib/Electrical/Electrical Elements/Resistor  Description=|  R=10000 Ohm  i_specify=off  i_priority=None  i=0 A  i_nominal_specify=off  i_nominal_value=1  i_nominal_unit=A  v_specify=off  v_priority=None  v=0 V  v_nominal_specify=off  v_nominal_value=1  v_nominal_unit=V
      | この回路での名前　　; R48
      | 部品名　　　　　　　; ERJ6ENF1002V
      | この回路での役割　　; マイコンが指令を出していないとき、上側ゲート駆動用の絶縁電源U10を停止側に置くための抵抗。
      | ここでの動き　　　　; U7のGP8とU10のENAを結ぶBIAS_ENを、10 kΩで共通GNDへ引き下げる。マイコンがHighを出すとU10の動作を許可し、Lowまたは未駆動の間は停止側にする。U10の起動完了を待ってからPWMを開始する順序はプログラムが受け持つ。
      | 
      | 【詳しい働き・仕様・接続・確認の範囲】
      | 部品種別　　　　　　; 絶縁電源イネーブル・プルダウン
      | 公称値　　　　　　　; 10k 1%
      | 配置目的　　　　　　; BIAS_ENをGNDへ引き下げ、RP2040未駆動時のU10停止側の状態を作る。
      | 意図する動作　　　　; U10の起動完了確認とPWM開始の順序はファームウェア側の責務。
      | 端子と接続　　　　　; 1 1 → BIAS_EN、2 2 → GND
      | モデルの範囲　　　　; Simscape抵抗の集中定数表現。部品の許容差、定格電力、温度係数、寄生インダクタンスの適合を示すものではない。
      | モデル設定　　　　　; R=10 kΩ。これらは保存モデルの設定値であり、すべてが実部品の保証値という意味ではない。
      | 確認の範囲　　　　　; 本説明は保存回路の部品情報・端子割当・既存設計意図を整理したもの。今回の説明更新によって新たな動作試験や実機検証を実施した意味ではない。
      | 設計記録　　　　　　; evaluation\component_annotations_20261022_r01\before_graph.json
      | evaluation\component_annotations_20261022_r01\before_metadata.json
      | evaluation\protection_capacitor_integration_20261021_r01\final_delivery\independent_readback\physical_bom.json
      | 
      | 【この説明欄の略語・記号】
      | 用語1　　　　　　　 ; PWM：Pulse Width Modulation（パルス幅変調）。周期に対するON時間の割合を変えて、スイッチの平均的な電力伝達を調整する方式。
      | 用語2　　　　　　　 ; GND：Ground（回路の基準電位・電流帰路）。この図の共通基準。保護接地や大地への接続を意味するとは限らない。
      | 用語3　　　　　　　 ; EN：Enable（動作許可）。対象機能の動作を許可する信号。端子ごとの有効レベルや接続状態に従う。
      | 
      | 【マイコン端子との関係】
      | 名前の意味　　　　　; BIASは英単語Bias（バイアス）で、この図ではゲート駆動用の補助電源を指す。EN = Enable（動作許可）、PG = Power Good（電源状態通知）。ラベルは部品ではなく、同じ階層の同名ノードとの接続を示す。
      | 支える信号　　　　　; U7のGP8とU10のENA（4番）は同じノード。Highで絶縁電源の動作を許可し、Lowで停止を指示する。R48はそのノードからGNDへの10 kΩプルダウンで、マイコン端子が駆動されない間のLow側の状態を作る。
      | 配置の理由　　　　　; 対応するU7の端子へ直接配線し、その接続点から遠隔U10へのラベルを分岐する。抵抗の目的を回路図で読み取りやすくするための配置。実基板では配線長・受信側端子・起動条件を含めて配置を検討する。
      | メーカー根拠　　　　; https://www.ti.com/lit/gpn/ucc14131-q1（UCC14131-Q1データシート、端子表と11.3.3）
      settings: AttributesFormatString=10 kΩ
  R49 : fl_lib/Electrical/Electrical Elements/Resistor  Description=|  R=10000 Ohm  i_specify=off  i_priority=None  i=0 A  i_nominal_specify=off  i_nominal_value=1  i_nominal_unit=A  v_specify=off  v_priority=None  v=0 V  v_nominal_specify=off  v_nominal_value=1  v_nominal_unit=V
      | この回路での名前　　; R49
      | 部品名　　　　　　　; ERJ6ENF1002V
      | この回路での役割　　; 絶縁電源U10から返る状態通知を、マイコンU7のGP9がHigh・Lowとして読めるようにするための抵抗。
      | ここでの動き　　　　; U10が通知出力を解放すると、10 kΩを通じて信号を3.3 VのHighへ引き上げる。U10の電源が正常に成立するとU10自身がLowへ引き下げるため、この信号ではLowが正常成立を表す。抵抗は入力信号の電位を作り、マイコン本体の運転電力を供給するものではない。
      | 
      | 【詳しい働き・仕様・接続・確認の範囲】
      | 部品種別　　　　　　; 絶縁電源Power Goodプルアップ
      | 公称値　　　　　　　; 10k 1%
      | 配置目的　　　　　　; U10のオープンドレインPG信号BIAS_PGをPicoの3V3へ引き上げ、GP9で読める電圧にする。
      | 意図する動作　　　　; PG端子自身がHIGH電圧を供給するわけではない。U10入力12 Vへのプルアップではなく3.3 V系への接続。
      | 端子と接続　　　　　; 1 1 → BIAS_PG、2 2 → 3V3
      | モデルの範囲　　　　; Simscape抵抗の集中定数表現。部品の許容差、定格電力、温度係数、寄生インダクタンスの適合を示すものではない。
      | モデル設定　　　　　; R=10 kΩ。これらは保存モデルの設定値であり、すべてが実部品の保証値という意味ではない。
      | 確認の範囲　　　　　; 本説明は保存回路の部品情報・端子割当・既存設計意図を整理したもの。今回の説明更新によって新たな動作試験や実機検証を実施した意味ではない。
      | 設計記録　　　　　　; evaluation\component_annotations_20261022_r01\before_graph.json
      | evaluation\component_annotations_20261022_r01\before_metadata.json
      | evaluation\protection_capacitor_integration_20261021_r01\final_delivery\independent_readback\physical_bom.json
      | 
      | 【この説明欄の略語・記号】
      | 用語1　　　　　　　 ; IC：Integrated Circuit（集積回路）。複数の電子素子と機能を小さな半導体チップに集積した部品。
      | 用語2　　　　　　　 ; GPIO：General-Purpose Input/Output（汎用入出力端子）。入力・出力や周辺機能に割り当てられる端子。GPの後の数字はRP2040の端子信号番号で、基板上の物理ピン番号とは別。
      | 用語3　　　　　　　 ; PG：Power Good（電源状態通知）。電源出力が規定状態にあるかを知らせる信号。プルアップ条件と実際の通知条件は対象ICの説明で確認する。
      | 
      | 【マイコン端子との関係】
      | 名前の意味　　　　　; BIASは英単語Bias（バイアス）で、この図ではゲート駆動用の補助電源を指す。EN = Enable（動作許可）、PG = Power Good（電源状態通知）。ラベルは部品ではなく、同じ階層の同名ノードとの接続を示す。
      | 支える信号　　　　　; U10のPG（3番）からU7のGP9へ状態を返す。U10の正常成立時は内部出力がLowへ引き込み、正常不成立・停止時は出力を解放する。R49は解放時のノードを3.3 Vへ引き上げる10 kΩプルアップ。GP9は入力として読む。Highが正常という意味ではない。
      | 配置の理由　　　　　; 対応するU7の端子へ直接配線し、その接続点から遠隔U10へのラベルを分岐する。抵抗の目的を回路図で読み取りやすくするための配置。実基板では配線長・受信側端子・起動条件を含めて配置を検討する。
      | 電源との違い　　　　; マイコン本体の運転電力を供給する抵抗ではない。入力信号のHigh電位を作る。Low時の抵抗電流は公称値で約3.3 V / 10 kΩ = 0.33 mA。
      | メーカー根拠　　　　; https://www.ti.com/lit/gpn/ucc14131-q1（UCC14131-Q1データシート、端子表と11.3.3）
      settings: AttributesFormatString=10 kΩ
  R5 : fl_lib/Electrical/Electrical Elements/Resistor  Description=|  R=4.42 Ohm  i_specify=off  i_priority=None  i=0 A  i_nominal_specify=off  i_nominal_value=1  i_nominal_unit=A  v_specify=off  v_priority=None  v=0 V  v_nominal_specify=off  v_nominal_value=1  v_nominal_unit=V
      | この回路での名前　　; R5
      | 部品名　　　　　　　; CRCW25124R42FKEGHP
      | この回路での役割　　; 主電力MOSFET Q1・Q2の切替え時に生じる、電圧の振動を弱めるためのスナバ抵抗。
      | ここでの動き　　　　; C1と組み合わせ、切替え時の振動エネルギーを熱として消費する。R6と直列の一組になり、同じ二個直列の枝を六組並列にして抵抗値と電力負担を分ける。実際の減衰量・パルス電力・温度は別途確認する。
      | 
      | 【詳しい働き・仕様・接続・確認の範囲】
      | 部品種別　　　　　　; スナバ抵抗
      | 公称値　　　　　　　; 4.42 ohm
      | 配置目的　　　　　　; Q1/Q2のSWノードからC1へつながるスナバ抵抗網の一部。R3〜R14は2個直列の枝を6本並列にした構成。
      | 意図する動作　　　　; スイッチング時の振動エネルギーを抵抗で消費する意図。個々のパルス電力・温度・配置寄生は別途確認する。
      | 端子と接続　　　　　; 2 n → SNUB_MID_2、1 p → SW
      | モデルの範囲　　　　; Simscape抵抗の集中定数表現。部品の許容差、定格電力、温度係数、寄生インダクタンスの適合を示すものではない。
      | モデル設定　　　　　; R=4.42 Ω。これらは保存モデルの設定値であり、すべてが実部品の保証値という意味ではない。
      | 確認の範囲　　　　　; 本説明は保存回路の部品情報・端子割当・既存設計意図を整理したもの。今回の説明更新によって新たな動作試験や実機検証を実施した意味ではない。
      | 設計記録　　　　　　; evaluation\component_annotations_20261022_r01\before_graph.json
      | evaluation\component_annotations_20261022_r01\before_metadata.json
      | evaluation\protection_capacitor_integration_20261021_r01\final_delivery\independent_readback\physical_bom.json
      | 
      | 【この説明欄の略語・記号】
      | 用語1　　　　　　　 ; MOSFET：Metal-Oxide-Semiconductor Field-Effect Transistor（金属・酸化膜・半導体構造の電界効果トランジスタ）。ゲートとソースの電圧でドレインとソースの導通を制御する素子。N-MOSはNチャネル型を表す。
      | 用語2　　　　　　　 ; GND：Ground（回路の基準電位・電流帰路）。この図の共通基準。保護接地や大地への接続を意味するとは限らない。
      | 用語3　　　　　　　 ; SW：Switching Node（スイッチング点）。主電力段の上下MOSFETとL1がつながる、電圧が高速に切り替わる点。GNDとは別電位。
      settings: AttributesFormatString=4.42 Ω
  R6 : fl_lib/Electrical/Electrical Elements/Resistor  Description=|  R=4.42 Ohm  i_specify=off  i_priority=None  i=0 A  i_nominal_specify=off  i_nominal_value=1  i_nominal_unit=A  v_specify=off  v_priority=None  v=0 V  v_nominal_specify=off  v_nominal_value=1  v_nominal_unit=V
      | この回路での名前　　; R6
      | 部品名　　　　　　　; CRCW25124R42FKEGHP
      | この回路での役割　　; 主電力MOSFET Q1・Q2の切替え時に生じる、電圧の振動を弱めるためのスナバ抵抗。
      | ここでの動き　　　　; C1と組み合わせ、切替え時の振動エネルギーを熱として消費する。R5と直列の一組になり、同じ二個直列の枝を六組並列にして抵抗値と電力負担を分ける。実際の減衰量・パルス電力・温度は別途確認する。
      | 
      | 【詳しい働き・仕様・接続・確認の範囲】
      | 部品種別　　　　　　; スナバ抵抗
      | 公称値　　　　　　　; 4.42 ohm
      | 配置目的　　　　　　; Q1/Q2のSWノードからC1へつながるスナバ抵抗網の一部。R3〜R14は2個直列の枝を6本並列にした構成。
      | 意図する動作　　　　; スイッチング時の振動エネルギーを抵抗で消費する意図。個々のパルス電力・温度・配置寄生は別途確認する。
      | 端子と接続　　　　　; 2 n → SNUB_C、1 p → SNUB_MID_2
      | モデルの範囲　　　　; Simscape抵抗の集中定数表現。部品の許容差、定格電力、温度係数、寄生インダクタンスの適合を示すものではない。
      | モデル設定　　　　　; R=4.42 Ω。これらは保存モデルの設定値であり、すべてが実部品の保証値という意味ではない。
      | 確認の範囲　　　　　; 本説明は保存回路の部品情報・端子割当・既存設計意図を整理したもの。今回の説明更新によって新たな動作試験や実機検証を実施した意味ではない。
      | 設計記録　　　　　　; evaluation\component_annotations_20261022_r01\before_graph.json
      | evaluation\component_annotations_20261022_r01\before_metadata.json
      | evaluation\protection_capacitor_integration_20261021_r01\final_delivery\independent_readback\physical_bom.json
      | 
      | 【この説明欄の略語・記号】
      | 用語1　　　　　　　 ; MOSFET：Metal-Oxide-Semiconductor Field-Effect Transistor（金属・酸化膜・半導体構造の電界効果トランジスタ）。ゲートとソースの電圧でドレインとソースの導通を制御する素子。N-MOSはNチャネル型を表す。
      | 用語2　　　　　　　 ; GND：Ground（回路の基準電位・電流帰路）。この図の共通基準。保護接地や大地への接続を意味するとは限らない。
      | 用語3　　　　　　　 ; SW：Switching Node（スイッチング点）。主電力段の上下MOSFETとL1がつながる、電圧が高速に切り替わる点。GNDとは別電位。
      settings: AttributesFormatString=4.42 Ω
  R7 : fl_lib/Electrical/Electrical Elements/Resistor  Description=|  R=4.42 Ohm  i_specify=off  i_priority=None  i=0 A  i_nominal_specify=off  i_nominal_value=1  i_nominal_unit=A  v_specify=off  v_priority=None  v=0 V  v_nominal_specify=off  v_nominal_value=1  v_nominal_unit=V
      | この回路での名前　　; R7
      | 部品名　　　　　　　; CRCW25124R42FKEGHP
      | この回路での役割　　; 主電力MOSFET Q1・Q2の切替え時に生じる、電圧の振動を弱めるためのスナバ抵抗。
      | ここでの動き　　　　; C1と組み合わせ、切替え時の振動エネルギーを熱として消費する。R8と直列の一組になり、同じ二個直列の枝を六組並列にして抵抗値と電力負担を分ける。実際の減衰量・パルス電力・温度は別途確認する。
      | 
      | 【詳しい働き・仕様・接続・確認の範囲】
      | 部品種別　　　　　　; スナバ抵抗
      | 公称値　　　　　　　; 4.42 ohm
      | 配置目的　　　　　　; Q1/Q2のSWノードからC1へつながるスナバ抵抗網の一部。R3〜R14は2個直列の枝を6本並列にした構成。
      | 意図する動作　　　　; スイッチング時の振動エネルギーを抵抗で消費する意図。個々のパルス電力・温度・配置寄生は別途確認する。
      | 端子と接続　　　　　; 2 n → SNUB_MID_3、1 p → SW
      | モデルの範囲　　　　; Simscape抵抗の集中定数表現。部品の許容差、定格電力、温度係数、寄生インダクタンスの適合を示すものではない。
      | モデル設定　　　　　; R=4.42 Ω。これらは保存モデルの設定値であり、すべてが実部品の保証値という意味ではない。
      | 確認の範囲　　　　　; 本説明は保存回路の部品情報・端子割当・既存設計意図を整理したもの。今回の説明更新によって新たな動作試験や実機検証を実施した意味ではない。
      | 設計記録　　　　　　; evaluation\component_annotations_20261022_r01\before_graph.json
      | evaluation\component_annotations_20261022_r01\before_metadata.json
      | evaluation\protection_capacitor_integration_20261021_r01\final_delivery\independent_readback\physical_bom.json
      | 
      | 【この説明欄の略語・記号】
      | 用語1　　　　　　　 ; MOSFET：Metal-Oxide-Semiconductor Field-Effect Transistor（金属・酸化膜・半導体構造の電界効果トランジスタ）。ゲートとソースの電圧でドレインとソースの導通を制御する素子。N-MOSはNチャネル型を表す。
      | 用語2　　　　　　　 ; GND：Ground（回路の基準電位・電流帰路）。この図の共通基準。保護接地や大地への接続を意味するとは限らない。
      | 用語3　　　　　　　 ; SW：Switching Node（スイッチング点）。主電力段の上下MOSFETとL1がつながる、電圧が高速に切り替わる点。GNDとは別電位。
      settings: AttributesFormatString=4.42 Ω
  R8 : fl_lib/Electrical/Electrical Elements/Resistor  Description=|  R=4.42 Ohm  i_specify=off  i_priority=None  i=0 A  i_nominal_specify=off  i_nominal_value=1  i_nominal_unit=A  v_specify=off  v_priority=None  v=0 V  v_nominal_specify=off  v_nominal_value=1  v_nominal_unit=V
      | この回路での名前　　; R8
      | 部品名　　　　　　　; CRCW25124R42FKEGHP
      | この回路での役割　　; 主電力MOSFET Q1・Q2の切替え時に生じる、電圧の振動を弱めるためのスナバ抵抗。
      | ここでの動き　　　　; C1と組み合わせ、切替え時の振動エネルギーを熱として消費する。R7と直列の一組になり、同じ二個直列の枝を六組並列にして抵抗値と電力負担を分ける。実際の減衰量・パルス電力・温度は別途確認する。
      | 
      | 【詳しい働き・仕様・接続・確認の範囲】
      | 部品種別　　　　　　; スナバ抵抗
      | 公称値　　　　　　　; 4.42 ohm
      | 配置目的　　　　　　; Q1/Q2のSWノードからC1へつながるスナバ抵抗網の一部。R3〜R14は2個直列の枝を6本並列にした構成。
      | 意図する動作　　　　; スイッチング時の振動エネルギーを抵抗で消費する意図。個々のパルス電力・温度・配置寄生は別途確認する。
      | 端子と接続　　　　　; 2 n → SNUB_C、1 p → SNUB_MID_3
      | モデルの範囲　　　　; Simscape抵抗の集中定数表現。部品の許容差、定格電力、温度係数、寄生インダクタンスの適合を示すものではない。
      | モデル設定　　　　　; R=4.42 Ω。これらは保存モデルの設定値であり、すべてが実部品の保証値という意味ではない。
      | 確認の範囲　　　　　; 本説明は保存回路の部品情報・端子割当・既存設計意図を整理したもの。今回の説明更新によって新たな動作試験や実機検証を実施した意味ではない。
      | 設計記録　　　　　　; evaluation\component_annotations_20261022_r01\before_graph.json
      | evaluation\component_annotations_20261022_r01\before_metadata.json
      | evaluation\protection_capacitor_integration_20261021_r01\final_delivery\independent_readback\physical_bom.json
      | 
      | 【この説明欄の略語・記号】
      | 用語1　　　　　　　 ; MOSFET：Metal-Oxide-Semiconductor Field-Effect Transistor（金属・酸化膜・半導体構造の電界効果トランジスタ）。ゲートとソースの電圧でドレインとソースの導通を制御する素子。N-MOSはNチャネル型を表す。
      | 用語2　　　　　　　 ; GND：Ground（回路の基準電位・電流帰路）。この図の共通基準。保護接地や大地への接続を意味するとは限らない。
      | 用語3　　　　　　　 ; SW：Switching Node（スイッチング点）。主電力段の上下MOSFETとL1がつながる、電圧が高速に切り替わる点。GNDとは別電位。
      settings: AttributesFormatString=4.42 Ω
  R9 : fl_lib/Electrical/Electrical Elements/Resistor  Description=|  R=4.42 Ohm  i_specify=off  i_priority=None  i=0 A  i_nominal_specify=off  i_nominal_value=1  i_nominal_unit=A  v_specify=off  v_priority=None  v=0 V  v_nominal_specify=off  v_nominal_value=1  v_nominal_unit=V
      | この回路での名前　　; R9
      | 部品名　　　　　　　; CRCW25124R42FKEGHP
      | この回路での役割　　; 主電力MOSFET Q1・Q2の切替え時に生じる、電圧の振動を弱めるためのスナバ抵抗。
      | ここでの動き　　　　; C1と組み合わせ、切替え時の振動エネルギーを熱として消費する。R10と直列の一組になり、同じ二個直列の枝を六組並列にして抵抗値と電力負担を分ける。実際の減衰量・パルス電力・温度は別途確認する。
      | 
      | 【詳しい働き・仕様・接続・確認の範囲】
      | 部品種別　　　　　　; スナバ抵抗
      | 公称値　　　　　　　; 4.42 ohm
      | 配置目的　　　　　　; Q1/Q2のSWノードからC1へつながるスナバ抵抗網の一部。R3〜R14は2個直列の枝を6本並列にした構成。
      | 意図する動作　　　　; スイッチング時の振動エネルギーを抵抗で消費する意図。個々のパルス電力・温度・配置寄生は別途確認する。
      | 端子と接続　　　　　; 2 n → SNUB_MID_4、1 p → SW
      | モデルの範囲　　　　; Simscape抵抗の集中定数表現。部品の許容差、定格電力、温度係数、寄生インダクタンスの適合を示すものではない。
      | モデル設定　　　　　; R=4.42 Ω。これらは保存モデルの設定値であり、すべてが実部品の保証値という意味ではない。
      | 確認の範囲　　　　　; 本説明は保存回路の部品情報・端子割当・既存設計意図を整理したもの。今回の説明更新によって新たな動作試験や実機検証を実施した意味ではない。
      | 設計記録　　　　　　; evaluation\component_annotations_20261022_r01\before_graph.json
      | evaluation\component_annotations_20261022_r01\before_metadata.json
      | evaluation\protection_capacitor_integration_20261021_r01\final_delivery\independent_readback\physical_bom.json
      | 
      | 【この説明欄の略語・記号】
      | 用語1　　　　　　　 ; MOSFET：Metal-Oxide-Semiconductor Field-Effect Transistor（金属・酸化膜・半導体構造の電界効果トランジスタ）。ゲートとソースの電圧でドレインとソースの導通を制御する素子。N-MOSはNチャネル型を表す。
      | 用語2　　　　　　　 ; GND：Ground（回路の基準電位・電流帰路）。この図の共通基準。保護接地や大地への接続を意味するとは限らない。
      | 用語3　　　　　　　 ; SW：Switching Node（スイッチング点）。主電力段の上下MOSFETとL1がつながる、電圧が高速に切り替わる点。GNDとは別電位。
      settings: AttributesFormatString=4.42 Ω
  ReadLabel_D3_VSYS_5V : ConnectionLabel  Description=|  Label=VSYS_5V
      | この回路での名前　　; VSYS_5V
      | 種別　　　　　　　　; ConnectionLabel
      | この回路での役割　　; ダイオードD3の出力を、RP2040基板U7のVSYS電源入力へ渡す。P5からはD3を介して供給されるため、P5とは別ノード。
      | この場所の直接接続　; D3（DIODE／40V 1A Schottky VSYS OR）: 1(K)
      | 直接接続の範囲　　　; このラベルから実際の線・分岐・明示的な境界端子だけを追った接続。同名ラベルによる離れた場所への接続はこの欄に含めない。
      | 同一ネットの主接続　; D3（DIODE／40V 1A Schottky VSYS OR）: 1(K)
      |                     ; U7（RP2040搭載Pico W／SC0918）: 39(VSYS)
      | 同一ネット全端子　　; D3: 1(K)
      |                     ; U7: 39(VSYS)
      | 接続部品数　　　　　; 2部品（部品番号で集計。同一ネット全体）
      | 接続端子数　　　　　; 2端子（423端子の部品対応表で集計。ラベル・境界ポートの重複は含めない）
      | この場所の端子数　　; 1端子／1部品（同名ラベルによる接続を除く）
      | 同階層同名ラベル数　; 2個（このラベル自身を含む）
      | 全階層の接続ラベル　; 2個（実際に同じノードへつながるラベル。名前が違う別名も含む）
      | 接続ルール　　　　　; 同じ階層の同じラベル名を仮想配線として結ぶ。別のSubsystem内とは名前だけでつながらず、明示的なConnection Portと配線をたどる。色は用途の表示であり接続を決めない。
      | 確認の範囲　　　　　; 現在の保存回路の端子・配線から求めた静的接続。抵抗やICの内部を導線として短絡せずに集計した。説明の更新は動作シミュレーション、タイミング、実部品の性能・実機動作を保証するものではない。
      | 記録の基準　　　　　; measurement_label_layout_20261022_r01/after_layout_graph.json。部品対応表は端子名の対応付けにのみ使用。
      | 
      | 【この説明欄の略語・記号】
      | 用語1　　　　　　　 ; IC：Integrated Circuit（集積回路）。複数の電子素子と機能を小さな半導体チップに集積した部品。
  ReadLabel_R15_SPI_CS_N : ConnectionLabel  Description=|  Label=SPI_CS_N
      | この回路での名前　　; SPI_CS_N
      | 種別　　　　　　　　; ConnectionLabel
      | この回路での役割　　; RP2040基板U7のGP17と、外付けADC U1のCS_Nを結ぶSPIチップ選択信号。R15によって3.3Vへプルアップする。
      | この場所の直接接続　; R15（SPI_CS_Nを3V3へ引き上げ、RP2040の出力が未確定なときにU1を非選択側へ保つ／10 kohm）: 2
      | 直接接続の範囲　　　; このラベルから実際の線・分岐・明示的な境界端子だけを追った接続。同名ラベルによる離れた場所への接続はこの欄に含めない。
      | 同一ネットの主接続　; U7（RP2040搭載Pico W／SC0918）: 22(GP17)
      |                     ; U1（外付けADC／MCP3208-CI/SL）: 10(CS_N)
      |                     ; R15（SPI_CS_Nを3V3へ引き上げ、RP2040の出力が未確定なときにU1を非選択側へ保つ／10 kohm）: 2
      | 同一ネット全端子　　; R15: 2
      |                     ; U1: 10(CS_N)
      |                     ; U7: 22(GP17)
      | 接続部品数　　　　　; 3部品（部品番号で集計。同一ネット全体）
      | 接続端子数　　　　　; 3端子（423端子の部品対応表で集計。ラベル・境界ポートの重複は含めない）
      | この場所の端子数　　; 1端子／1部品（同名ラベルによる接続を除く）
      | 同階層同名ラベル数　; 3個（このラベル自身を含む）
      | 全階層の接続ラベル　; 3個（実際に同じノードへつながるラベル。名前が違う別名も含む）
      | 接続ルール　　　　　; 同じ階層の同じラベル名を仮想配線として結ぶ。別のSubsystem内とは名前だけでつながらず、明示的なConnection Portと配線をたどる。色は用途の表示であり接続を決めない。
      | 確認の範囲　　　　　; 現在の保存回路の端子・配線から求めた静的接続。抵抗やICの内部を導線として短絡せずに集計した。説明の更新は動作シミュレーション、タイミング、実部品の性能・実機動作を保証するものではない。
      | 記録の基準　　　　　; measurement_label_layout_20261022_r01/after_layout_graph.json。部品対応表は端子名の対応付けにのみ使用。
      | 
      | 【この説明欄の略語・記号】
      | 用語1　　　　　　　 ; ADC：Analog-to-Digital Converter（アナログ・デジタル変換器）。測定電圧をデジタル値へ変換する回路。電流や温度も、センサーで電圧へ変換した後に読み取る。
      | 用語2　　　　　　　 ; IC：Integrated Circuit（集積回路）。複数の電子素子と機能を小さな半導体チップに集積した部品。
      | 用語3　　　　　　　 ; GPIO：General-Purpose Input/Output（汎用入出力端子）。入力・出力や周辺機能に割り当てられる端子。GPの後の数字はRP2040の端子信号番号で、基板上の物理ピン番号とは別。
      | 用語4　　　　　　　 ; SPI：Serial Peripheral Interface（同期式シリアル通信）。クロックとデータ線を使う通信方式。本回路ではRP2040と外付け測定用ADCの通信に使う。
      | 用語5　　　　　　　 ; CS_N：Chip Select（チップ選択信号）。末尾Nはこの設計でLow有効を表す。Lowにして通信対象のADCを選択する。
  ReadLabel_R15_V3V3 : ConnectionLabel  Description=|  Label=V3V3
      | この回路での名前　　; V3V3
      | 種別　　　　　　　　; ConnectionLabel
      | この回路での役割　　; RP2040基板U7の3.3V出力から、ADC・電流検出IC・温度センサー・基準電圧ICなどへ電源を分配する。信号のプルアップ抵抗にも供給する。
      | この場所の直接接続　; R15（SPI_CS_Nを3V3へ引き上げ、RP2040の出力が未確定なときにU1を非選択側へ保つ／10 kohm）: 1
      | 直接接続の範囲　　　; このラベルから実際の線・分岐・明示的な境界端子だけを追った接続。同名ラベルによる離れた場所への接続はこの欄に含めない。
      | 同一ネットの主接続　; U7（RP2040搭載Pico W／SC0918）: 36(3V3_OUT)
      |                     ; U1（外付けADC／MCP3208-CI/SL）: 16(VDD)
      |                     ; U2（PV入力電流の検出アンプ／INA241A3IDDFR）: 6(VS)
      |                     ; U3（L1直後の出力電流の検出アンプ／INA241A3IDDFR）: 6(VS)
      |                     ; U4（電池温度センサー／TMP235A2DBZR）: 1(VDD)
      |                     ; U5（放熱器温度センサー／TMP235A2DBZR）: 1(VDD)
      |                     ; U6（2.5Vの測定基準電圧源／REF3025EAIDBZR）: 1(IN)
      |                     ; R49（U10のオープンドレインPG信号BIAS_PGをPicoの3V3へ引き上げ、GP9で読める電圧にする／10k 1%）: 2
      |                     ; P_RFLT_PU（LTC4364のオープンドレインFLTをMCUの3.3 V系へ引き上げる／22 kΩ）: 1
      | 同一ネット全端子　　; C17: 1
      |                     ; C18: 1
      |                     ; C22: 1
      |                     ; C24: 1
      |                     ; C26: 1
      |                     ; C28: 1
      |                     ; C30: 1
      |                     ; P_RFLT_PU: 1
      |                     ; R15: 1
      |                     ; R49: 2
      |                     ; U1: 16(VDD)
      |                     ; U2: 6(VS)
      |                     ; U3: 6(VS)
      |                     ; U4: 1(VDD)
      |                     ; U5: 1(VDD)
      |                     ; U6: 1(IN)
      |                     ; U7: 36(3V3_OUT)
      | 接続部品数　　　　　; 17部品（部品番号で集計。同一ネット全体）
      | 接続端子数　　　　　; 17端子（423端子の部品対応表で集計。ラベル・境界ポートの重複は含めない）
      | この場所の端子数　　; 1端子／1部品（同名ラベルによる接続を除く）
      | 同階層同名ラベル数　; 10個（このラベル自身を含む）
      | 全階層の接続ラベル　; 10個（実際に同じノードへつながるラベル。名前が違う別名も含む）
      | 接続ルール　　　　　; 同じ階層の同じラベル名を仮想配線として結ぶ。別のSubsystem内とは名前だけでつながらず、明示的なConnection Portと配線をたどる。色は用途の表示であり接続を決めない。
      | 確認の範囲　　　　　; 現在の保存回路の端子・配線から求めた静的接続。抵抗やICの内部を導線として短絡せずに集計した。説明の更新は動作シミュレーション、タイミング、実部品の性能・実機動作を保証するものではない。
      | 記録の基準　　　　　; measurement_label_layout_20261022_r01/after_layout_graph.json。部品対応表は端子名の対応付けにのみ使用。
      | 
      | 【この説明欄の略語・記号】
      | 用語1　　　　　　　 ; ADC：Analog-to-Digital Converter（アナログ・デジタル変換器）。測定電圧をデジタル値へ変換する回路。電流や温度も、センサーで電圧へ変換した後に読み取る。
      | 用語2　　　　　　　 ; IC：Integrated Circuit（集積回路）。複数の電子素子と機能を小さな半導体チップに集積した部品。
      | 用語3　　　　　　　 ; MCU：Microcontroller Unit（マイクロコントローラ）。プログラムを実行し、測定値の処理や出力制御を担当する小型計算機。
      | 用語4　　　　　　　 ; GPIO：General-Purpose Input/Output（汎用入出力端子）。入力・出力や周辺機能に割り当てられる端子。GPの後の数字はRP2040の端子信号番号で、基板上の物理ピン番号とは別。
      | 用語5　　　　　　　 ; SPI：Serial Peripheral Interface（同期式シリアル通信）。クロックとデータ線を使う通信方式。本回路ではRP2040と外付け測定用ADCの通信に使う。
      | 用語6　　　　　　　 ; CS_N：Chip Select（チップ選択信号）。末尾Nはこの設計でLow有効を表す。Lowにして通信対象のADCを選択する。
      | 用語7　　　　　　　 ; MOSFET：Metal-Oxide-Semiconductor Field-Effect Transistor（金属・酸化膜・半導体構造の電界効果トランジスタ）。ゲートとソースの電圧でドレインとソースの導通を制御する素子。N-MOSはNチャネル型を表す。
      | 用語8　　　　　　　 ; PV：Photovoltaic（太陽光発電）。光を電気へ変える発電方式。PVを含むネット名は太陽電池側の測定・電力経路を表す。
      | 用語9　　　　　　　 ; GND：Ground（回路の基準電位・電流帰路）。この図の共通基準。保護接地や大地への接続を意味するとは限らない。
      | 用語10　　　　　　　; PG：Power Good（電源状態通知）。電源出力が規定状態にあるかを知らせる信号。プルアップ条件と実際の通知条件は対象ICの説明で確認する。
      | 用語11　　　　　　　; FLT：Fault（故障状態通知）。LTC4364の故障警告出力。全種類の異常や逆流を一律に通知する信号という意味ではない。
      | 用語12　　　　　　　; VCC/VDD/VEE/VS：ICの電源端子名。文字の歴史的な由来を現在の接続機能へ当てはめない。現回路のVEEはU8/U10では浮動基準SW、U9ではGND。各電圧・基準は端子と接続を参照する。
      | 用語13　　　　　　　; SW：Switching Node（スイッチング点）。主電力段の上下MOSFETとL1がつながる、電圧が高速に切り替わる点。GNDとは別電位。
  ReadLabel_R22_BAT_PLUS : ConnectionLabel  Description=|  Label=BAT_PLUS
      | この回路での名前　　; BAT_PLUS
      | 種別　　　　　　　　; ConnectionLabel
      | この回路での役割　　; 保護回路の出力、充電経路のヒューズF3、電池側電圧測定の分圧抵抗R22上側を結ぶ。BT1正極へはF3を介してつながる。
      | この場所の直接接続　; R22（電池側電圧の分圧抵抗・上側／75 kohm 0.1%）: 1
      | 直接接続の範囲　　　; このラベルから実際の線・分岐・明示的な境界端子だけを追った接続。同名ラベルによる離れた場所への接続はこの欄に含めない。
      | 同一ネットの主接続　; F3（BT1と充電器の間の充電経路を保護するヒューズ／25A DC）: 2
      |                     ; R22（電池側電圧の分圧抵抗・上側／75 kohm 0.1%）: 1
      |                     ; P_U1（保護MOSFETを制御する保護IC／LTC4364IMS-1#PBF）: OUT
      |                     ; P_RSNS（保護ICの電流検出抵抗／2.7 mΩ）: 2
      |                     ; P_COUT（保護回路出力側のコンデンサ／330 µF）: P
      |                     ; P_R7（BAT_PLUSからP_FBへ接続し、P_R8とともに出力電圧クランプの帰還比を作る／236 kΩ）: 1
      | 部品を介する経路　　; R22→R23の上側抵抗とR24の下側抵抗で分圧し、C21とADC U1のCH6へ渡す。ADC入力はBAT_PLUSと同じ導線ではない。F3の反対側はBT1正極のBAT_RAW。
      | 同一ネット全端子　　; F3: 2
      |                     ; P_COUT: P
      |                     ; P_R7: 1
      |                     ; P_RSNS: 2
      |                     ; P_U1: OUT
      |                     ; R22: 1
      | 接続部品数　　　　　; 6部品（部品番号で集計。同一ネット全体）
      | 接続端子数　　　　　; 6端子（423端子の部品対応表で集計。ラベル・境界ポートの重複は含めない）
      | この場所の端子数　　; 1端子／1部品（同名ラベルによる接続を除く）
      | 同階層同名ラベル数　; 2個（このラベル自身を含む）
      | 全階層の接続ラベル　; 2個（実際に同じノードへつながるラベル。名前が違う別名も含む）
      | 接続ルール　　　　　; 同じ階層の同じラベル名を仮想配線として結ぶ。別のSubsystem内とは名前だけでつながらず、明示的なConnection Portと配線をたどる。色は用途の表示であり接続を決めない。
      | 確認の範囲　　　　　; 現在の保存回路の端子・配線から求めた静的接続。抵抗やICの内部を導線として短絡せずに集計した。説明の更新は動作シミュレーション、タイミング、実部品の性能・実機動作を保証するものではない。
      | 記録の基準　　　　　; measurement_label_layout_20261022_r01/after_layout_graph.json。部品対応表は端子名の対応付けにのみ使用。
      | 
      | 【この説明欄の略語・記号】
      | 用語1　　　　　　　 ; DC：Direct Current（直流）。ここでは直流電源または直流成分。DCバイアスはコンデンサに重なる直流電圧を指す。
